simulink model "Controller_trorque_cbf_22Franka"  (R2022b)
settings: Solver=FixedStepDiscrete  StartTime=0.0  StopTime=inf  FixedStep=0.001  RelTol=1e-3
PreLoadFcn:
  | set_param(gcs, 'RTWSystemTargetFile', 'franka_emika_panda.tlc');
  | 
  | demos_common_configs();
  | collision_behavior = ones(1,52)*100;
values from neighbouring files (symbols this model uses):
  b_sg = fliplr(B(end, :))    [init_torque_cbf.m]
  cbf_dt = 0.001    [init_torque_cbf.m]
  cbf_Kd_rot = [120; 120; 120]*0    [init_torque_cbf.m]
  cbf_Kd_trans = [2000; 2000; 0]*0    [init_torque_cbf.m]
  cbf_stiff_decouple = 0    [init_torque_cbf.m]
  cbf_zeta_rot = [0.7; 0.7; 0.7]*0    [init_torque_cbf.m]
  cbf_zeta_trans = [0.7; 0.7; 0]*0    [init_torque_cbf.m]
  Dn = 20 * ones(7,1)    [init_torque_cbf.m]
  H_home = getTransform(Franka_robot, q_home, 'panda_link8', 'panda_link0')    [init_torque_cbf.m]
  Kn = 0 * ones(7,1)    [init_torque_cbf.m]
  plane_normal = [0.0; 0.0; 1.0]    [init_torque_cbf.m]
  q_home = q_init    [init_torque_cbf.m]
  q_init = [0 0  0  -(2/4)*pi  0  pi/2  -pi/4]'    [init_torque_cbf.m]
undefined symbols (not defined in the file or in its folder): cbf_torque_params, DiscIntNeverNeededParam, Fext_mag
libraries: franka_simulink_library x2, Robotics_lib x1, matrix_library x1
(part 6 of 7)

== matlab function Controller_trorque_cbf_22Franka/Dynamic Parameters/Coriolis Matrix ==
  data: q input; m output; q_dot input
function m = maple_R7plus_coriolismatrix_02(q, q_dot)
% Author: TU Wien, ACIN Robotics group
% Optimized and generated from Maple
  m = zeros(7,7);
  t2607 = q(4);
  t2593 = cos(t2607);
  t2531 = 0.345563e0 * t2593;
  t2606 = q(5);
  t2585 = sin(t2606);
  t2592 = cos(t2606);
  t3061 = 0.41065e-1 * t2585 + 0.11953e-1 * t2592;
  t2285 = t3061 + 0.825e-1;
  t2586 = sin(t2607);
  t3832 = t2285 * t2586;
  t3327 = -0.316e0 + t3832;
  t1967 = t2531 - t3327;
  t2609 = q(2);
  t2595 = cos(t2609);
  t3493 = 0.41065e-1 * t2592;
  t2464 = 0.11953e-1 * t2585 - t3493;
  t2608 = q(3);
  t2587 = sin(t2608);
  t3786 = t2587 * t2464;
  t2594 = cos(t2608);
  t2528 = 0.345563e0 * t2586;
  t3831 = t2285 * t2593;
  t4080 = t2528 + t3831;
  t3385 = 0.825e-1 - t4080;
  t4278 = t3385 * t2594;
  t1699 = t4278 + t3786;
  t2588 = sin(t2609);
  t3947 = t1699 * t2588;
  t1517 = -t1967 * t2595 + t3947;
  t2610 = q(1);
  t2596 = cos(t2610);
  t3108 = 0.61297300000000000000000000000000e0 * t2596;
  t3044 = t1517 * t3108;
  t4305 = 0.1e1 * t3044;
  t2605 = q(6);
  t2584 = sin(t2605);
  t2591 = cos(t2605);
  t2467 = 0.60149e-1 * t2591 + 0.14117e-1 * t2584;
  t3495 = 0.10517e-1 * t2592;
  t3243 = t2467 * t2585 + t3495;
  t2789 = t3243 * t2587;
  t2463 = 0.60149e-1 * t2584 - 0.14117e-1 * t2591;
  t2283 = t2463 + 0.384e0;
  t2155 = t2283 * t2586;
  t3503 = 0.10517e-1 * t2585;
  t2822 = -t2467 * t2592 + t3503;
  t4152 = 0.825e-1 + t2822;
  t4214 = t4152 * t2593;
  t3516 = -t4214 + 0.825e-1;
  t4288 = t3516 - t2155;
  t1526 = t2594 * t4288 - t2789;
  t4206 = t1526 * t2595;
  t4304 = 0.1e1 * t1526;
  t2604 = q(7);
  t2583 = sin(t2604);
  t2085 = 0.48418875570424600000000000000000e-2 * t2583 + 0.55042935974400000000000000000000e-3;
  t2590 = cos(t2604);
  t2576 = t2590 ^ 2;
  t2317 = 0.48418875570424600000000000000000e-2 * t2576;
  t3208 = 0.31608697465260160000000000000000e-2 * t2583;
  t2179 = t2590 * t3208;
  t2413 = 0.13614453378240000000000000000000e-2 * t2590;
  t3715 = t2179 - t2413;
  t1629 = -t2085 * t2583 + t2317 + t3715;
  t2417 = 0.51602752476000000000000000000000e-3 * t2590;
  t3214 = 0.12763550042100000000000000000000e-2 * t2583;
  t3681 = -t3214 + t2417;
  t1504 = t1629 * t2585 + t3681;
  t3793 = t2585 * t2584;
  t4076 = -0.33449653235675560000000000000000e-2 * t2590 + 0.10967182128164640000000000000000e-2 * t2583;
  t4303 = t2592 * (t1504 * t2591 + t3793 * t4076);
  t4301 = t1504 * t2584;
  t1692 = t1699 * t2595;
  t2156 = t2283 * t2593;
  t4215 = t2586 * t4152;
  t4230 = t2156 - t4215;
  t1706 = t4230 + 0.316e0;
  t4300 = t1706 * t2588;
  t2578 = t2592 ^ 2;
  t4235 = t1629 * t2591 + t2584 * t4076;
  t4299 = t4235 * t2578;
  t2129 = 0.4841887557042460000000000000000e-2 * t2583 + 0.55042935974400000000000000000000e-3;
  t2324 = 0.15804348732630080000000000000000e-2 * t2576;
  t2356 = 0.13614453378240000000000000000000e-2 * t2583;
  t3689 = t2324 + t2356;
  t1675 = -t2129 * t2590 + t3689 - 0.5826996021941340000000000000000e-3;
  t2347 = 0.59408523832320000000000000000000e-2 * t2583;
  t2412 = 0.24018735697920000000000000000000e-2 * t2590;
  t2026 = t2347 - t2412;
  t1891 = 0.47796540830203740000000000000000e-1 - t2026;
  t1498 = -t1675 * t2584 + t1891;
  t3158 = 0.10967182128164640000000000000000e-2 * t2590;
  t3207 = 0.33449653235675560000000000000000e-2 * t2583;
  t2029 = t3158 + t3207;
  t1896 = t2029 + 0.18713819462921000000000000000000e-3;
  t3916 = t1896 * t2591;
  t4289 = t1498 + t3916;
  t4298 = t4289 * t2592;
  t3802 = t2583 * t2590;
  t3035 = 0.85600000000000000000000000000000e-3 * t3802;
  t2812 = 0.28220000000000000000000000000000e-2 + t3035;
  t3238 = 0.2489000000000000000000000000000e-2 * t2576;
  t1821 = t2812 + t3238;
  t2577 = t2591 ^ 2;
  t1775 = t1821 * t2577;
  t4174 = -0.23920000000000000000000000000000e-2 * t2590 + 0.14820000000000000000000000000000e-2 * t2583;
  t1985 = -t4174 + 0.218e-3;
  t3796 = t2584 * t2591;
  t3618 = t1985 * t3796;
  t2321 = 0.24890000000000000000000000000000e-2 * t2576;
  t1809 = t2321 + t2812;
  t3710 = -t3035 - t2321;
  t1812 = -t3710 - 0.27050000000000000000000000000000e-2;
  t1414 = t1809 * t2577 + t1812 - t3618;
  t1397 = t1414 * t2578;
  t3154 = 0.14820000000000000000000000000000e-2 * t2590;
  t2200 = t2584 * t3154;
  t3211 = 0.23920000000000000000000000000000e-2 * t2583;
  t2267 = 0.682e-3 + t3211;
  t3033 = 0.49780000000000000000000000000000e-2 * t3802;
  t3222 = 0.17120000000000000000000000000000e-2 * t2576;
  t2726 = t3033 - t3222 - 0.14600000000000000000000000000000e-2;
  t2713 = t2726 * t2591;
  t3534 = t2267 * t2584 + t2200 - t2713;
  t1549 = 0.4234e-2 - t3534;
  t3761 = t2592 * t2585;
  t1518 = t1549 * t3761;
  t3736 = -t1518 - t1397;
  t4297 = -t3736 - t3618 + t1775;
  t1960 = t3681 * t2584;
  t2408 = 0.59408523832320000000000000000000e-2 * t2590;
  t3210 = 0.24018735697920000000000000000000e-2 * t2583;
  t3678 = -t3210 - t2408;
  t4286 = t1629 * t2584 + t3678;
  t4295 = -t2585 * t4286 - t1960;
  t2024 = 0.10517000000000000000000000000000e-1 * t2583 - 0.42520000000000000000000000000000e-2 * t2590;
  t1962 = t2024 * t2585;
  t2028 = 0.10517000000000000000000000000000e-1 * t2590 + 0.42520000000000000000000000000000e-2 * t2583;
  t1887 = 0.88000000000000000000000000000000e-1 + t2028;
  t3197 = 0.61597000000000000000000000000000e-1 * t2584;
  t3764 = t2591 * t2592;
  t3725 = t1887 * t3764 + t2592 * t3197;
  t4099 = t1962 + t3725;
  t1501 = 0.82500000000000000000000000000000e-1 - t4099;
  t4294 = t1501 * t2586;
  t4293 = t1501 * t2593;
  t3213 = 0.15804348732630080000000000000000e-2 * t2583;
  t2089 = -0.27228906756480000000000000000000e-2 + t3213;
  t3157 = 0.11008587194880000000000000000000e-2 * t2590;
  t3141 = 0.96837751140849200000000000000000e-2 * t2590;
  t2177 = t2583 * t3141;
  t3706 = -t2177 + t2324;
  t1627 = t2089 * t2583 + t3157 - t3706;
  t4275 = t1627 * t2584 - t2026;
  t3976 = t4275 * t2591;
  t2318 = 0.48152918111602840000000000000000e-2 * t2576;
  t2569 = t2583 ^ 2;
  t2299 = 0.26595745882176000000000000000000e-4 * t2569;
  t2357 = 0.11008587194880000000000000000000e-2 * t2583;
  t3692 = -t2299 - t2357;
  t3848 = t2089 * t2590;
  t3524 = -t3848 - t3692;
  t2932 = 0.17806630741175110000000000000000e-1 + t3524;
  t1592 = -t2318 + t2932;
  t2902 = (0.2e1 * t1592 - 0.12491350982639572000000000000000e-1) * t3796;
  t2589 = sin(t2610);
  t2575 = t2589 ^ 2;
  t2582 = t2596 ^ 2;
  t4260 = t2575 + t2582;
  t1322 = -t1526 * t2588 + t1706 * t2595;
  t2466 = 0.39252e-1 * t2594 + 0.27518e-1 * t2587;
  t3481 = 0.249498e0 * t2588;
  t3059 = 0.39252e-1 * t2587 - 0.27518e-1 * t2594;
  t4201 = t3059 * t2595;
  t2818 = t4201 - t3481;
  t4273 = t2466 * t2589 + t2596 * t2818;
  t4292 = 0.1e1 * t4273;
  t3970 = t1592 * t2577;
  t3201 = 0.11357396418885000000000000000000e-1 * t2584;
  t2099 = -0.24178658687700000000000000000000e-2 + t3201;
  t3155 = 0.12763550042100000000000000000000e-2 * t2590;
  t3220 = 0.51602752476000000000000000000000e-3 * t2583;
  t3684 = -t3220 - t3155;
  t1894 = -t3684 + 0.27219646194675000000000000000000e-1;
  t3918 = t1894 * t2591;
  t1681 = -t3918 - t2099;
  t3952 = t1681 * t2585;
  t1651 = t1681 * t2592;
  t2470 = 0.10517e-1 * t2590 + 0.4252e-2 * t2583;
  t2288 = t2470 + 0.88e-1;
  t3504 = 0.61597e-1 * t2584;
  t3244 = t2288 * t2591 + t3504;
  t3065 = 0.10517e-1 * t2583 - 0.4252e-2 * t2590;
  t4212 = t2585 * t3065;
  t2699 = t2592 * t3244 + t4212;
  t2693 = 0.825e-1 - t2699;
  t4290 = t2593 * t2693;
  t1595 = t1627 * t2577;
  t3676 = -0.66899306471351120000000000000000e-2 * t2583 - 0.21934364256329280000000000000000e-2 * t2590;
  t1922 = t3676 * t3796;
  t3262 = -t1922 - t1595;
  t2361 = 0.63817750210500000000000000000000e-3 * t2583;
  t2418 = 0.25801376238000000000000000000000e-3 * t2590;
  t3682 = t2418 - t2361;
  t2415 = 0.68072266891200000000000000000000e-3 * t2590;
  t3209 = 0.24209437785212300000000000000000e-2 * t2583;
  t2088 = 0.27521467987200000000000000000000e-3 + t3209;
  t3851 = t2088 * t2583;
  t3153 = 0.15804348732630080000000000000000e-2 * t2590;
  t2181 = t2583 * t3153;
  t2322 = 0.24209437785212300000000000000000e-2 * t2576;
  t4094 = t2181 + t2322;
  t1631 = t2415 + t3851 - t4094;
  t3966 = t1631 * t2585;
  t4287 = t3682 - t3966;
  t3496 = 0.61597e-1 * t2591;
  t3830 = t2288 * t2584;
  t2783 = -t3496 + t3830;
  t4044 = 0.384e0 + t2783;
  t3889 = t4044 * t2593;
  t4285 = t2586 * t2693 - t3889 - 0.316e0;
  t4283 = t1631 * t2584;
  t4282 = t1631 * t2591;
  t3506 = 0.5317e-1 * t2593;
  t3060 = 0.104419e0 * t2586 + t3506;
  t2286 = t3060 - 0.825e-1;
  t3497 = 0.27454e-1 * t2587;
  t2015 = t2286 * t2594 - t3497;
  t1943 = t2015 * t2595;
  t3511 = 0.5317e-1 * t2586;
  t2516 = -0.316e0 + t3511;
  t3475 = 0.104419e0 * t2593;
  t1694 = t2588 * (t2516 - t3475) + t1943;
  t4281 = t1694 * t2596;
  t4210 = t3385 * t2587;
  t4200 = t3065 * t2592;
  t2700 = t2585 * t3244 - t4200;
  t3888 = t4044 * t2586;
  t4045 = 0.825e-1 - t3888;
  t2661 = -t2700 * t2587 + (t4045 - t4290) * t2594;
  t1089 = t2588 * t2661 + t2595 * t4285;
  t4169 = 0.735522e0 * t4260 * t1089;
  t1924 = 0.3742763892584200000000000000000e-3 - t3676;
  t3900 = t1924 * t2591;
  t2084 = 0.96837751140849200000000000000000e-2 * t2583 + 0.11008587194880000000000000000000e-2;
  t2319 = 0.31608697465260160000000000000000e-2 * t2576;
  t2351 = 0.27228906756480000000000000000000e-2 * t2583;
  t4227 = t2319 + t2351 - 0.11653992043882680000000000000000e-2;
  t1667 = -t2084 * t2590 + t4227;
  t4268 = t1667 * t2584;
  t4277 = t3900 - t4268;
  t3223 = 0.85600000000000000000000000000000e-3 * t2576;
  t2804 = -0.85600000000000000000000000000000e-3 * t2569 + t3223;
  t1783 = t2804 - t3033;
  t2033 = t3154 + t3211;
  t3614 = t2033 * t3796;
  t1393 = t1783 * t2577 + t1783 + t3614;
  t3705 = t4174 * t2584;
  t2316 = 0.49780000000000000000000000000000e-2 * t2576;
  t4090 = -0.49780000000000000000000000000000e-2 * t2569 + t2316 + 0.34240000000000000000000000000000e-2 * t3802;
  t4165 = t2591 * t4090 + t3705;
  t3737 = -t1393 * t2578 - t3761 * t4165;
  t2341 = 0.4841887557042460000000000000000e-2 * t2576;
  t3869 = t4076 * t2591;
  t3444 = -t3678 + t3869;
  t4274 = t2584 * (-t2129 * t2583 + t2341 + t3715) - t3444;
  t1955 = t3682 * t2586;
  t4272 = 0.1e1 * t1955;
  t4271 = 0.1e1 * t2589;
  t2994 = 0.11198654185125000000000000000000e-1 + t3681;
  t3911 = t2994 * t2592;
  t4270 = 0.1e1 * t3911;
  t3492 = 0.61597e-1 * t2592;
  t2480 = t2584 * t3492;
  t4065 = -t2288 * t3764 - t4212;
  t1704 = t2480 - 0.825e-1 - t4065;
  t4267 = t1704 * t2593;
  t2007 = t2531 - t3832;
  t3743 = t2595 * t2594;
  t4264 = t2007 * t3743;
  t2451 = 0.11357396418885000000000000000000e-1 * t2591;
  t3921 = t1894 * t2584;
  t4161 = t3921 - t2451;
  t1698 = t2592 * t4161;
  t4263 = t2700 * t2594;
  t2973 = -0.11022068765350630000000000000000e-1 + t4076;
  t1769 = t2973 * t2586;
  t3753 = t2593 * t2584;
  t1795 = t2973 * t3753;
  t4261 = t4230 * t3743;
  t3212 = 0.16724826617837780000000000000000e-2 * t2583;
  t2130 = 0.9356909731460500000000000000000e-4 + t3212;
  t3164 = 0.54835910640823200000000000000000e-3 * t2590;
  t2965 = t2130 + t3164;
  t2105 = 0.12669508046976000000000000000000e0 + t3210;
  t2993 = -t2408 - t2105;
  t2300 = 0.13297872941088000000000000000000e-4 * t2569;
  t2362 = 0.55042935974400000000000000000000e-3 * t2583;
  t3694 = t2300 + t2362;
  t2989 = -0.32797153116247448000000000000000e-1 - t3694;
  t3239 = 0.2407645905580142000000000000000e-2 * t2576;
  t4259 = t2989 + t3239;
  t3131 = 0.61597000000000000000000000000000e-1 * t2591;
  t3932 = t1887 * t2584;
  t2893 = -t3131 + t3932;
  t1679 = t2893 + 0.38400000000000000000000000000000e0;
  t1650 = t1679 * t2586;
  t1636 = -0.825e-1 + t1650;
  t1525 = 0.825e-1 - t4099;
  t3972 = t1525 * t2593;
  t4191 = (t1636 + t3972) * t2594;
  t3791 = t2585 * t2591;
  t3276 = -t2288 * t3791 - t2585 * t3504 + t4200;
  t4241 = t3276 * t2587;
  t2987 = t4191 - t4241;
  t1239 = t2987 * t2589;
  t3742 = t2596 * t2587;
  t3772 = t2589 * t2588;
  t1369 = t1525 * t3742 - t3772 * t4044;
  t3973 = t1525 * t2586;
  t1484 = -0.316e0 + t3973;
  t2508 = 0.825e-1 * t3742;
  t3784 = t2587 * t2586;
  t3948 = t3276 * t2594;
  t1084 = t1484 * t3772 + t1239 * t2595 + t1369 * t2593 - t2508 + (t1679 * t3784 + t3948) * t2596;
  t3348 = -t1887 * t3791 - t2585 * t3197;
  t1576 = t4200 + t3348;
  t3747 = t2594 * t2593;
  t3349 = t1576 * t2587 + t1704 * t3747 + t2594 * t4045;
  t1281 = t3349 * t2596;
  t3741 = t2596 * t2588;
  t3773 = t2589 * t2587;
  t1483 = -t1704 * t3773 + t3741 * t4044;
  t3950 = t1704 * t2586;
  t1665 = 0.316e0 + t3950;
  t3971 = t1576 * t2594;
  t1112 = t1665 * t3741 + t1281 * t2595 + t1483 * t2593 + (-t2587 * t4045 + t3971) * t2589;
  t3109 = 0.36776100000000000000000000000000e0 * t2596;
  t3172 = 0.36776100000000000000000000000000e0 * t2589;
  t4175 = t1084 * t3109 + t1112 * t3172;
  t1862 = t1924 * t2584;
  t3103 = -t1667 * t2591 + 0.60609778933081200000000000000000e-2;
  t1441 = t3103 - t1862;
  t3221 = 0.25801376238000000000000000000000e-3 * t2583;
  t2107 = 0.13609823097337500000000000000000e-1 + t3221;
  t3163 = 0.63817750210500000000000000000000e-3 * t2590;
  t2996 = -t3163 - t2107;
  t4073 = -0.2392e-2 * t2590 + 0.1482e-2 * t2583;
  t3867 = t3682 * t2593;
  t4257 = -t3867 + t3682;
  t2416 = 0.55042935974400000000000000000000e-3 * t2590;
  t2038 = t2356 - t2416;
  t3876 = t2026 * t2584;
  t3531 = t3876 + t2038;
  t3917 = t1896 * t2584;
  t1739 = t3917 - 0.30304889466540600000000000000000e-2;
  t4256 = t1739 * t2585 - t2099;
  t3850 = t2088 * t2590;
  t2325 = 0.79021743663150400000000000000000e-3 * t2576;
  t2360 = 0.68072266891200000000000000000000e-3 * t2583;
  t2835 = -0.29134980109706700000000000000000e-3 + t2360;
  t4178 = -t2835 - t2325;
  t2861 = -0.1e1 * t3850 - t4178;
  t4255 = -0.1e1 * t2582 - 0.1e1 * t2575;
  t4179 = 0.24890000000000000000000000000000e-2 * t3802 - 0.73000000000000000000000000000000e-3 - t3223;
  t3942 = t4179 * t2584;
  t4254 = 0.229e-3 - t3942;
  t3143 = 0.48418875570424600000000000000000e-2 * t2590;
  t3034 = t2583 * t3143;
  t3226 = 0.79021743663150400000000000000000e-3 * t2569;
  t3691 = -t3226 + t2325;
  t3527 = -t3034 + t3691;
  t3218 = 0.79021743663150400000000000000000e-3 * t2583;
  t2091 = -0.13614453378240000000000000000000e-2 + t3218;
  t2911 = -t2325 + t3034;
  t1633 = -t2091 * t2583 - t2416 - t2911;
  t3615 = t2029 * t3796;
  t4069 = t1633 * t2577 + t3615;
  t1341 = (t3527 + t4069) * t2578;
  t3738 = t3761 * t4235 + t1341;
  t1961 = t3676 * t2577;
  t4252 = 0.1e1 * t1961;
  t3650 = t2973 * t3796;
  t4251 = 0.1e1 * t3650;
  t3925 = t2973 * t2577;
  t4250 = 0.1e1 * t3925;
  t4249 = t2593 - 0.1e1;
  t3148 = 0.24444132201840000000000000000000e-2 * t2590;
  t3217 = 0.98827089590400000000000000000000e-3 * t2583;
  t2046 = -t3217 - t3148;
  t1907 = -t2046 + 0.52129746651620000000000000000000e-1;
  t1858 = t1907 * t2584;
  t2093 = -t2361 + 0.55993270925625000000000000000000e-2;
  t4084 = t2418 + t2093;
  t3935 = t4084 * t2585;
  t1540 = 0.58416762559717300000000000000000e0 + t3935 + t1858;
  t4248 = t1540 * t2593;
  t1742 = -t1896 * t2585 + 0.11357396418885000000000000000000e-1;
  t4217 = t1742 * t2584;
  t4216 = t1742 * t2591;
  t4246 = t2578 * t3747;
  t3657 = t1809 * t3796;
  t2570 = t2584 ^ 2;
  t3815 = t2577 * t1985;
  t4164 = -t1985 * t2570 + t3815;
  t4061 = 0.2e1 * t3657 + t4164;
  t4245 = t2578 * t4061;
  t3781 = t2587 * t2593;
  t2792 = t2588 * t2822;
  t2132 = t2464 * t3747;
  t4042 = t2587 * t3061 + t2132;
  t4244 = t2588 * t4042;
  t2491 = 0.4978e-2 * t3802;
  t2527 = 0.1712e-2 * t2576;
  t2880 = -0.1460e-2 + t2491 - t2527;
  t4243 = t2591 * t2880;
  t2791 = t2822 * t2593;
  t2400 = 0.63817750210500000000000000000000e-3 * t2586;
  t4026 = 0.29704261916160000000000000000000e-2 - t2400;
  t4240 = t4026 * t2590;
  t4239 = (t2587 * t3065 + t3244 * t3747) * t2585;
  t2871 = t2288 * t2586;
  t3489 = 0.61597e-1 * t2593;
  t4238 = (t2592 * t3489 - t2871) * t2591;
  t4237 = t4179 * t2591;
  t1878 = -0.89033153705875550000000000000000e-2 - t3694;
  t2323 = 0.24076459055801420000000000000000e-2 * t2576;
  t3846 = t2091 * t2590;
  t1589 = t2323 + t3846 + t1878;
  t4143 = -0.2e1 * t1589 - 0.62456754913197860000000000000000e-2;
  t2901 = t4143 * t3796;
  t3926 = t2973 * t2570;
  t3450 = -t3925 + t3926;
  t1302 = (t2901 - t3450) * t2578;
  t3907 = t2993 * t2591;
  t4236 = t1302 - t3907;
  t1947 = t2029 + 0.187138194629210e-3;
  t1766 = t1947 * t2585 - 0.11357396418885000000000000000000e-1;
  t1735 = t1766 * t2591;
  t4234 = t1891 * t2585 + t1735 + 0.27752814537092170000000000000000e0;
  t3698 = 0.17120000000000000000000000000000e-2 * t2569 - t3222;
  t1788 = -0.9956000000000000000000000000000e-2 * t3802 - t3698;
  t2245 = 0.4978000000000000000000000000000e-2 * t3802;
  t1789 = t2804 - t2245;
  t4233 = -t1789 * t2577 + t1788 - t3614;
  t1951 = t2029 * t2577;
  t3679 = -t3212 - t3164;
  t4232 = t1951 + t3679;
  t4231 = t2155 + t4214;
  t2180 = 0.17120000000000000000000000000000e-2 * t3802;
  t2340 = 0.4978000000000000000000000000000e-2 * t2576;
  t3713 = t2180 + t2340;
  t1823 = 0.5644000000000000000000000000000e-2 + t3713;
  t3619 = t1823 * t3796;
  t4229 = -0.8292e-2 + t3619 + t4174;
  t2182 = t2590 * t3218;
  t2298 = 0.81354094419858000000000000000000e-4 * t2569;
  t3711 = t2182 + t2298;
  t3528 = 0.25022978729410880000000000000000e-2 * t2576 + t3711;
  t2882 = -0.31228377456598930000000000000000e-2 * t2570 + t3528;
  t2571 = t2585 ^ 2;
  t3912 = t2994 * t2585;
  t3712 = t2181 + t3912;
  t4228 = -0.22516878283212450000000000000000e-2 * t2571 - t3712;
  t4226 = 0.8292e-2 - t4073;
  t1600 = t1633 * t2584;
  t2350 = 0.29704261916160000000000000000000e-2 * t2583;
  t2414 = 0.12009367848960000000000000000000e-2 * t2590;
  t2030 = t2350 - t2414;
  t4105 = t1600 + t2030;
  t3977 = t4105 * t2591;
  t4225 = -t4232 + t3977;
  t4224 = t3681 - t3867;
  t4222 = -0.1e1 * t2576 + t2569;
  t3087 = -0.65941286852573577000000000000000e0 - t2362;
  t2104 = 0.17600000000000000000000000000000e0 + 0.76800000000000000000000000000000e0 * t2584;
  t3393 = 0.7735484874e-2 * t2590;
  t3295 = t2104 * t3393;
  t4221 = t3087 - 0.1e1 * t3295;
  t2714 = t2726 * t2584;
  t4220 = t2714 - 0.458e-3;
  t3507 = 0.4252e-2 * t2592;
  t3512 = 0.4252e-2 * t2585;
  t2730 = t2583 * (t2591 * t3495 - t3512) - t2590 * (t2591 * t3507 + t3503);
  t3799 = t2584 * t2586;
  t4116 = t3065 * t3799;
  t4219 = t2594 * (-t2593 * t2730 + t4116) + (t2583 * (t2591 * t3503 + t3507) - t2590 * (t2591 * t3512 - t3495)) * t2587;
  t1948 = -t3679 + 0.93569097314605e-4;
  t3132 = 0.52863517876992000000000000000000e-1 * t2591;
  t2353 = 0.24444132201840000000000000000000e-2 * t2583;
  t3160 = 0.98827089590400000000000000000000e-3 * t2590;
  t4172 = -t3160 + t2353;
  t2997 = -0.21447119530300000000000000000000e-1 + t4172;
  t3924 = t2973 * t2584;
  t1737 = 0.52863517876992000000000000000000e-1 - t3924;
  t4218 = t1737 * t2591;
  t4213 = t2015 * t2588;
  t3215 = 0.12009367848960000000000000000000e-2 * t2583;
  t2094 = -t3215 - 0.63347540234880000000000000000000e-1;
  t3844 = t2094 * t2584;
  t3783 = t2587 * t2591;
  t4211 = t2587 * t3244;
  t3067 = 0.2872e-1 * t2588 - 0.3141e-2 * t2595;
  t4208 = t2589 * t3067;
  t3749 = t2594 * t2585;
  t4207 = t2591 * t3749;
  t4205 = t2596 * t3067;
  t3785 = t2587 * t2585;
  t4204 = t2783 * t3785;
  t2363 = 0.54835910640823200000000000000000e-3 * t2583;
  t3152 = 0.16724826617837780000000000000000e-2 * t2590;
  t2801 = -t3152 + t2363;
  t4203 = t2801 * t2584;
  t4202 = t2801 * t2591;
  t2524 = 0.3507900e-3 * t2585;
  t3229 = 0.925496e-3 + t2524;
  t3474 = 0.735522e0 * t2593;
  t4199 = t3229 * t3474;
  t3746 = t2595 * t2586;
  t4198 = t3243 * t3746;
  t1931 = t3243 * t3747;
  t3779 = t2588 * t2586;
  t4115 = t3243 * t3779;
  t1537 = t1549 * t2578;
  t3216 = 0.11960000000000000000000000000000e-2 * t2583;
  t2268 = -0.341e-3 - t3216;
  t2072 = t2268 * t2584 + 0.3449e-2;
  t3162 = 0.74100000000000000000000000000000e-3 * t2590;
  t3028 = t2584 * t3162;
  t3609 = t1414 * t3761;
  t4048 = -t1537 - t3028 + t3609 + t4237 + t2072;
  t4196 = t4048 * t2586;
  t4195 = t4048 * t2593;
  t1918 = t4076 * t3791;
  t4192 = t4288 * t2587;
  t1999 = t2099 * t2585;
  t1584 = t1999 - t3917 - 0.47802211058981400000000000000000e-2;
  t4190 = -t1441 * t2578 + t1584;
  t3198 = 0.52863517876992000000000000000000e-1 * t2584;
  t1762 = -t4076 + t3198 + 0.8968493211292842000000000000000e-2;
  t2034 = -0.66899306471351120000000000000000e-2 * t2590 + 0.21934364256329280000000000000000e-2 * t2583;
  t1888 = 0.22044137530701260000000000000000e-1 - t2034;
  t3930 = t1888 * t2577;
  t3452 = t1762 - t3930;
  t4098 = t2965 * t2584;
  t1867 = -t2091 * t2584 + 0.29704261916160000000000000000000e-2;
  t1949 = t2416 + 0.26595745882176000000000000000000e-4 * t3802;
  t2216 = t2584 * t2325;
  t3233 = 0.4815291811160284000000000000000e-2 * t2590;
  t1390 = t1949 * t2584 - t2216 + t2414 + (t2584 * t3233 - 0.1e1 * t1867) * t2583;
  t4189 = t1390 * t2591 + t4232;
  t2080 = -0.23044843893347959000000000000000e-1 - t2298;
  t2512 = 0.13297872941088e-4 * t2576;
  t4188 = t2080 - t2512;
  t2092 = -t3220 - 0.27219646194675000000000000000000e-1;
  t4187 = t2092 - t3155;
  t2115 = -0.52129746651620000000000000000000e-1 - t3217;
  t4186 = t2115 - t3148;
  t3714 = t2180 + t2316;
  t2795 = -0.47840000000000000000000000000000e-2 * t2590 + 0.29640000000000000000000000000000e-2 * t2583;
  t1988 = t2795 - 0.436e-3;
  t1937 = t1988 * t2577;
  t4185 = -0.1e1 * t1937 + t4229;
  t3219 = 0.74100000000000000000000000000000e-3 * t2583;
  t2264 = 0.4146e-2 - t3219;
  t3156 = 0.11960000000000000000000000000000e-2 * t2590;
  t3620 = t1821 * t3796;
  t4184 = t2264 - 0.1e1 * t3815 - 0.1e1 * t3620 + t3156;
  t2982 = -t2300 + t3239;
  t3695 = t2300 - t2323;
  t4148 = -t2182 - 0.2489553776598930000000000000000e-3;
  t1714 = t2982 - t4148;
  t4183 = -t1714 * t2577 + t2341;
  t3683 = -t2362 - t2413;
  t2803 = t2415 - t2322;
  t4181 = t1896 * t3791 - t2451;
  t4059 = t3850 - t2325;
  t1670 = -t2835 + t4059;
  t1644 = t1670 * t2585;
  t2106 = -0.31600000000000000000000000000000e0 * t2586 + 0.82500000000000000000000000000000e-1;
  t2916 = 0.3127439544e-2 * t2583 + t3393;
  t2454 = 0.21751134959804000000000000000000e-1 * t2592;
  t2991 = t2454 - t2107;
  t2928 = t2991 - t3163;
  t4180 = t2916 * t2106 + t2593 * t2928 + t1644 + 0.13609823097337500000000000000000e-1;
  t3096 = t2363 - 0.44842466056464210000000000000000e-2;
  t3188 = 0.12089329343850000000000000000000e-2 * t2586;
  t2722 = 0.46305794820080000000000000000000e-2 * t2593 + t3096 - t3188;
  t4177 = t3198 + t4236;
  t1333 = t4300 + t4206;
  t2788 = t3243 * t2594;
  t1514 = -t2788 - t4192;
  t3975 = t1514 * t2589;
  t1211 = t1333 * t2596 + t3975;
  t2565 = 0.316e0 * t2588;
  t1334 = -t2588 * t4230 - t2565 - t4206;
  t3974 = t1514 * t2596;
  t1214 = t1334 * t2589 + t3974;
  t3106 = 0.83327750000000000000000000000000e0 * t2596;
  t3169 = 0.83327750000000000000000000000000e0 * t2589;
  t4176 = t1211 * t3169 + t1214 * t3106;
  t2044 = t3163 + t3221;
  t3473 = 0.104419e0 * t2595;
  t4060 = t2516 * t2595 - t2593 * t3473;
  t1574 = -t4213 + t4060;
  t4171 = 0.3587895e1 * t4260 * t1574;
  t1963 = t2024 * t2592;
  t4170 = t3348 + t1963;
  t2405 = 0.54835910640823200000000000000000e-3 * t2587;
  t3361 = 0.2444413220184e-2 * t2594;
  t3671 = -t3361 + t2405;
  t3373 = 0.6381775021050e-3 * t2586;
  t2890 = 0.2444413220184e-2 * t2593 - t3373;
  t4167 = 0.4784e-2 * t2590 - 0.2964e-2 * t2583;
  t4160 = 0.62456754913197860000000000000000e-2 * t2570 - 0.16270818883971600000000000000000e-3 * t2569 - 0.50045957458821760000000000000000e-2 * t2576 - t2181;
  t3471 = 0.345563e0 * t2595;
  t2479 = t2593 * t3471;
  t3520 = 0.825e-1 * t2593;
  t2520 = 0.825e-1 - t3520;
  t2946 = 0.41065e-1 * t3747 - 0.11953e-1 * t2587;
  t3522 = 0.825e-1 * t2586;
  t3271 = -0.316e0 + t3522;
  t3480 = 0.345563e0 * t2588;
  t3352 = t2594 * t3480;
  t3378 = 0.11953e-1 * t3747;
  t3775 = t2588 * t2594;
  t3777 = t2588 * t2592;
  t3778 = t2588 * t2587;
  t3792 = t2585 * t2588;
  t1330 = -t2520 * t3775 + t2586 * t3352 - t2595 * t3271 + t2946 * t3792 - t3061 * t3746 + t3378 * t3777 + t3493 * t3778 + t2479;
  t4158 = 0.1225946e1 * t4255 * t1330;
  t3441 = 0.1666555e1 * t1322;
  t3341 = t2582 * t3441;
  t3342 = t2575 * t3441;
  t4157 = 0.1e1 * t3341 + 0.1e1 * t3342;
  t4156 = t2180 + t2321 - 0.24890000000000000000000000000000e-2 * t2569;
  t4155 = t2181 - t2803;
  t3758 = t2592 * t2590;
  t4154 = t2091 * t3758 + t2592 * t4259;
  t4151 = -t2588 * t3059 - 0.249498e0 * t2595;
  t1654 = t2882 - 0.6284682367054690000000000000000e-3;
  t3852 = t2085 * t2590;
  t4147 = t3852 + 0.5826996021941340000000000000000e-3;
  t4146 = 0.16143020000000000000000000000000e1 * t4151;
  t3192 = 0.50000000000000000000000000000000e0 * t2585;
  t2087 = t2350 - 0.23898270415101870000000000000000e-1;
  t4144 = -t3912 - 0.80863245317250000000000000000000e-1;
  t3182 = 0.82500000000000000000000000000000e-1 * t2586;
  t2101 = -0.31600000000000000000000000000000e0 + t3182;
  t4142 = -t2101 * t2916 + 0.52129746651620000000000000000000e-1;
  t2102 = -0.38400000000000000000000000000000e0 + t3182;
  t4141 = t2102 * t2916 - 0.63347540234880000000000000000000e-1;
  t4022 = 0.2e1 * t2584;
  t4140 = 0.2e1 * t3761;
  t3523 = -t3852 + t3689;
  t1673 = -0.5826996021941340000000000000000e-3 + t3523;
  t4137 = t1673 * t2585;
  t4136 = t2029 * t3799;
  t4135 = t2087 * t2594;
  t4134 = t2093 * t2593;
  t3519 = 0.384e0 * t2593;
  t2292 = -t3271 + t3519;
  t4131 = t2292 * t2591;
  t4130 = t2463 * t2586;
  t4129 = t2466 * t2588;
  t3814 = t2577 * t2585;
  t3999 = t2595 / 0.2e1;
  t3578 = t2577 * t3999;
  t4128 = t2578 * t2586;
  t3748 = t2594 * t2586;
  t3547 = t3748 / 0.2e1;
  t3408 = t2578 * t3547;
  t2579 = t2593 ^ 2;
  t2581 = t2595 ^ 2;
  t4013 = t2581 / 0.2e1;
  t3577 = t2579 * t4013;
  t3789 = t2586 * t2585;
  t4126 = t2587 * t3060;
  t3765 = t2591 * t2586;
  t3751 = t2593 * t2591;
  t2472 = 0.2872e-1 * t2595 + 0.3141e-2 * t2588;
  t2602 = q_dot(2);
  t3435 = 0.3228604e1 * t2818;
  t2465 = -t3475 + t3511;
  t3518 = 0.825e-1 * t2595;
  t3387 = t2594 * t3518;
  t3672 = -t3387 - t2565;
  t3436 = 0.3587895e1 * t2465 * t2588 + 0.3587895e1 * (t2594 * t3060 - 0.1e1 * t3497) * t2595 + 0.3587895e1 * t3672;
  t3521 = 0.825e-1 * t2588;
  t2497 = t2586 * t3521;
  t3398 = t2593 * t3387 + t2497 + t3672;
  t4117 = t3061 * t2593;
  t4118 = t3061 * t2586;
  t3438 = 0.1225946e1 * (-0.1e1 * t2531 + t4118) * t2588 + 0.1225946e1 * (-0.1e1 * t3786 + (t2528 + t4117) * t2594) * t2595 + 0.1225946e1 * t3398;
  t3517 = 0.384e0 * t2595;
  t3389 = t2594 * t3517;
  t3440 = 0.1666555e1 * t2586 * t3389 + 0.1666555e1 * (t2789 + (t4130 + t2791) * t2594) * t2595 + 0.1666555e1 * t3398 + 0.1666555e1 * (-0.1e1 * t2463 * t2593 + t2586 * t2822 - 0.1e1 * t3519) * t2588;
  t3486 = -0.735522e0 * t4285 * t2588 + 0.735522e0 * t2661 * t2595;
  t4123 = t2602 * (t1089 * t3486 + t1322 * t3440 + t1330 * t3438 - t1574 * t3436 - 0.646926e0 * t2472 * t3067 - t3435 * t4151);
  t2706 = t4090 * t2584;
  t3760 = t2592 * t2586;
  t3254 = t2463 * t3760 - t2467 * t2593;
  t4114 = t3254 * t2588;
  t3757 = t2592 * t2593;
  t3255 = t2463 * t3757 + t2467 * t2586;
  t1774 = t3255 * t2594;
  t4113 = t3867 * t2591;
  t1495 = t4187 + t4137;
  t1471 = t1495 * t2591;
  t1306 = t1471 + t4256;
  t1712 = t3695 + t4148;
  t3097 = t2362 + 0.89033153705875550000000000000000e-2;
  t1591 = -t3846 + t3097 + t3695;
  t1568 = t1591 * t2577;
  t3264 = -t3650 + t1568;
  t3266 = t3264 - t2882;
  t1295 = 0.28801560650267140000000000000000e-2 + t3266;
  t1899 = -0.60294330025875550000000000000000e-2 + t3683;
  t3908 = t2993 * t2584;
  t4027 = -t3908 + 0.54361295502067749900000000000000e0;
  t2840 = t1295 * t2578 + t1899 * t2570 - t4027 + t4218 - t4228;
  t1081 = t1306 * t2592 + t1712 * t2577 + t2317 + t2840;
  t1653 = -0.1256936473410938000000000000000e-2 - t4160;
  t3651 = t1888 * t3796;
  t3265 = -t3651 - t3970;
  t1296 = t1653 + t3265;
  t4112 = -0.73920491408125335100000000000000e0 + t1296 * t2578 + t1441 * t3761 + 0.18916511922000000000000000000000e0 * t2586 - t2322 - t2182 + t1081 * t2579;
  t1877 = -0.11560955249855324000000000000000e-1 + t3692;
  t2935 = t3848 + t1877;
  t3236 = 0.4815291811160284000000000000000e-2 * t2576;
  t1603 = t2935 + t3236;
  t1450 = t1603 * t2584 + t2993;
  t3981 = t1450 * t2591;
  t1277 = -t3452 + t3981;
  t1272 = t1277 * t2592;
  t3101 = t3921 + 0.27752814537092170000000000000000e0;
  t4111 = t1272 + t3101;
  t2295 = 0.15804348732630080000000000000000e-2 * t2569;
  t3697 = t2295 - t2324;
  t3866 = t3684 * t2585;
  t4110 = t1341 + t3697 - t3866 + t4303;
  t1876 = 0.57804776249276620000000000000000e-2 + t3694;
  t2985 = t1876 - t3239;
  t1421 = t1867 * t2590 + t2584 * t2985 - t2094;
  t1401 = t1421 * t2593;
  t1897 = t2044 + 0.13609823097337500000000000000000e-1;
  t1852 = t1897 * t2586;
  t3735 = t1401 - t1852;
  t1674 = -t3689 + t4147;
  t3955 = t1674 * t2584;
  t1496 = t1891 + t3955;
  t3893 = t1947 * t2591;
  t4109 = t1496 + t3893;
  t3146 = 0.29704261916160000000000000000000e-2 * t2590;
  t2040 = t3146 + t3215;
  t1505 = t4283 + t2040;
  t4108 = t1505 + t4202;
  t2930 = -t3846 + t1876;
  t1605 = -t3239 + t2930;
  t1570 = t1605 * t2584;
  t1884 = t2040 + 0.63347540234880000000000000000000e-1;
  t4107 = t1570 + t1884;
  t3767 = t2590 * t2591;
  t1583 = t2088 * t3767 + t2591 * t4178;
  t1925 = -t3679 + 0.9356909731460500000000000000000e-4;
  t3899 = t1925 * t2584;
  t4106 = t1583 - t3899;
  t1647 = t1674 * t2591;
  t1440 = t1647 - t1739;
  t2392 = 0.26431758938496000000000000000000e-1 * t2584;
  t1758 = -t3152 + t3096 - t2392;
  t3453 = t1758 - t3925;
  t4087 = -t2413 - 0.81354094419858e-4 * t2576;
  t2929 = t3097 - t4087;
  t1700 = t2300 + t2929;
  t1797 = t2973 * t3757;
  t4101 = -t1700 * t2586 - t1797;
  t4100 = -t1907 + t1852;
  t4095 = -t2267 * t2591 - t2714;
  t2212 = t2585 * t2451;
  t4093 = t2212 - t3916;
  t4092 = t4226 * t2585 + 0.17282e-1;
  t4091 = -t2295 + t3866;
  t3685 = 0.25527100084200000000000000000000e-2 * t2583 - 0.10320550495200000000000000000000e-2 * t2590;
  t2833 = -0.11198654185125000000000000000000e-1 + t3214;
  t4085 = -t2417 + t2833;
  t2460 = 0.16724826617837780000000000000000e-2 * t2594;
  t2133 = -t2460 - 0.988270895904e-3 * t2587;
  t3513 = 0.2392e-2 * t2583;
  t2517 = 0.682e-3 + t3513;
  t3510 = 0.1482e-2 * t2590;
  t3325 = t2517 + t3510;
  t4081 = -0.436e-3 - t4167;
  t2551 = 0.4784e-2 * t2583;
  t3509 = 0.2964e-2 * t2590;
  t4079 = t2551 + t3509;
  t3119 = 0.49096519673609460000000000000000e-2 * t2593;
  t3002 = t2594 * t3119;
  t3194 = 0.49096519673609460000000000000000e-2 * t2585;
  t4078 = t2587 * t3194 - t2592 * t3002;
  t2526 = 0.4978e-2 * t2576;
  t2847 = -0.4978e-2 * t2569 + t2526 + 0.3424e-2 * t3802;
  t1782 = -t3033 + t3691;
  t2879 = -t2526 - 0.1712e-2 * t3802 - 0.5644e-2;
  t4077 = -t1651 + t4144;
  t2027 = 0.47840000000000000000000000000000e-2 * t2583 + 0.29640000000000000000000000000000e-2 * t2590;
  t2047 = -0.48888264403680000000000000000000e-2 * t2583 + 0.19765417918080000000000000000000e-2 * t2590;
  t4074 = t3651 + t4160;
  t1567 = t1589 * t2577;
  t4064 = -t3650 - t1567;
  t1294 = t2882 - 0.28801560650267140000000000000000e-2 - t4064;
  t4072 = t1294 * t2578 + t4228;
  t4067 = -t3620 - t3815;
  t2250 = t2470 * t2592;
  t4066 = -t3065 * t3791 - t2250;
  t3639 = t3681 * t3764;
  t3724 = t3639 - t3866;
  t1669 = -t3850 - t4178;
  t3318 = 0.1644487577369270e-2 * t2586;
  t4063 = t1669 * t3751 + t3318;
  t4062 = 0.2e1 * t3620 + t4164;
  t1826 = t4084 * t2593;
  t3902 = t2997 * t2586;
  t4058 = -t3902 + t1826;
  t4057 = -0.45033756566424900000000000000000e-2 * t3761 - t3911;
  t3913 = t1897 * t2593;
  t4056 = t1884 * t2586 + t3913;
  t3903 = t2997 * t2585;
  t3915 = t1897 * t2584;
  t1541 = t3915 - 0.12908973617152500000000000000000e-1 + t3903;
  t1870 = t2321 + t2182 + 0.3122837745659893e-2;
  t4055 = t1870 * t2570 - t4188;
  t2086 = 0.18713819462921000000000000000000e-3 + t3207;
  t1997 = t2086 * t2584;
  t2201 = t2584 * t3158;
  t3535 = t1647 - t2201 - t1997;
  t1432 = 0.3030488946654060e-2 + t3535;
  t4053 = t1432 * t2578 + t4098 + 0.2390110552949070e-2;
  t4052 = -0.1e1 * t2569 + t2576;
  t4051 = 0.1e1 * t4192 + t2788;
  t3086 = -0.1e1 * t3832 + t2531;
  t2048 = -0.41065000000000000000000000000000e-1 * t2592 + 0.11953000000000000000000000000000e-1 * t2585;
  t3858 = t2048 * t2587;
  t4050 = -0.1e1 * t3858 - t4278;
  t4049 = 0.1e1 * t3952 - t3911;
  t3080 = -t1654 + t4064;
  t3313 = 0.735522e0 * t2524 - t4199;
  t3425 = 0.8676525e-3 * t2585;
  t2509 = -0.374176e-3 + t3425;
  t2280 = t2509 * t2593;
  t3314 = 0.735522e0 * t2280 - 0.735522e0 * t3425;
  t3185 = 0.13609823097337500000000000000000e-1 * t2586;
  t4043 = t3185 + t4141;
  t2800 = -t3156 + t3219;
  t4041 = t2584 * t4156 - t2591 * t2800;
  t3138 = 0.16724826617837780000000000000000e-2 * t2591;
  t3660 = 0.88e-1 * t2584;
  t2523 = 0.384e0 + t3660;
  t3396 = 0.7735484874e-2 * t2523;
  t2853 = -t3138 + t3396;
  t3366 = 0.6381775021050e-3 * t2593;
  t4040 = -t2586 * t2853 - t3366;
  t4039 = 0.988270895904e-3 * t2586;
  t3365 = 0.1200936784896e-2 * t2593;
  t2962 = 0.988270895904e-3 + t3365;
  t1646 = t1673 * t2591;
  t3894 = t1947 * t2584;
  t3246 = -0.3030488946654060e-2 + t3894;
  t1462 = t1646 + t3246;
  t3979 = t1462 * t2578;
  t4036 = t3979 - 0.2390110552949070e-2;
  t3181 = 0.63817750210500000000000000000000e-3 * t2587;
  t3756 = t2592 * t2594;
  t1784 = -t2088 * t3756 - t3181;
  t3240 = 0.7902174366315040000000000000000e-3 * t2576;
  t4035 = t1784 * t2590 + (t3240 + t2835) * t3756;
  t3490 = 0.60149e-1 * t2593;
  t3491 = 0.14117e-1 * t2593;
  t3500 = 0.60149e-1 * t2586;
  t3501 = 0.14117e-1 * t2586;
  t4033 = t2584 * (t2592 * t3500 - t3491) - t2591 * (t2592 * t3501 + t3490);
  t4032 = t2585 * (0.41065e-1 * t2587 + t3378) - t2592 * t2946;
  t4030 = 0.50000000000000000000000000000000e0 * t2571;
  t4029 = 0.50000000000000000000000000000000e0 * t2578;
  t3123 = 0.50000000000000000000000000000000e0 * t2592;
  t2399 = 0.56786982094425000000000000000000e-2 * t2586;
  t3091 = t2399 - 0.21751134959804000000000000000000e-1;
  t4028 = t3908 - 0.10771188545559324000000000000000e-1;
  t2098 = 0.21751134959804000000000000000000e-1 * t2584 - 0.46305794820080000000000000000000e-2;
  t4025 = 0.26431758938496000000000000000000e-1 - t2399;
  t3686 = 0.11881704766464000000000000000000e-1 * t2590 + 0.48037471395840000000000000000000e-2 * t2583;
  t1913 = -0.25339016093952000000000000000000e0 - t3686;
  t4021 = -0.2e1 * t2584;
  t4020 = -0.2e1 * t2585;
  t2572 = t2586 ^ 2;
  t4019 = -t2572 / 0.2e1;
  t4018 = t2572 / 0.2e1;
  t2573 = t2587 ^ 2;
  t4017 = t2573 / 0.2e1;
  t2574 = t2588 ^ 2;
  t4016 = t2574 / 0.2e1;
  t4015 = t2579 / 0.2e1;
  t2580 = t2594 ^ 2;
  t4014 = t2580 / 0.2e1;
  t4012 = -t2584 / 0.2e1;
  t4011 = t2585 / 0.2e1;
  t4010 = -t2586 / 0.2e1;
  t4009 = t2586 / 0.2e1;
  t4008 = -t2587 / 0.2e1;
  t4007 = t2587 / 0.2e1;
  t4006 = -t2588 / 0.2e1;
  t4005 = t2588 / 0.2e1;
  t4004 = t2591 / 0.2e1;
  t4003 = t2592 / 0.2e1;
  t4002 = t2593 / 0.2e1;
  t4001 = -t2594 / 0.2e1;
  t4000 = t2594 / 0.2e1;
  t2603 = q_dot(1);
  t3235 = 0.9683775114084920000000000000000e-2 * t2583;
  t2131 = -0.11008587194880000000000000000000e-2 - t3235;
  t1672 = t2131 * t2590 + t4227;
  t3673 = -0.25527100084200000000000000000000e-2 * t2590 - 0.10320550495200000000000000000000e-2 * t2583;
  t1912 = -0.54439292389350000000000000000000e-1 + t3673;
  t1494 = t1672 * t2585 + t1912;
  t2053 = 0.48888264403680000000000000000000e-2 * t2590 + 0.19765417918080000000000000000000e-2 * t2583;
  t1889 = t2053 + 0.10425949330324000000000000000000e0;
  t1370 = t1494 * t2586 + t1889;
  t1765 = t1862 - 0.6060977893308120e-2;
  t1617 = t1765 * t2585 - 0.22714792837770000000000000000000e-1 * t2584 + 0.48357317375400000000000000000000e-2;
  t3199 = 0.43502269919608000000000000000000e-1 * t2584;
  t2097 = -0.92611589640160000000000000000000e-2 + t3199;
  t1242 = t1370 * t2591 + t1617 * t2586 + t2097;
  t1827 = t1888 * t2584;
  t1736 = t1827 + 0.10572703575398400000000000000000e0;
  t1658 = t1736 * t2586 - 0.11357396418885000000000000000000e-1;
  t1911 = -0.42894239060600000000000000000000e-1 - t2047;
  t1857 = t1911 * t2585;
  t1607 = -t3236 + t2932;
  t1299 = t1607 * t2577 + 0.5760312130053428000000000000000e-2 + t4074;
  t1713 = -t2318 - t2181 + t2299 - 0.4979107553197860000000000000000e-3;
  t1908 = 0.22397308370250000000000000000000e-1 - t3685;
  t2411 = 0.27228906756480000000000000000000e-2 * t2590;
  t1910 = -0.12058866005175110000000000000000e-1 - t2411 - t2357;
  t2314 = 0.96837751140849200000000000000000e-2 * t2576;
  t3250 = t1299 * t2578 + t1713 * t2577 + 0.45033756566424900000000000000000e-2 * t2571 + t1908 * t2585 + t1910 * t2570 + t1913 * t2584 + t2314 + t2179 - 0.10872259100413549980000000000000e1;
  t1069 = t1242 * t2592 + t1658 * t2591 + t1857 + t3921 - 0.25817947234305000000000000000000e-1 + t3250 * t2586;
  t1497 = t1674 * t2585 + t1894;
  t1473 = t1497 * t2591;
  t1307 = t1473 - t4256;
  t3723 = t3846 - t2362;
  t2934 = t2323 - 0.57804776249276620000000000000000e-2 + t3723;
  t1588 = -t2300 + t2934;
  t3732 = t1588 * t2577 + t3650;
  t1093 = t1307 * t2592 - t2317 + 0.53887119947770573000000000000000e0 + t3732 + t4072;
  t2933 = 0.11560955249855324000000000000000e-1 + t3524;
  t1593 = -t2318 + t2933;
  t1448 = t1593 * t2584 - t2993;
  t1353 = t1448 * t2586 + t4187;
  t1213 = t1353 * t2591 + (-0.1e1 * t3930 + t1762) * t2586 - t2099;
  t1668 = -0.58269960219413400000000000000000e-3 + t3523;
  t1490 = t1668 * t2584 - t1891;
  t3466 = t1490 * t2585 - t3101 + t4216;
  t1105 = t1213 * t2592 + t2586 * t3466 - t4144;
  t3078 = t3970 + 0.12569364734109380000000000000000e-2 + t4074;
  t1249 = t2585 * t3078 - t2994;
  t1900 = -0.37427638925842000000000000000000e-3 + t3676;
  t1434 = t1900 * t2584 + t3103;
  t3920 = t1894 * t2585;
  t1488 = t1668 - t3920;
  t1108 = t1249 * t2592 + t1434 * t2578 + t1488 * t2591 - t1584;
  t3252 = t1498 * t2585 + t4111 - t4216;
  t1127 = -0.88047764582400000000000000000000e0 + t3252 * t2586;
  t2096 = -t3208 + 0.54457813512960000000000000000000e-2;
  t1594 = -0.96305836223205680000000000000000e-2 * t2576 + t2096 * t2590 + 0.53191491764352000000000000000000e-4 * t2569 + 0.22017174389760000000000000000000e-2 * t2583 + 0.23121910499710648000000000000000e-1;
  t1449 = t1594 * t2584 - t1913;
  t1902 = -0.13379861294270224000000000000000e-1 * t2590 + 0.43868728512658560000000000000000e-2 * t2583 - 0.44088275061402520000000000000000e-1;
  t1276 = t1902 * t2577 + t1449 * t2591 + 0.10572703575398400000000000000000e0 * t2584 + 0.17936986422585684000000000000000e-1 - t2034;
  t3144 = 0.48037471395840000000000000000000e-2 * t2590;
  t3687 = 0.11881704766464000000000000000000e-1 * t2583 - t3144;
  t1489 = t4268 - 0.95593081660407480000000000000000e-1 + t3687;
  t2975 = t1924 * t2585 - 0.22714792837770000000000000000000e-1;
  t1132 = t1276 * t2592 - t2975 * t2591 + t1489 * t2585 + t1912 * t2584 - 0.55505629074184340000000000000000e0;
  t1731 = t1762 * t2585;
  t1792 = t1888 * t3814;
  t1170 = -t4298 + t1792 + t1450 * t3791 - t1731 + 0.3288975154738540e-2;
  t1586 = t2318 + t2935;
  t1447 = t1586 * t2584 + t2993;
  t1477 = t1653 * t2585 + t2994;
  t1493 = t1674 + t3920;
  t3928 = t1889 * t2584;
  t1542 = -t3912 - t3928 - 0.11683352511943460000000000000000e1;
  t1613 = t3683 + t4028;
  t3133 = 0.43502269919608000000000000000000e-1 * t2591;
  t1678 = -t3133 + t3928 + 0.20699436005309600000000000000000e0;
  t1685 = -t1731 + 0.3288975154738540000000000000000e-2;
  t1738 = t3921 + 0.28391278634449500000000000000000e0;
  t1744 = t1857 - 0.12056561435880000000000000000000e0;
  t1798 = t1896 * t3751;
  t3118 = 0.56786982094425000000000000000000e-2 * t2593;
  t3003 = t2591 * t3118;
  t3774 = t2588 * t2595;
  t3565 = t3774 / 0.2e1;
  t3594 = t2587 * t3757;
  t3787 = t2586 * t2593;
  t3662 = -0.2e1 * t3787;
  t3780 = t2587 * t2594;
  t3927 = t1889 * t2591;
  t949 = ((t1093 * t3662 + ((t1448 * t2591 + t3452) * t2592 + t3466) * t2579 - 0.1e1 * t1105 * t2586 + (0.10572703575398400000000000000000e0 * t2586 - 0.11357396418885000000000000000000e-1) * t3751 + 0.2e1 * t1613 * t3787 + t1738 * t2593) * t2580 + (-0.1e1 * t1108 * t2586 - 0.1e1 * t1798 * t2592 + (t1490 * t2592 + t1685 + (t1447 * t2591 + t3930) * t2585) * t2593) * t3780 - 0.1e1 * t1678 * t2586 + (t2097 + t3927) * t3757 + t1744 * t2593) * t4016 + ((t1132 * t3662 + ((t1494 * t2591 + t1617) * t2592 + t1736 * t2591 + t3250) * t2579 - 0.1e1 * t1069 * t2586 - t1681 * t3757 + (t3133 + t1542) * t2593) * t2594 - 0.1e1 * t1170 * t3784 + (t2585 * t3265 + t1477) * t3594 + t2587 * t1493 * t3751 + t4190 * t3781) * t3565 + t3252 * t3577 + (t1127 * t2581 - t1651 - t3912 + 0.79961440050675000000000000000000e0) * t4010 + t3003 + (-0.1e1 * t3921 - 0.47307790556449500000000000000000e0) * t4002 + (-0.1e1 * t1081 * t2586 + 0.94582559610000000000000000000000e-1) * t2593 * t2581;
  t3998 = t949 * t2603;
  t1208 = (t1477 + (-0.1e1 * t3651 - t3970) * t2585) * t2586 + t1911;
  t3919 = t1894 * t2586;
  t1351 = t1447 + t3919;
  t1216 = t1351 * t2591 + t2099 * t2586 - t3452;
  t1297 = 0.6284682367054690000000000000000e-3 + t3266;
  t3421 = -0.1e1 * t3916 + t1490;
  t1304 = t2586 * t3421 + t2994;
  t1312 = -0.4533121716787550000000000000000e-3 + t3528 + t3732;
  t1611 = t1889 * t2586 + t4187;
  t1394 = t1611 * t2591 + t2097 * t2586 - t2099;
  t1423 = t2578 * t1440;
  t1625 = t1673 * t3764;
  t3759 = t2592 * t2587;
  t3597 = t2586 * t3759;
  t3416 = t2585 * t3597;
  t3661 = -0.2e1 * t3761;
  t3468 = t2586 * t3661;
  t3539 = t1295 * t3661 - t4057;
  t3589 = t2591 * t3759;
  t3593 = t2587 * t3747;
  t3644 = t1896 * t3764;
  t3668 = t2571 - t2578;
  t3782 = t2578 * t2587;
  t3804 = t2581 * t2586;
  t3817 = t2571 * t1440;
  t1352 = t1447 * t2586 + t1894;
  t3987 = t1352 * t2591;
  t3989 = t1277 * t2585;
  t952 = ((t1423 - 0.1e1 * t3817 - (t2579 - 0.1e1 * t2593) * t3911) * t2580 + t4270 + ((-0.1e1 * t1307 * t2579 - 0.1e1 * t1213 * t2593) * t2580 + (-0.1e1 * t1249 * t2593 - 0.1e1 * t1304) * t3780 - 0.1e1 * t1394) * t2585 + (((-0.1e1 * t3918 - 0.1e1 * t2099) * t2593 + t3987 + t2099) * t3780 + (t1440 * t2579 * t2580 + t3078 * t3593) * t2592 + (((-0.2e1 * t1294 - 0.45033756566424900000000000000000e-2) * t2579 - 0.2e1 * t1312 + 0.65959876213732140000000000000000e-2) * t2580 - 0.2e1 * t1434 * t3593) * t2585 + (t3421 * t2593 * t2580 + (t3930 - 0.1e1 * t1762) * t3780 + t1911) * t2586) * t2592) * t4016 + (((-0.1e1 * t1276 * t2585 + (t1489 - 0.1e1 * t3900) * t2592) * t2579 + (t1299 * t3468 + (t1672 * t2591 + t1765) * t4128 - 0.1e1 * t1242 * t2585 + (0.90067513132849800000000000000000e-2 * t2585 + t1908) * t3760 + t1911 * t2592) * t2593 - 0.1e1 * t1216 * t2585 + t3644 - t2994 * t3760 + t1496 * t2592) * t2594 + (0.1e1 * t4289 * t2585 + (-0.1e1 * t3452 + t3981) * t2592) * t3781 + 0.2e1 * t1441 * t3416 + t1296 * t2586 * t3782 - 0.1e1 * t1208 * t3785 + (-0.1e1 * t1889 + t3919) * t3589 + t2099 * t3597 - 0.1e1 * t2097 * t3759) * t3565 + ((t1739 * t2592 + t1625) * t2592 - 0.1e1 * t1306 * t2585 + t3539) * t3577 + ((-0.1e1 * t3989 + t4298) * t3804 + t4049) * t4002 + (t1296 * t3661 - 0.1e1 * t1441 * t3668) * t4013 - 0.1e1 * t1297 * t3761 + (t4029 - t4030) * (t1646 + t1739);
  t3997 = t952 * t2603;
  t3726 = -0.2e1 * t3651 - t3132;
  t3969 = t1603 * t2577;
  t1226 = (-t1450 * t2584 + t3726 + t3969) * t2592;
  t2952 = t2591 * (-0.2e1 * t1591 + 0.62456754913197860000000000000000e-2);
  t2837 = 0.1e1 * t3926 + t2584 * t2952;
  t1310 = -t3925 + t2837;
  t1303 = t1310 * t2578;
  t1361 = t1493 * t2586 - t1889 * t2585;
  t1466 = -t3916 - t3955;
  t1442 = t1466 * t3761;
  t3186 = 0.11357396418885000000000000000000e-1 * t2586;
  t1655 = t1827 + 0.52863517876992000000000000000000e-1 * t2572 - t3186;
  t1677 = -t1742 + 0.43502269919608000000000000000000e-1 * t2586;
  t3663 = -0.2e1 * t3796;
  t3346 = t1588 * t3663 - t3450;
  t3401 = 0.2e1 * t1899 * t3796 + t1303 + t3907 - t3925;
  t3590 = t2585 * t3765;
  t3413 = t2584 * t3590;
  t3464 = -t1495 * t2592 - t1737;
  t3556 = t3761 / 0.2e1;
  t3563 = -t3765 / 0.2e1;
  t3623 = t2578 * t3784;
  t3625 = t2577 * t3789;
  t3813 = t2577 * t2586;
  t3652 = t1888 * t3813;
  t3664 = -0.1e1 * t2577 + t2570;
  t3727 = t1674 * t3791 + t3918;
  t3798 = t2584 * t2587;
  t3812 = t2577 * t2592;
  t3929 = t1888 * t2591;
  t3931 = t1888 * t2570;
  t3956 = t1673 * t2584;
  t3978 = t1497 * t2584;
  t953 = (((t1302 + (-t3978 - t4181) * t2592 + t3346) * t2579 + ((-0.1e1 * t1353 * t2584 - t2451) * t2592 + (t1593 * t3812 - 0.1e1 * t4217 - t3918 + ((0.52863517876992000000000000000000e-1 + 0.2e1 * t1827) * t2592 + t1668 * t2585) * t2591) * t2586) * t2593 + t3346 * t2578 + t1442 + t1593 * t3663 + t3930 - t1655 * t2584 + t2572 * t3907 + t1894 * t3765) * t2580 + (((t1900 * t2591 + t4268) * t2578 + (t1792 + (-0.1e1 * t3931 - t2902) * t2585) * t2592 - t1488 * t2584 - t4093) * t2593 + (t1668 * t2591 + t3917) * t3760 - 0.2e1 * t1888 * t3413 + t1586 * t3625 - t1352 * t3793 - t3132 * t3789 + t2212) * t3780 + (t3199 + t3927) * t2593 + (-t1611 * t2584 + t2586 * t3133 - t2451) * t2592 + t3346) * t4016 + ((((t1594 * t2577 - 0.1e1 * t1449 * t2584) * t2592 + t2975 * t2584 + ((t1902 * t4021 + 0.10572703575398400000000000000000e0) * t2592 + t1667 * t2585 + t1912) * t2591) * t2579 + ((t3930 - 0.1e1 * t3931 + (-0.2e1 * t1607 + 0.12491350982639572000000000000000e-1) * t3796) * t4128 + (-t1370 * t2584 + t2975 * t3765 + t3133) * t2592 + t1713 * t2586 * t3663 + t3652 - t1658 * t2584 + (t1910 * t4022 + t1913) * t3765 + t3918) * t2593 + (-t1351 * t2584 + t1586 * t2577 + t2451 * t2586 + t3726) * t2592 - t1677 * t2584 - t1889 * t3765 + t3727) * t2594 + ((t1675 * t2591 + t3917) * t2592 + (t3969 - t3132 + (-0.2e1 * t3929 - 0.1e1 * t1450) * t2584) * t2585) * t3781 + t4277 * t3623 + (t1888 * t3664 + t2902) * t3416 - t1361 * t3798 + t4093 * t3784 - t3133 * t3785) * t3565 + (t4181 * t2592 + (-0.2e1 * t1712 * t2591 + t3464) * t2584 + t3401) * t3577 + (-t1698 + (-t1675 * t3791 + t1226 + t3918 + t4217) * t3804) * t4002 + ((-t3930 + t2902 + t3931) * t2578 - t4277 * t3761) * t4013 + t1303 / 0.2e1 + (t3916 - t3956) * t3556 + (-0.52863517876992000000000000000000e-1 + t3186) * t4012 + t1894 * t3563 - t3907 / 0.2e1;
  t3996 = t953 * t2603;
  t1472 = t1496 * t2585;
  t1004 = t1132 * t2579 + t1069 * t2593 + t1216 * t2592 + t1677 * t2591 + t1542 * t2586 + t1472 + t3921 + 0.72089127222315021200000000000000e0;
  t1403 = t1440 * t3761;
  t1008 = -0.61633316391764946000000000000000e0 + t1093 * t2579 + t1105 * t2593 + t1312 * t2578 + t1403 + t1593 * t2577 + t1655 * t2591 + t1613 * t2572 + t1738 * t2586 + 0.32979938106866070000000000000000e-2 * t2571 + t2182 - t3695;
  t1040 = t1108 * t2593 + t1304 * t2592 + t1685 * t2586 + t1999 + 0.2438248419014880000000000000000e-3 + (t3652 + t3987) * t2585;
  t2765 = t1170 * t2593 + t1208 * t2592 + t1361 * t2591 - 0.26594038206575168000000000000000e-1 - 0.1e1 * t2097 * t2585;
  t3016 = 0.50000000000000000000000000000000e0 * t3774;
  t954 = -t1004 * t2587 * t3016 + 0.50000000000000000000000000000000e0 * (-0.1e1 * t2573 + t2580) * t2574 * t1040 + (-0.10000000000000000000000000000000e1 * t1008 * t2587 * t2574 + (-t1441 * t4128 + t1584 * t2586 + t2765) * t3016) * t2594;
  t3995 = t954 * t2603;
  t2774 = t1961 + t2029;
  t1325 = (t2774 - t3976) * t2592;
  t3688 = -t2325 + t2416;
  t1628 = (t2091 + t3143) * t2583 + t3688;
  t1597 = t1628 * t2577;
  t1459 = t1597 - t3615;
  t1779 = t2911 + t3226;
  t1349 = t1779 + t1459;
  t1340 = t1349 * t2578;
  t3142 = 0.63217394930520320000000000000000e-2 * t2590;
  t3873 = t2034 * t2584;
  t1467 = (t2314 - t2411 + (t3142 - 0.1e1 * t2084) * t2583) * t2591 + t3873;
  t3707 = -t2583 * t3142 + t2411;
  t1634 = t2084 * t2583 - t2314 + t3707;
  t1778 = t2177 + t3697;
  t1748 = t1779 * t2577;
  t1953 = t2038 * t2570;
  t3690 = t2324 - t3615;
  t2924 = t1340 + t1748 + t1953 + t3690 + t3876 + t4091 - t4303;
  t3140 = 0.19367550228169840000000000000000e-1 * t2590;
  t3165 = 0.27521467987200000000000000000000e-3 * t2590;
  t3303 = -t1961 + t3976;
  t3640 = t3681 * t3799;
  t3409 = -t3640 / 0.2e1;
  t3537 = -t1918 - t4295;
  t3612 = t2584 * t3784;
  t3870 = t3681 * t2591;
  t958 = (((t2177 + t4069 + t4110) * t2579 + ((-t3870 + (-0.1e1 * t2029 + t3303) * t2586) * t2592 + t4076 * t3590 + t4295 * t2586 + t3866) * t2593 + t3531 * t2572 + t3640 + t3527 - t3262 + t3738) * t2580 + ((t1467 * t2578 - t3684 * t2592 + ((t1595 + 0.1e1 * t1922 + t1778) * t2592 - t3870) * t2585 - t4235) * t2593 + ((-t4286 + t3869) * t2586 + t3684) * t2592 + t3676 * t3625 + (-t2586 * t4275 + t3681) * t3791 + t2029 * t3789) * t3780 + t2047 * t3753 + (t2047 * t2586 - t3681) * t3764 + t2053 * t3789 + t3866 + t4069) * t4016 + (((((0.13379861294270224000000000000000e-1 * t2583 + 0.43868728512658560000000000000000e-2 * t2590) * t2577 + ((-t2319 + 0.22017174389760000000000000000000e-2 * t2590) * t2584 + t3144 + ((t3140 - 0.1e1 * t2096) * t2584 - 0.11881704766464000000000000000000e-1) * t2583) * t2591 + t3676) * t2592 + t2034 * t3791 + (t1634 * t2584 + t3686) * t2585 + t3685 * t2584) * t2579 + (t2047 * t3764 + t2053 * t2585 + t1960 + ((t1778 - t3262) * t2578 + ((-0.9683775114084920000000000000000e-2 * t2576 - 0.1e1 * t2131 * t2583 + t3707) * t2585 + t3685) * t3764 + t1778 * t2577 + t3673 * t2585 + (t2351 - t3157) * t2570 - t2583 * t3140 + t2319 - 0.31608697465260160000000000000000e-2 * t2569 + (-0.1e1 * t2034 * t3761 + t3676 * t2591 + t3687) * t2584) * t2586) * t2593 + ((t2586 * t3681 - t4275) * t2591 + t2774) * t2592 + (-t2047 * t2584 - t3866) * t2586 + t3537) * t2594 + (-t4274 * t2592 + (t4252 - t3976 + t2029) * t2585) * t3781 + (t1634 * t2591 - t3873) * t3623 + (((-0.1e1 * t1778 + t3262) * t2585 + t3684) * t2586 + t2053) * t3759 + ((t2585 * t3681 + t1629) * t2586 - t2047 * t2585) * t3783 + t4076 * t3612) * t3565 + (-t2177 + t2924) * t3577 + ((t2585 * t4274 + t1325 + t1960) * t3804 + t3724) * t4002 + ((-t2295 + t3262 + t3706) * t2578 + t1467 * t3761 + t1779) * t4013 + t1340 / 0.2e1 - t4235 * t3556 + t3409 - t3876 / 0.2e1 - t2360 + t3165;
  t3994 = t958 * t2603;
  t3946 = t1766 * t2584;
  t1314 = -0.3030488946654060e-2 * t2585 + t1471 + t3946 + 0.24178658687700000000000000000000e-2;
  t1083 = t1314 * t2592 + t2840 + t4183;
  t3992 = t1083 * t2586;
  t1987 = t3162 - t2268;
  t3883 = t1987 * t2591;
  t1546 = -0.1e1 * t3883 + t4254;
  t2805 = -t3156 - 0.1e1 * t2264 - t4067;
  t1264 = t1546 * t2592 + t2585 * t2805 - 0.8641e-2;
  t3991 = t1264 * t2593;
  t1461 = -t1937 + t4229;
  t1986 = t2033 + 0.682e-3;
  t3885 = t1986 * t2591;
  t2729 = t3885 + t4220;
  t1265 = 0.15592e-1 + t1461 * t2592 + t2729 * t2585;
  t3990 = t1265 * t2579;
  t3986 = t1414 * t2571;
  t3985 = t1421 * t2591;
  t3116 = 0.26431758938496000000000000000000e-1 * t2593;
  t2735 = -t3116 + t3091;
  t2838 = t2861 * t2587;
  t1443 = -t2594 * t2735 + t2838;
  t3982 = t1443 * t2584;
  t2884 = t2982 + t3723;
  t1604 = t2884 - 0.57804776249276620000000000000000e-2;
  t1569 = t1604 * t2584;
  t3000 = t1569 + t2094;
  t1451 = -t3146 + t3000;
  t3980 = t1451 * t2591;
  t3968 = t1604 * t2577;
  t1596 = t1628 * t2584;
  t3857 = t2048 * t2594;
  t1638 = t3857 - t4210;
  t3963 = t1638 * t2589;
  t3962 = t1638 * t2596;
  t1643 = t1669 * t2584;
  t3960 = t1669 * t2591;
  t3959 = t1670 * t2584;
  t3958 = t1670 * t2592;
  t3954 = t1679 * t2593;
  t1749 = t1783 * t2578;
  t3938 = t1821 * t2570;
  t1844 = t1884 * t2593;
  t3934 = t4084 * t2586;
  t1886 = -t2091 + 0.29704261916160000000000000000000e-2 * t2584;
  t3933 = t1886 * t2590;
  t3923 = t2973 * t2587;
  t1893 = -t2801 + 0.44842466056464210000000000000000e-2;
  t3922 = t1893 * t2586;
  t1843 = t1893 * t2593;
  t1895 = t2414 - t2087;
  t1832 = t1895 * t2593;
  t3914 = t1897 * t2585;
  t1853 = t1897 * t2591;
  t2103 = -t3118 + 0.56786982094425000000000000000000e-2;
  t3183 = 0.26431758938496000000000000000000e-1 * t2586;
  t1904 = t2103 - t3183;
  t3910 = t1904 * t2584;
  t3909 = t1904 * t2591;
  t3906 = t1907 * t2586;
  t3905 = t1907 * t2587;
  t3904 = t1907 * t2592;
  t1859 = t1907 * t2593;
  t3901 = t2997 * t2593;
  t3898 = t1925 * t2585;
  t3897 = t1925 * t2586;
  t3896 = t1925 * t2591;
  t3895 = t1925 * t2594;
  t3892 = t1948 * t2584;
  t3891 = t1948 * t2594;
  t3887 = t2822 * t2587;
  t3886 = t1986 * t2584;
  t3884 = t1987 * t2584;
  t3488 = 0.27454e-1 * t2594;
  t2014 = t2286 * t2587 + t3488;
  t3879 = t2014 * t2589;
  t3058 = t2014 * t2596;
  t3875 = t4172 * t2584;
  t3874 = t4172 * t2593;
  t3872 = t3679 * t2592;
  t3871 = t4174 * t2591;
  t3868 = t3682 * t2591;
  t3865 = t2044 * t2585;
  t3863 = t2801 * t2585;
  t3861 = t2801 * t2592;
  t3860 = t2801 * t2594;
  t3859 = t2046 * t2593;
  t3114 = 0.24444132201840000000000000000000e-2 * t2594;
  t2051 = -t3114 - t2405;
  t3856 = t2051 * t2590;
  t2082 = t2463 * t2585;
  t3854 = t2082 * t2587;
  t3845 = t2093 * t2586;
  t3843 = t2098 * t2586;
  t3842 = t2098 * t2587;
  t3841 = t2098 * t2594;
  t3202 = 0.56786982094425000000000000000000e-2 * t2584;
  t2100 = -0.12089329343850000000000000000000e-2 + t3202;
  t3840 = t2100 * t2586;
  t3839 = t2100 * t2587;
  t3838 = t2100 * t2592;
  t2000 = t2100 * t2594;
  t2002 = t2107 * t2586;
  t3837 = t2835 * t2594;
  t3836 = t2115 * t2587;
  t2006 = t2115 * t2594;
  t2011 = t2130 * t2587;
  t3834 = t2130 * t2594;
  t3833 = t2133 * t2593;
  t2293 = -0.316e0 * t2593 + t3522 - 0.384e0;
  t3829 = t2293 * t2591;
  t3827 = t2466 * t2596;
  t3822 = t2470 * t2585;
  t3819 = t2570 * t2586;
  t3818 = t2570 * t2593;
  t3816 = t2571 * t2587;
  t3811 = t2577 * t2593;
  t3810 = t2578 * t2579;
  t3809 = t2578 * t2584;
  t3807 = t2578 * t2593;
  t3806 = t2579 * t2594;
  t3805 = t2579 * t2595;
  t3803 = t2583 * t2585;
  t3801 = t2583 * t2595;
  t3800 = t2584 * t2583;
  t3797 = t2584 * t2588;
  t3795 = t2584 * t2592;
  t3794 = t2584 * t2595;
  t3790 = t2585 * t2595;
  t3776 = t2588 * t2593;
  t3771 = t2589 * t2594;
  t3770 = t2589 * t2595;
  t3769 = t2590 * t2585;
  t3768 = t2590 * t2587;
  t3766 = t2590 * t2595;
  t3763 = t2591 * t2594;
  t3762 = t2591 * t2595;
  t3755 = t2592 * t2595;
  t3752 = t2593 * t2585;
  t2919 = t2594 * t2464;
  t3750 = t2594 * t2584;
  t3745 = t2595 * t2587;
  t3744 = t2595 * t2593;
  t3740 = t2596 * t2594;
  t3739 = t2596 * t2595;
  t2230 = t2591 * t3154;
  t1558 = t2230 - t4095;
  t3734 = t1558 * t3761 + t4245;
  t3733 = t1604 * t3753 - t1844;
  t1571 = t1605 * t2577;
  t3731 = t1571 - 0.2e1 * t3650;
  t3728 = t1670 * t3753 + t1832;
  t2003 = t2107 * t2593;
  t2235 = t2593 * t3163;
  t3722 = t2003 + t2235;
  t2170 = t2587 * t2350;
  t2227 = t2587 * t2414;
  t3721 = t2170 - t2227;
  t2226 = t2587 * t3160;
  t3178 = 0.24444132201840000000000000000000e-2 * t2587;
  t3720 = t2583 * t3178 - t2226;
  t2220 = t2587 * t3146;
  t3719 = t2587 * t3215 + t2220;
  t2228 = t2587 * t3152;
  t3718 = t2405 * t2583 - t2228;
  t3717 = t2044 * t2587;
  t2222 = t2587 * t2418;
  t3716 = -t2583 * t3181 + t2222;
  t3139 = 0.54835910640823200000000000000000e-3 * t2591;
  t3703 = t2130 * t2591 + t2590 * t3139;
  t2504 = t2587 * t3518;
  t3388 = t2593 * t3518;
  t3702 = -t2587 * t3388 + t2504;
  t2500 = t2588 * t3520;
  t3701 = -t2586 * t3387 + t2500;
  t3675 = t2399 - t3116;
  t3674 = -t3188 - t1843;
  t3667 = t2579 - t2572;
  t3666 = t2579 + t2578;
  t3665 = -0.1e1 * t2571 + t2578;
  t3659 = t4170 * t3747;
  t3656 = t1809 * t3787;
  t3655 = t1870 * t3819;
  t3649 = t2973 * t3799;
  t3648 = t2973 * t3760;
  t3647 = t2577 * t3923;
  t1796 = t2973 * t3811;
  t3646 = t2594 * t3925;
  t3643 = t1925 * t3789;
  t3642 = t1925 * t3760;
  t3641 = t1925 * t3751;
  t3637 = t2591 * t3851;
  t2289 = 0.218e-3 - t4073;
  t3633 = t2289 * t3796;
  t3632 = t2464 * t3746;
  t3631 = t2464 * t3779;
  t3630 = t2465 * t3743;
  t3629 = t3065 * t3797;
  t3627 = t2570 * t3789;
  t3626 = t2570 * t3748;
  t3624 = t2577 * t3747;
  t3622 = t2578 * t3746;
  t3617 = t1988 * t3796;
  t3616 = t2027 * t3796;
  t3613 = t2584 * t3761;
  t3611 = t2584 * t3791;
  t3610 = t2584 * t3746;
  t3608 = t2024 * t3791;
  t3607 = t2033 * t3814;
  t3606 = t2585 * t3748;
  t3605 = t2585 * t3746;
  t3098 = -t2180 + 0.33106000000000000000000000000000e-1;
  t1184 = -t2340 + t3098 + t4297;
  t3604 = t1184 * t3787;
  t3603 = t2586 * t3772;
  t3602 = t2586 * t3741;
  t3601 = t2589 * t3748;
  t3600 = t2584 * t3760;
  t3599 = t2586 * t3757;
  t3598 = t2586 * t3744;
  t3596 = t2586 * t3742;
  t3595 = t2586 * t3773;
  t3592 = t2585 * t3778;
  t3591 = t2589 * t3747;
  t3588 = t2584 * t3751;
  t3587 = t2591 * t3746;
  t3586 = t2593 * t3773;
  t3585 = t2584 * t3747;
  t3584 = t2593 * t3742;
  t3583 = -t4283 / 0.2e1;
  t3582 = t1782 * t2570 / 0.2e1;
  t3581 = t2577 * t4019;
  t3580 = t2572 * t3999;
  t3579 = -t3814 / 0.2e1;
  t3576 = t3805 / 0.2e1;
  t3575 = t3801 / 0.2e1;
  t3574 = t3794 / 0.2e1;
  t3573 = -t3792 / 0.2e1;
  t3572 = t3790 / 0.2e1;
  t3571 = t3787 / 0.2e1;
  t3570 = t3780 / 0.2e1;
  t3569 = t2580 * t4005;
  t3568 = -t3779 / 0.2e1;
  t3567 = -t3777 / 0.2e1;
  t3566 = -t3776 / 0.2e1;
  t3564 = t3766 / 0.2e1;
  t3562 = t3765 / 0.2e1;
  t3561 = t2591 * t4006;
  t3560 = -t3764 / 0.2e1;
  t3559 = t3764 / 0.2e1;
  t3558 = t3763 / 0.2e1;
  t3557 = t3762 / 0.2e1;
  t3555 = t3757 / 0.2e1;
  t3554 = t3756 / 0.2e1;
  t3553 = t3755 / 0.2e1;
  t3552 = -t3752 / 0.2e1;
  t3551 = t3752 / 0.2e1;
  t3550 = -t3750 / 0.2e1;
  t3549 = t3749 / 0.2e1;
  t3548 = -t3748 / 0.2e1;
  t3546 = t3747 / 0.2e1;
  t3545 = -t3746 / 0.2e1;
  t3544 = t3746 / 0.2e1;
  t3543 = -t3745 / 0.2e1;
  t3542 = t3745 / 0.2e1;
  t3541 = t3744 / 0.2e1;
  t3538 = -t2578 * t3080 + t2362 - t3132;
  t3536 = t1596 - t2030;
  t2459 = 0.21751134959804000000000000000000e-1 * t2594;
  t3038 = t2587 * t2325;
  t3532 = t2088 * t3768 + t2459 - t3038;
  t3529 = t4155 * t2587;
  t2176 = 0.99560000000000000000000000000000e-2 * t3802;
  t1777 = t2176 + t3698;
  t3525 = -t3517 * t3784 + t3702;
  t3515 = 0.1712e-2 * t2569;
  t3505 = 0.3495e-2 * t2596;
  t3499 = 0.61597e-1 * t2586;
  t3485 = 0.735522e0 * t2583;
  t3484 = 0.735522e0 * t2584;
  t3483 = 0.735522e0 * t2586;
  t3482 = 0.104419e0 * t2588;
  t3479 = 0.646926e0 * t2589;
  t3478 = 0.735522e0 * t2590;
  t3477 = 0.735522e0 * t2591;
  t3476 = 0.735522e0 * t2592;
  t3470 = 0.646926e0 * t2596;
  t3469 = -0.2e1 * t3611;
  t3467 = t1297 * t2585 - t4084;
  t1865 = t2088 * t2584 + 0.12009367848960000000000000000000e-2;
  t1464 = t1865 * t2590 - t2584 * t2835 - t2087 - t2216;
  t2841 = t1464 + t3896;
  t3465 = t1484 - t3889;
  t3463 = t1650 - 0.82500000000000000000000000000000e-1 + t4293;
  t1590 = -t2323 + t2930;
  t3462 = t1590 * t2577 - t3650;
  t3461 = -t1884 + t1569;
  t3459 = t1779 + t1597;
  t3456 = t1665 + t3889;
  t3316 = t2201 - 0.3030488946654060e-2;
  t1734 = t3316 + t1997;
  t3455 = t1734 + t1646;
  t3454 = t2591 * t3158 - t3956;
  t1770 = t2088 * t2594 + t2592 * t3181;
  t2244 = t2594 * t2325;
  t3451 = t1770 * t2590 - t2244;
  t2001 = t2100 * t2593;
  t3448 = -t2591 * t3913 - t2001;
  t1863 = t1925 * t2592;
  t3447 = t1884 * t2585 - t1863;
  t3443 = -t2835 + t3850;
  t3434 = 0.1632768e-2 * t2586;
  t3433 = 0.4038528e-2 * t2586;
  t3432 = 0.1225946e1 * t2589;
  t3431 = 0.1666555e1 * t2589;
  t3430 = 0.3587895e1 * t2589;
  t3429 = 0.1225946e1 * t2596;
  t3428 = 0.1666555e1 * t2596;
  t3427 = 0.3228604e1 * t2596;
  t3426 = 0.3587895e1 * t2596;
  t3424 = t1569 - 0.1e1 * t1884;
  t3423 = -t4283 - 0.1e1 * t2040;
  t3422 = -t3925 - 0.1e1 * t1893;
  t3420 = t1870 * t3588;
  t3419 = t2973 * t3585;
  t3418 = t2973 * t3611;
  t3415 = t2592 * t3606;
  t3414 = t2592 * t3605;
  t3412 = t2587 * t3598;
  t3411 = t2593 * t3582;
  t3410 = -t3655 / 0.2e1;
  t3407 = t2578 * t3544;
  t3406 = t2591 * t3549;
  t3405 = t2591 * t3551;
  t3404 = t2579 * t3542;
  t3403 = t2585 * t3543;
  t3402 = t2592 * t3542;
  t3399 = t2593 * t3389 + t3701 + 0.384e0 * t3779;
  t3397 = 0.3127439544e-2 * t2523;
  t3394 = 0.7735484874e-2 * t2583;
  t3392 = 0.3127439544e-2 * t2592;
  t3391 = 0.7735484874e-2 * t2592;
  t3390 = t2587 * t3521;
  t3384 = 0.9956e-2 * t3802;
  t3382 = -0.1e1 * t3959 - 0.1e1 * t1895;
  t3381 = 0.275214679872e-3 * t2591;
  t3380 = 0.680722668912e-3 * t2591;
  t3376 = 0.2580137623800e-3 * t2584;
  t3375 = 0.6381775021050e-3 * t2584;
  t3374 = 0.2580137623800e-3 * t2586;
  t3372 = 0.2580137623800e-3 * t2587;
  t3371 = 0.6381775021050e-3 * t2587;
  t3370 = 0.2444413220184e-2 * t2587;
  t3369 = 0.2580137623800e-3 * t2591;
  t3368 = 0.6381775021050e-3 * t2591;
  t3367 = 0.2580137623800e-3 * t2593;
  t3364 = 0.2970426191616e-2 * t2593;
  t3363 = 0.2580137623800e-3 * t2594;
  t3362 = 0.6381775021050e-3 * t2594;
  t1983 = t2292 * t3503 + 0.374176e-3 * t2586;
  t3358 = t1983 * t3477;
  t1989 = -t2292 * t3512 + 0.925496e-3 * t2586;
  t3357 = t1989 * t3477;
  t3355 = t2472 * t3470;
  t3354 = t2587 * t3483;
  t3353 = t2594 * t3483;
  t3351 = t2591 * t3476;
  t3350 = 0.2e1 * t3413;
  t3347 = -t1414 * t3661 + t1549 * t2571 - t1537;
  t3345 = t2093 * t2587 + t2000 + t2222;
  t3344 = t2006 - t2011 + t3856;
  t3343 = 0.13297872941088e-4 * t2569;
  t3339 = t1322 * t3428;
  t2284 = t2465 - 0.316e0;
  t1724 = t2284 * t2595 - t4213;
  t3333 = t1724 * t3426;
  t3331 = t4151 * t3427;
  t3330 = t2585 * t3434;
  t3329 = t2585 * t3433;
  t1822 = -0.5644000000000000000000000000000e-2 - t3714;
  t1416 = 0.5410000000000000000000000000000e-2 + t1822 * t2577 - t3617 - t3714;
  t1810 = -0.34240000000000000000000000000000e-2 * t2576 + t2176 - 0.29200000000000000000000000000000e-2;
  t2964 = -0.1364e-2 - t2027;
  t1548 = t1810 * t2591 + t2584 * t2964 + 0.8468e-2;
  t1194 = t1416 * t3761 + t1548 * t2578 + t3534 - 0.6898e-2;
  t1547 = -0.1e1 * t3885 - t4220;
  t2745 = t1547 * t2592 + t4185 * t2585 - 0.17282e-1;
  t1097 = 0.95220000000000000000000000000000e-2 + t1194 * t2593 + t2745 * t2586;
  t1460 = -t2800 + 0.4146e-2 + t4067;
  t1515 = t3879 - t4281;
  t1519 = t1694 * t2589 + t3058;
  t1661 = t2589 * t2818 - t3827;
  t2688 = 0.83327750000000000000000000000000e0 * t2588 * t4051;
  t1185 = -0.33106000000000000000000000000000e-1 + t3713 - t4297;
  t1776 = t1823 * t2577;
  t2737 = t1185 * t2579 + t1265 * t3787 + t1776 - t3035 - t3238 + t3617 + t3736 + 0.31784000000000000000000000000000e-1;
  t2786 = 0.36776100000000000000000000000000e0 * t2588 * (-t2587 * t3463 - t2594 * t4170);
  t2819 = 0.17939475000000000000000000000000e1 * t2588 * t2014;
  t2957 = -t2919 + t4210;
  t2979 = t4254 * t2585 - 0.19192000000000000000000000000000e-1;
  t3040 = 0.16143020000000000000000000000000e1 * t4129;
  t3105 = 0.17939475000000000000000000000000e1 * t2596;
  t3041 = t1724 * t3105;
  t3168 = 0.17939475000000000000000000000000e1 * t2589;
  t3042 = t1724 * t3168;
  t3171 = 0.61297300000000000000000000000000e0 * t2589;
  t3045 = t1517 * t3171;
  t3046 = t1322 * t3106;
  t3047 = t1322 * t3169;
  t1511 = -t2007 * t2588 - t1692 - t2565;
  t1311 = t1511 * t2589 + t3962;
  t3048 = t1311 * t3108;
  t1657 = t4278 + t3858;
  t1455 = t1657 * t2595 + (0.316e0 + t3086) * t2588;
  t1286 = t1455 * t2596 + t3963;
  t3049 = t1286 * t3171;
  t1308 = t3954 + 0.31600000000000000000000000000000e0 - t4294;
  t2988 = -t2587 * t4170 + t2594 * t3463;
  t1118 = t1308 * t2595 + t2588 * t2988;
  t3053 = t1118 * t3109;
  t3055 = t1118 * t3172;
  t2611 = t1097 * t2587 * t3775 - 0.1e1 * (-t1704 * t3591 - 0.1e1 * t1576 * t3773 + t4044 * t3601 - 0.825e-1 * t3771) * t3055 + (t2957 * t4305 - 0.1e1 * t4051 * t3046 - 0.1e1 * t2014 * t3041 - 0.1e1 * (-t3948 + (-0.1e1 * t3972 - 0.1e1 * t1636) * t2587) * t3053) * t3770 + (-0.1e1 * t1084 * t2786 - 0.1e1 * t1661 * t3040 + t4050 * t4305 - 0.1e1 * t1214 * t2688 + t3046 * t4304 + t1519 * t2819 + t2015 * t3041 - 0.1e1 * (-0.1e1 * t4241 + t4191) * t3053 - (-0.1e1 * t3059 * t2596 - 0.1e1 * t2466 * t3770) * t4146) * t2596 + ((-0.1e1 * t4210 + t3857) * t3045 - 0.1e1 * (t3971 + (-0.1e1 * t4267 - 0.1e1 * t4045) * t2587) * t3055 - 0.1e1 * (-0.1e1 * (-0.1e1 * t2155 + t3516) * t2587 - 0.1e1 * t2788) * t3047) * t3739 + (t1987 * t3406 + (t3991 - 0.12805000000000000000000000000000e-1 + t4196) * t4007 + t3058 * t3042) * t2595 + (-0.1e1 * t1112 * t2786 + t3040 * t4292 + t4050 * t3045 - 0.1e1 * t1211 * t2688 + t3047 * t4304 + t1515 * t2819 + t2015 * t3042 + (-0.1e1 * t2466 * t3739 + t3059 * t2589) * t4146) * t2589 - 0.50000000000000000000000000000000e0 * (t1460 * t2592 + t2979 + t3604 + t3990) * t3743 + ((t2587 * t4007 - 0.50000000000000000000000000000000e0 * t2580) * t2737 - 0.1e1 * t2957 * t3048 + (-0.1e1 * t4210 + t2919) * t3049) * t2588;
  t1606 = -t3236 + t2933;
  t1452 = t1606 * t2584 - t2993;
  t1278 = t1452 * t2591 + t3452;
  t1139 = t1278 * t2592 + t1495 * t2584 - t4234;
  t2897 = t1651 + t1571 + t2341 - t3650 - 0.53661951164938448500000000000000e0;
  t1219 = t2897 + t3712;
  t3249 = t3453 + t3980;
  t1222 = t2594 * t3249 - 0.21447119530300000000000000000000e-1 * t2587 + t3720;
  t1492 = t1644 + t1897;
  t1347 = t1492 * t2584 + t1895 * t2585 + 0.36044563611157510600000000000000e0;
  t1771 = t1948 * t2585 - 0.56786982094425000000000000000000e-2;
  t1521 = t1771 * t2594 - t1907 * t3785;
  t2839 = t1272 + t3978 + t4234;
  t2715 = t2586 * t2839 + t4077;
  t2860 = t1403 + t2413 + t3538 - t4028;
  t2870 = -t2392 + t3422;
  t3193 = 0.56786982094425000000000000000000e-2 * t2585;
  t1803 = t3193 - t1948;
  t2927 = t1803 * t2584 + t4036;
  t3089 = t2451 - 0.28391278634449500000000000000000e0;
  t2992 = -t3921 + t3089;
  t3174 = 0.21751134959804000000000000000000e-1 * t2587;
  t3029 = t2584 * t3174;
  t3175 = 0.13297019103287584000000000000000e-1 * t2587;
  t3177 = 0.46305794820080000000000000000000e-2 * t2587;
  t2223 = t2587 * t3164;
  t1560 = t1907 * t2594 - t2223 + (-0.93569097314605e-4 - t3212) * t2587;
  t1252 = t1560 * t2591 + t3841 + (-0.23898270415101870000000000000000e-1 + t1643) * t2587 + t3721;
  t3112 = 0.56786982094425000000000000000000e-2 * t2594;
  t3288 = t2585 * t3424;
  t1363 = t2587 * t3288 - t3112;
  t3305 = t1252 * t2592 + t1363 * t2591;
  t1544 = t1897 * t2594 + t3785 * t3924;
  t2875 = t1567 + t1654;
  t1188 = t1544 * t2591 + t2000 + (t2585 * t2875 + 0.55993270925625000000000000000000e-2) * t2587 + t3716;
  t2775 = -t2835 + t3914;
  t1382 = t2587 * t2775 + t3532;
  t3306 = t1188 * t2592 + t1382 * t2591;
  t2647 = (t1139 * t3806 + ((t1541 + t3992) * t2594 + (t2585 * t2870 + 0.1644487577369270e-2) * t2587 + t3305) * t2593 + (-t1540 * t2594 + (-0.12089329343850000000000000000000e-2 * t2585 + t2927) * t2587 + t3306) * t2586 + t1222 * t2592 + t1521 * t2591 + t1347 * t2594 - 0.1e1 * t2585 * t3029 + t2585 * t3177 - 0.1e1 * t3175) * t3999 + t2992 * t3568 + t2715 * t3566 + (t1219 * t2579 + t2572 * t2860 - t2182 + 0.68731045565809253900000000000000e0 - t2982) * t4006;
  t938 = t2611 + t2647;
  t1813 = -0.56440000000000000000000000000000e-2 - t3714;
  t2111 = -0.68200000000000000000000000000000e-3 - t3211;
  t2966 = t2111 - t3154;
  t1520 = t1813 * t3795 + t2585 * t2966;
  t1883 = -0.21800000000000000000000000000000e-3 + t4174;
  t1528 = t1883 * t3809 + t2726 * t3761;
  t1280 = t1520 * t3787 + t1528 * t2579;
  t2134 = 0.2920e-2 + 0.3424e-2 * t2576 - t3384;
  t1610 = t2134 * t2578 + t3613 * t4081 + t2880;
  t3068 = -t3510 - t3513;
  t2290 = -t3068 + 0.682e-3;
  t2766 = t2290 * t2592 + t2879 * t3793;
  t1339 = t1610 * t2593 + t2586 * t2766;
  t1707 = 0.42340000000000000000000000000000e-2 - t2200 + t2111 * t2584;
  t1358 = t1707 * t3761 + t1812 * t2578 - t2316 + t3098;
  t1892 = 0.82920000000000000000000000000000e-2 - t4174;
  t2692 = 0.45800000000000000000000000000000e-3 - t2714;
  t1404 = t1892 * t2592 - 0.15592000000000000000000000000000e-1 + t2692 * t2585;
  t1930 = -0.5410e-2 + t3714;
  t2493 = t2584 * t3509;
  t2515 = 0.1364e-2 + t2551;
  t1979 = t2515 * t2584 + t2493 - 0.8468e-2;
  t1480 = 0.6898e-2 + t1979 * t2578 + t1930 * t3761 + (-t3510 - 0.1e1 * t2517) * t2584;
  t2949 = t2289 * t3666 + t4081;
  t1485 = t2584 * t2949 - t2880 * t3761;
  t1901 = -0.43600000000000000000000000000000e-3 + t2795;
  t1516 = t1809 * t3810 + t1901 * t3599;
  t1929 = -0.2822e-2 + t3710;
  t2136 = -0.2822e-2 - 0.2489e-2 * t2576 - 0.856e-3 * t3802;
  t1554 = t1929 * t2578 + t2136 * t2579 - t2879;
  t1928 = 0.5644e-2 + t3714;
  t1641 = t1928 * t3757 + t2586 * t4081;
  t1923 = t2584 * t2880 - 0.458e-3;
  t1927 = 0.2705e-2 + t3710;
  t1982 = t2584 * t3325 - 0.4234e-2;
  t950 = t2466 * t2595 * t3435 + (t2504 + (-0.1e1 * t4126 - 0.1e1 * t3488) * t2595) * t3436 + ((-0.1e1 * t2919 + (-0.1e1 * t4117 - 0.1e1 * t2528) * t2587) * t2595 + t3702) * t3438 + ((t2788 + (-0.1e1 * t4130 - t2791) * t2587) * t2595 + t3525) * t3440 - 0.1e1 * ((t4263 + (-t2586 * t2783 + t2593 * t2699) * t2587) * t2595 + t3525) * t3486 + (t1358 * t2579 + t1404 * t3787 - t3710 - 0.31784e-1 - 0.1e1 * t1927 * t2578 - 0.1e1 * t1982 * t3761 + (t1280 - 0.1e1 * t1485) * t2591 + (t1516 - 0.1e1 * t1554) * t2577) * t3780 + 0.3228604e1 * t4255 * t4151 * t4129 + t4171 * (-t3390 + (t3488 + t4126) * t2588) + t4158 * (-t3390 + (t2587 * t4080 + t2919) * t2588) + t4157 * (-t2587 * t2500 + t3390 + (t2788 + (-t2791 - t2155) * t2587) * t2588) + t4169 * (-t3390 + (-t4263 + (t3888 + t4290) * t2587) * t2588) + (-0.50000000000000000000000000000000e0 * t2573 + t4014) * (-0.9522e-2 + t1641 * t3814 + t1339 * t2591 + t1480 * t2593 + (t1923 * t2592 + t4092) * t2586);
  t3323 = t2602 * t950 - t2603 * t938;
  t2474 = t2586 * t3480;
  t1545 = t3883 - t4254;
  t2742 = t1545 * t2592 + t4184 * t2585 + 0.8641e-2;
  t2981 = t2587 * t3086;
  t3242 = t4230 * t2587;
  t3275 = t2586 * t3482 + t2588 * t3506 - t3630;
  t2614 = (t4044 * t3586 - 0.1e1 * t1483 * t2586 + (t1704 * t3776 + (-0.1e1 * t3889 - 0.1e1 * t3950) * t3743) * t2596) * t3055 + (t1679 * t3584 - 0.1e1 * t1369 * t2586 + (t1525 * t3776 + (t3954 - 0.1e1 * t3973) * t3743) * t2589) * t3053 + ((t2588 * t4231 + t4261) * t2589 + t2596 * t3242) * t3046 + ((-0.1e1 * t4261 + (-0.1e1 * t2155 - 0.1e1 * t4214) * t2588) * t2596 + t2589 * t3242) * t3047 - ((t2285 * t3776 + t2474 + t4264) * t2589 + t2596 * t2981) * t3044 - 0.1e1 * t1265 * t3412 + (-0.1e1 * t4196 + t2742 * t2593) * t4005 + ((-0.2e1 * t1185 * t3787 + (t2579 - 0.1e1 * t2572) * t1265) * t3778 + (-0.1e1 * t1264 * t2586 + t4195) * t2595) * t4000 + (-0.1e1 * t1194 * t2586 + t2745 * t2593) * t3569 - 0.1e1 * ((-0.1e1 * t4264 + (-0.1e1 * t2528 - 0.1e1 * t3831) * t2588) * t2596 + t2589 * t2981) * t3045 - 0.1e1 * ((-0.1e1 * t2588 * t3060 + t3630) * t2596 - 0.1e1 * t2465 * t3773) * t3042 - 0.1e1 * (-0.1e1 * t2465 * t3742 + t2589 * t3275) * t3041 + (-0.1e1 * t1515 * t3168 - 0.1e1 * t1519 * t3105) * (t2465 * t3775 + t2595 * t3060) + t4176 * (-0.1e1 * t4231 * t2595 + t3775 * t4230) + (t2572 * t3543 + t3404) * t1184 + t4175 * ((-t4293 - 0.1e1 * t1650) * t2595 + (-0.1e1 * t4294 + t3954) * t3775) + (t3048 + 0.1e1 * t3049) * (t2007 * t3775 - t2595 * t4080);
  t2287 = -0.3344965323567556e-2 * t2583 - 0.187138194629210e-3;
  t2166 = 0.4841887557042460e-2 * t2583 + 0.55042935974400000000000000000000e-3;
  t2926 = t2166 * t2590 - 0.1580434873263008e-2 * t2576 + 0.582699602194134e-3 - t2356;
  t2779 = 0.1e1 * t3419 + t2926 * t2587;
  t3317 = 0.1096718212816464e-2 * t2590;
  t3270 = t2587 * t3317;
  t2678 = t1589 * t3624 + t1654 * t3747 + t2287 * t3798 - t2584 * t3270 + t2591 * t2779 + 0.3030488946654060e-2 * t2587;
  t2750 = t2594 * t4084 - t3839;
  t2752 = t1464 * t2594 - t3842;
  t3014 = t2587 * t3148;
  t1556 = -t3014 + t3836 + t3895;
  t2221 = t2587 * t3155;
  t2925 = t1556 * t2586 + t2221 + (-t2092 - t3913) * t2587;
  t2657 = t2099 * t2587 + t2585 * t2678 + t2586 * t2752 + t2591 * t2925 + t2593 * t2750;
  t1324 = t1421 * t2586 + t3913;
  t2832 = -0.21447119530300000000000000000000e-1 + t2353;
  t2969 = -t2832 + t3160;
  t2836 = -0.1e1 * t1758 * t2594 + t2969 * t2587;
  t2672 = t1324 * t3763 + t2593 * t3345 + t4085 * t2587 + (t2836 + t3646) * t2586;
  t2768 = -t2584 * t2996 + 0.29682175996164750000000000000000e0;
  t2703 = t2587 * t2768 - 0.16444875773692700000000000000000e-2 * t2594;
  t2762 = 0.2502297872941088e-2 * t2576 + t2298 + 0.790217436631504e-3 * t3802 - 0.6002993810686607e-2;
  t2704 = t2587 * t2762 + t3455 * t3747;
  t1709 = -0.23901105529490700000000000000000e-2 - t4098;
  t2767 = t4186 * t2584 - 0.50330438027992300000000000000000e0;
  t2732 = t1709 * t2594 + t2587 * t2767;
  t1564 = t1670 * t2594 + t3174;
  t2751 = t1564 * t2593 + (0.52863517876992000000000000000000e-1 - t2399) * t2587;
  t2856 = t2591 * t3735 - t2593 * t3453 - t3840;
  t2874 = t2586 * t3467 + t2593 * t2841;
  t2907 = t3462 - 0.22516878283212450000000000000000e-2;
  t2878 = t2587 * t2907;
  t2617 = 0.82224378868463500000000000000000e-3 * t3776 + (-0.1e1 * t2105 * t3798 + t2571 * t2878 + t2578 * t2704 + t2585 * t2672 + t2586 * t2703 + t2591 * t2751 + t2592 * t2657 + t2593 * t2732 + t4221 * t2587) * t3999 + t2874 * t3567 + t2856 * t3573 + t1669 * t2586 * t3561 + t4053 * t3568;
  t940 = t2614 - t2617;
  t2790 = t2822 * t2595;
  t951 = t3275 * t3436 + (t2474 - 0.1e1 * t3743 * t4118 + (t2588 * t3061 + t2594 * t3471) * t2593 + t3701) * t3438 + ((t2463 * t3743 + t2792) * t2593 + (t2463 * t2588 - t2594 * t2790) * t2586 + t3399) * t3440 - 0.1e1 * ((-t2588 * t2699 + t2783 * t3743) * t2593 + (t2588 * t2783 + t2699 * t3743) * t2586 + t3399) * t3486 + ((t1901 * t2592 * t3667 - 0.2e1 * t2578 * t3656) * t2577 + (t1520 * t3667 + t1528 * t3662) * t2591 + t1358 * t3662 + t3667 * t1404) * t4017 + (-0.1e1 * t1928 * t3760 * t3814 + t1923 * t3757 + (-0.1e1 * t1610 * t2591 - 0.1e1 * t1480) * t2586 + (t2591 * t2766 + t3814 * t4081 + t4092) * t2593) * t3570 + 0.2e1 * (-0.1e1 * t2136 * t2577 - 0.1e1 * t3633) * t2580 * t3571 - 0.1e1 * t2577 * t3656 - 0.1e1 * t2586 * t1883 * t3588 + t4171 * ((-t2594 * t3482 + 0.5317e-1 * t2595) * t2593 + (t3473 + 0.5317e-1 * t3775) * t2586) + t4158 * ((t2285 * t2595 - t3352) * t2593 + (t2285 * t3775 + t3471) * t2586) + t4157 * (-t2594 * t2497 - t3388 + (t2283 * t3775 - t2790) * t2593 + (-t2283 * t2595 - t2594 * t2792) * t2586) + t4169 * ((t2595 * t2693 - t3775 * t4044) * t2593 + (t2595 * t4044 + t2693 * t3775) * t2586);
  t3322 = t2602 * t951 + t2603 * t940;
  t1267 = -0.1e1 * t1461 * t2585 + t2729 * t2592;
  t1577 = -t3725 - t4212;
  t2055 = 0.41065000000000000000000000000000e-1 * t2585 + 0.11953000000000000000000000000000e-1 * t2592;
  t3256 = t2055 * t2594 - t2464 * t3781;
  t3257 = t2594 * t2822 + t3243 * t3781;
  t3309 = t3412 / 0.2e1;
  t2615 = ((t1577 * t2594 - t3276 * t3781) * t2589 + ((t1577 * t2587 + t3276 * t3747) * t2595 + t3276 * t3779) * t2596) * t3055 + ((-t3659 + (t2480 - 0.1e1 * t4065) * t2587) * t3770 + (-0.1e1 * t2480 + t4065) * t3740 - (t3584 + t3603) * t4170) * t3053 + (t3632 - t4244) * t3048 + (((t1931 - t3887) * t2595 + t4115) * t2589 + t3257 * t2596) * t3046 + (((-0.1e1 * t1931 + t3887) * t2595 - 0.1e1 * t4115) * t2596 + t3257 * t2589) * t3047 - ((-t4042 * t2595 - 0.1e1 * t3631) * t2589 + t3256 * t2596) * t3044 + ((-0.1e1 * t3986 + t1397 + 0.2e1 * t1518) * t2593 + (-0.1e1 * t1545 * t2585 + t4184 * t2592) * t2586) * t4005 + ((t1267 * t3787 + t2579 * t3347 + t3347) * t3778 + (-0.1e1 * t1546 * t2585 + t2805 * t2592) * t3744 + 0.2e1 * t1549 * t3414 + t1414 * t3622 - 0.1e1 * t3746 * t3986) * t4000 + ((-0.2e1 * t1548 * t3761 + t3665 * t1416) * t2593 + (-0.1e1 * t1547 * t2585 + t4185 * t2592) * t2586) * t3569 - 0.1e1 * (t4244 - 0.1e1 * t3632) * t3049 + t4254 * t3402 + t1267 * t3404 + t1460 * t3403 - 0.1e1 * (((t2055 * t2587 + t2132) * t2595 + t3631) * t2596 + t3256 * t2589) * t3045 + (-0.1e1 * t1549 * t3668 - 0.2e1 * t3609) * t3309 + t1987 * t3543 * t3764 + t4176 * (t1931 * t2588 - t2587 * t2792 - t4198) + t4175 * (t4170 * t3746 + (t2587 * t4099 - t3659) * t2588);
  t3117 = 0.21751134959804000000000000000000e-1 * t2593;
  t2794 = -t3117 + t2399;
  t2734 = t2794 - 0.26431758938496000000000000000000e-1;
  t2720 = t2734 * t2587;
  t1427 = t1669 * t3747 + t2720;
  t2883 = t2997 + t3934;
  t2747 = -t2228 + t1427 * t2584 + (-0.1e1 * t1832 + t2883) * t2594;
  t2831 = 0.46305794820080000000000000000000e-2 - t3188;
  t2776 = -t2831 + t1843;
  t2990 = -0.55993270925625000000000000000000e-2 - t3682;
  t2808 = t1826 + (t1895 + t3959) * t2586 + t2990;
  t2455 = 0.12089329343850000000000000000000e-2 * t2593;
  t3088 = t2455 - 0.12089329343850000000000000000000e-2;
  t2857 = t3088 + t3910 - t3922;
  t2971 = t2094 - t3146;
  t2764 = t1569 - 0.1e1 * t1859 + t1852 + t2971;
  t1228 = -0.1e1 * t1925 * t3747 + t2764 * t2587;
  t1235 = -t2223 - t2011 + (t2593 * t4107 - t4100) * t2594;
  t2905 = t1228 * t2585 + t1235 * t2592 - t2594 * t3649;
  t3260 = t1700 * t2593 - t3648;
  t3070 = t2577 * t3260;
  t1612 = -t3913 + t1897;
  t1287 = t2586 * t3424 + t1612;
  t3081 = t1287 * t2592 - t1795 + t3643;
  t3248 = 0.1e1 * t3901 + t3934 + t2087;
  t3253 = t2592 * t3747 - t3785;
  t2643 = ((t1700 * t3748 + t2973 * t3253) * t2577 + t2905 * t2591 + (t2587 * t3248 + t2594 * t2776 - t2227 + t3982) * t2592 + (t2587 * t2722 + t2747) * t2585 + t1870 * t3626 - t4188 * t3748) * t3999 + t2808 * t3573 + t3070 * t4006 + t3081 * t3561 + t2857 * t3567 + t4055 * t3566;
  t942 = t2615 - t2643;
  t2686 = (t2467 * t2587 + 0.10517e-1 * t3747) * t2592 + (t2467 * t3747 - 0.10517e-1 * t2587) * t2585;
  t2695 = t2586 * t2700;
  t2851 = t2879 * t2586;
  t2920 = t2464 * t2586;
  t2922 = t2593 * t3065;
  t957 = (-0.1e1 * t2588 * t2920 - 0.1e1 * t2595 * t4032) * t3438 + (t2595 * t2686 + t4115) * t3440 - 0.1e1 * (t2588 * t2695 + ((t4211 - 0.1e1 * t3065 * t3747) * t2592 + t4239) * t2595) * t3486 + ((-0.2e1 * t1809 * t2579 * t2592 - 0.1e1 * t1901 * t3787) * t3814 + ((-0.1e1 * t2726 * t3668 - 0.2e1 * t1883 * t3613) * t2579 + (-0.1e1 * t1813 * t3793 + t2966 * t2592) * t3787) * t2591 + (-0.1e1 * t1707 * t3668 + t1812 * t3661) * t2579 + (-0.1e1 * t1892 * t2585 + t2692 * t2592) * t3787) * t4017 + (t1641 * t3812 - 0.1e1 * t2571 * t1928 * t3811 + ((-0.2e1 * t2134 * t3757 - 0.1e1 * t2586 * t2290) * t2585 + (t2593 * t3665 * t4081 + t2592 * t2851) * t2584) * t2591 + (-0.1e1 * t1930 * t3668 + t1979 * t3661) * t2593 - 0.1e1 * t1923 * t3789 + t4226 * t3760) * t3570 + ((-0.1e1 * t1929 * t2577 - 0.1e1 * t1927 - 0.1e1 * t3633) * t4140 + (t4243 - 0.1e1 * t1982) * t3668) * t4014 + t4158 * (t2588 * t4032 - t2595 * t2920) + t4157 * (t2588 * t2686 - t4198) + t4169 * (t2595 * t2695 + ((t2594 * t2922 - t4211) * t2592 - t4239) * t2588);
  t3321 = t2602 * t957 + t2603 * t942;
  t1254 = (0.2e1 * t3617 - 0.1e1 * t2570 * t1823 + t1776) * t2592 + (-0.1e1 * t3886 + t2713) * t2585;
  t1682 = t2893 * t2585;
  t1683 = t2893 * t2592;
  t1721 = t1887 * t2591 + t3197;
  t3230 = -0.1e1 * t3830 + t3496;
  t1879 = t3230 * t2592;
  t2886 = -0.1e1 * t3932 + t3131;
  t2887 = t2463 * t3785;
  t3020 = 0.74100000000000000000000000000000e-3 * t3746;
  t3308 = t2591 * t3403;
  t3310 = t3542 * t3793;
  t2613 = ((t1682 * t2587 + (t1879 * t2593 - 0.1e1 * t3244 * t2586) * t2594) * t3739 + (t2589 * t2783 * t3759 + t3244 * t3741) * t2593 + t1879 * t3602 + t1682 * t3771 + t3244 * t3595) * t3055 + ((t2585 * t3230 * t3773 + t1683 * t3591 + t1721 * t3601) * t2595 + (t1683 * t3742 - 0.1e1 * t3244 * t3772) * t2593 + t2783 * t2585 * t3740 + t1683 * t3603 + t1721 * t3596) * t3053 + (((t1774 - 0.1e1 * t3854) * t2595 + t4114) * t2589 + (t2082 * t2594 + t2587 * t3255) * t2596) * t3046 + (((-0.1e1 * t1774 + t3854) * t2595 - 0.1e1 * t4114) * t2596 + t2082 * t3771 + t2463 * t2592 * t3586 + t2467 * t3595) * t3047 + ((t1558 * t2578 - t4061 * t3761 - 0.1e1 * t3942 + (t2268 - 0.1e1 * t3162) * t2591) * t2593 + (-0.1e1 * t3884 + t4237) * t3760 + t1985 * t3350 + (-0.1e1 * t3625 + t3627) * t1821) * t4005 + (((t3734 + t4062) * t2579 + t1254 * t3787 - 0.2e1 * t3619 + (t2577 - 0.1e1 * t2570) * t1988 + t3734) * t3778 + ((t3884 - 0.1e1 * t4237) * t2592 + t1985 * t3469 + t1821 * t3814 - 0.1e1 * t2585 * t3938) * t3744 + t1558 * t3622 - t4061 * t3414 - 0.1e1 * t4179 * t3610 - 0.1e1 * t3020 * t3767 + t2268 * t3587) * t4000 + (((-0.1e1 * t1810 * t2584 + t2964 * t2591) * t2578 + (t1822 * t3663 + t2570 * t1988 - 0.1e1 * t1937) * t3761 + t1558) * t2593 + (-0.1e1 * t2713 + t3886) * t3760 + t1988 * t3350 + (t3625 - 0.1e1 * t3627) * t1823) * t3569 + t1254 * t3404 + (-0.1e1 * t1775 + 0.2e1 * t3618 + t3938) * t3402 + t1987 * t3310 + (-t4245 + (-0.1e1 * t2230 + t4095) * t3761 - 0.1e1 * t4062) * t3309 + t4179 * t3308 + t4176 * ((t1774 - t2887) * t2588 - t3254 * t2595) + t4175 * ((t1721 * t2593 + t2886 * t3760) * t2595 + t2886 * t3592 + (t1683 * t3747 + t1721 * t3748) * t2588);
  t3124 = 0.26431758938496000000000000000000e-1 * t2592;
  t2696 = t1897 + t3124;
  t3125 = 0.56786982094425000000000000000000e-2 * t2592;
  t2829 = -0.52129746651620000000000000000000e-1 - t3125;
  t2810 = -t3217 + t2829;
  t2780 = t2810 * t2586;
  t2676 = t2780 + t2696;
  t2769 = t2884 - 0.32797153116247448000000000000000e-1;
  t2755 = t2769 * t2593;
  t2243 = t2586 * t3112;
  t3111 = 0.26431758938496000000000000000000e-1 * t2594;
  t2843 = t2593 * t3111 - t2243 + t3532;
  t2682 = (-t2587 * t2835 + t2843) * t2591 + t2594 * t2755;
  t2866 = t2996 + t4056;
  t2743 = t1670 * t2593 + t2585 * t2866 - t3642;
  t2757 = t4035 * t2593;
  t2895 = -t3846 - t4259;
  t2869 = t2895 * t2586;
  t2809 = t2869 + t3909;
  t2967 = t2107 * t2592 - 0.21751134959804000000000000000000e-1;
  t2816 = t2587 * t2967 + t3451;
  t3302 = -t1852 + t1844;
  t2864 = -t2594 * t3302 + t3344;
  t2914 = t2991 * t2593;
  t2970 = t2094 * t2592 + 0.56786982094425000000000000000000e-2;
  t3013 = t2592 * t3146;
  t3231 = 0.5483591064082320000000000000000e-3 * t2594;
  t2056 = -t3178 + t3231;
  t3297 = t2056 * t2590 + t3834;
  t3066 = t3297 + t3836;
  t3176 = 0.56786982094425000000000000000000e-2 * t2587;
  t2461 = 0.54835910640823200000000000000000e-3 * t2594;
  t2052 = -t3178 + t2461;
  t3298 = t2052 * t2590 + t3834;
  t3241 = t3298 * t2586;
  t3261 = t1670 * t3760 + t1925 * t2593;
  t2626 = t2809 * t3573 - t2743 * t3797 / 0.2e1 + t3261 * t3561 + ((t2864 * t2585 + (t2592 * t3066 - t3176) * t2593 + (t2816 - t3837) * t2586) * t2584 + t2682 * t2585 + (t2757 + t3241) * t2591 + ((-t3013 + t2970) * t2584 + (t2914 + t2676) * t2591 + t4154) * t2587) * t3999;
  t945 = t2613 - t2626;
  t2872 = t2288 * t2593;
  t2681 = (-t2586 * t3492 - t2872) * t2591 + (t2592 * t2871 - t3489) * t2584;
  t2684 = -t2887 + ((-t2592 * t3491 + t3500) * t2591 + (t2592 * t3490 + t3501) * t2584) * t2594;
  t959 = (t2588 * t4033 + t2595 * t2684) * t3440 - (t2681 * t2588 + (-t4204 + (-t4238 + (t2288 * t3757 + t3499) * t2584) * t2594) * t2595) * t3486 + (t1516 * t3663 + (t1813 * t3599 + t1883 * t3810) * t2577 - t1280 * t2584 + (t2111 * t2591 - t2230) * t2579 * t3761 - t2586 * t2713 * t3752) * t4017 + (t1641 * t3469 + (t3757 * t4081 + t2851) * t3814 - t1339 * t2584 + ((t2515 + t3509) * t2578 - t3325) * t3751 + t3760 * t4243) * t3570 + (t2591 * t3325 * t3761 - t1485 * t2584 + t1554 * t3663 + t2577 * t2949) * t4014 + t2572 * t3657 + t1883 * t3581 + t2570 * t1883 * t4018 + (t3341 + t3342) * (t2588 * t2684 - t2595 * t4033) + t4169 * (t2681 * t2595 + (t4204 + (t4238 + (-t2592 * t2872 - t3499) * t2584) * t2594) * t2588);
  t3320 = t2602 * t959 + t2603 * t945;
  t1268 = (-0.1e1 * t2027 * t2577 + t1788 * t3796 + t2033) * t2592 + (-0.1e1 * t3871 + t2706) * t2585;
  t1656 = t2024 * t3764 - t2028 * t2585;
  t1718 = t2250 + t3608;
  t1824 = -t3065 * t3764 + t3822;
  t3015 = t2585 * t3162;
  t3037 = t2585 * t3216;
  t3069 = (t1656 * t2593 - t2024 * t3799) * t2594;
  t2612 = ((t1718 * t2587 + (t1824 * t2593 + t4116) * t2594) * t3739 + (-0.1e1 * t1824 * t3773 - 0.1e1 * t2596 * t3629) * t2593 + t1824 * t3602 + t1718 * t3771 - 0.1e1 * t3065 * t2584 * t3595) * t3055 + ((t2587 * t4066 + t3069) * t3770 + (t1656 * t3742 + t2589 * t3629) * t2593 - 0.1e1 * t4066 * t3740 + t1656 * t3603 - 0.1e1 * t2024 * t2584 * t3596) * t3053 + ((-0.1e1 * t4165 * t2578 + t1393 * t3761 + 0.1e1 * t4156 * t2591 + t2800 * t2584) * t2593 + t4041 * t3760 - 0.1e1 * t1789 * t3413 + (t3607 - 0.1e1 * t3037 - 0.1e1 * t3015) * t2586) * t4005 + (((t3737 + t4233) * t2579 + t1268 * t3787 + t1788 * t2577 + t3616 + t2245 - 0.1e1 * t2804 + t3737) * t3778 + (t1789 * t3611 - 0.1e1 * t2592 * t4041 + t3015 + t3037 - 0.1e1 * t3607) * t3744 - 0.1e1 * t4165 * t3622 + t1393 * t3414 + t4156 * t3587 + t3020 * t3800 - 0.1e1 * t3156 * t3610) * t4000 + (((t2795 * t2584 + (0.68480000000000000000000000000000e-2 * t3802 + 0.99560000000000000000000000000000e-2 * t4052) * t2591) * t2578 + (t1777 * t2577 + t1777 - 0.1e1 * t3616) * t3761 - 0.1e1 * t4165) * t2593 + (-0.1e1 * t2706 + t3871) * t3760 - 0.1e1 * t2027 * t3625 + t1788 * t3413 + t2033 * t3789) * t3569 + t1268 * t3404 + (-0.1e1 * t1789 * t3796 + t2033 * t2577 - 0.1e1 * t3162 - 0.1e1 * t3216) * t3402 - 0.1e1 * t2800 * t3308 + (-0.1e1 * t4233 - t3737) * t3309 - 0.1e1 * t4156 * t3310 + t4175 * ((-t1656 * t2586 - t2024 * t3753) * t2595 + ((-t2028 * t2592 - t3608) * t2587 + t3069) * t2588);
  t2717 = -t4040 - 0.6381775021050e-3;
  t3120 = 0.16724826617837780000000000000000e-2 * t2593;
  t3007 = t2584 * t3120;
  t3189 = 0.54835910640823200000000000000000e-3 * t2586;
  t2761 = t2585 * t3189 + t3007;
  t2888 = t3313 - 0.735522e0 * t3330;
  t2673 = t2591 * t2888 + t2592 * t2717 - t2761;
  t2854 = t3139 + t3397;
  t2718 = t2586 * t2854 + t3367 - 0.2580137623800e-3;
  t3121 = 0.54835910640823200000000000000000e-3 * t2593;
  t3008 = t2584 * t3121;
  t3187 = 0.16724826617837780000000000000000e-2 * t2586;
  t2760 = t2585 * t3187 - t3008;
  t2889 = t3314 + 0.735522e0 * t3329;
  t2674 = t2591 * t2889 + t2592 * t2718 - t2760;
  t2824 = -t2890 - 0.2970426191616e-2;
  t2709 = t2587 * t2824 - t2593 * t3231;
  t3179 = 0.16724826617837780000000000000000e-2 * t2587;
  t2848 = -0.988270895904e-3 * t2594 + t3179;
  t3290 = t2594 * t3397;
  t2675 = t2586 * t3363 + t2591 * t2709 - t2593 * t3290 + t2848;
  t2961 = 0.1200936784896e-2 - t3374;
  t2826 = -0.1e1 * t3833 + t2961 * t2587;
  t3289 = t2594 * t3396;
  t2691 = t2586 * t3362 + t2591 * t2826 - t2593 * t3289 + t3671;
  t2702 = -t3229 * t3353 + (t2594 * t2962 - t3179) * t2585;
  t2845 = t2461 + t3370;
  t2738 = t2584 * t2845 - t2585 * t3372;
  t2739 = t2133 * t2584 - t2585 * t3371;
  t2771 = t2509 * t3353 + (-t2594 * t3364 + t3671) * t2585;
  t3285 = t2584 * t3372;
  t2815 = t2585 * t2845 - t3285;
  t3284 = t2584 * t3371;
  t2959 = -t2133 * t2585 + t3284;
  t3137 = 0.49096519673609460000000000000000e-2 * t2591;
  t3011 = t2586 * t3137;
  t3293 = t2587 * t3396;
  t3294 = t2587 * t3397;
  t2616 = ((t2585 * t3293 + t2586 * t2739 + t2591 * t2702 + t2592 * t2691 + t2593 * t2815 + t3285) * t2590 + (t2585 * t3294 + t2586 * t2738 + t2591 * t2771 + t2592 * t2675 + t2593 * t2959 - t3284) * t2583 - t2594 * t3011 + t4078 * t2584) * t3999 + (t2583 * t2674 + t2590 * t2673) * t4006 + 0.24548259836804730000000000000000e-2 * (t3751 - t3600) * t2588;
  t947 = t2612 - t2616;
  t2685 = t2584 * t2922 + t2586 * t2730;
  t968 = -0.1e1 * (t2685 * t2588 - 0.1e1 * t4219 * t2595) * t3486 + ((t1783 * t3810 + t2027 * t3599) * t2577 + ((t2033 * t3809 + t3761 * t4090) * t2579 + (t1777 * t3795 + t2585 * t4174) * t3787) * t2591 + (t3705 * t3761 + t1749 + t1777) * t2579 + (-0.1e1 * t2033 * t2592 - 0.1e1 * t2585 * t2706) * t3787 + t1783) * t4017 + ((-0.1e1 * t1777 * t3757 + t4079 * t2586) * t3814 + (((-0.6848e-2 * t3802 + 0.9956e-2 * t4222) * t2578 + t4079 * t3613 + t2847) * t2593 + (-0.1e1 * t4073 * t2592 + (-0.1e1 * t2527 + t3384 + t3515) * t3793) * t2586) * t2591 + (-0.1e1 * t1777 * t3761 + t4073 * t2584 + t3809 * t4167) * t2593 + t2847 * t3600 + (-0.1e1 * t3513 - 0.1e1 * t3510) * t3789) * t3570 + ((-0.1e1 * t1749 - 0.1e1 * t3384 + t2527 - 0.1e1 * t3515 + (t2491 + 0.856e-3 * t4222) * t2579) * t2577 + (-0.1e1 * t2847 * t3761 + t2493 + (t3068 * t3666 + t2551) * t2584) * t2591 - 0.1e1 * t1749 - 0.1e1 * t4073 * t3613) * t4014 + t1783 * t3581 + t3614 * t4019 + t4169 * (t2588 * t4219 + t2595 * t2685);
  t3319 = t2602 * t968 + t2603 * t947;
  t3315 = 0.3030488946654060e-2 - t3917;
  t1457 = -t1865 * t2583 + t2584 * t4155 - t3146;
  t3312 = (t1457 - t4202) * t2593;
  t3063 = t2590 * t3235;
  t3307 = t1597 - t3639 - t3063 + t3690;
  t1481 = t3893 - t3956;
  t2049 = t3118 + t3183;
  t3301 = -t2049 * t2584 - t3922;
  t3296 = t2104 * t3394;
  t3292 = t2593 * t3397;
  t3291 = t2593 * t3396;
  t3287 = -0.1e1 * t1951 + t3977;
  t3286 = t3874 + t4272;
  t3283 = t2586 * t3372;
  t3282 = t2586 * t3371;
  t3281 = t2587 * t3367;
  t3280 = t2587 * t3366;
  t3279 = t2584 * t3363;
  t3278 = t2584 * t3362;
  t3269 = t1647 + t3315;
  t3267 = -t2029 * t3753 + t2592 * t4257;
  t1946 = 0.6029433002587555e-2 - t3683;
  t3251 = t1946 * t2570 + t4027 + t4072 - t4183;
  t3247 = t1647 + 0.3030488946654060e-2;
  t3245 = t2100 * t2585 - 0.2390110552949070e-2;
  t3237 = 0.2502297872941088000000000000000e-2 * t2576;
  t3234 = 0.5483591064082320000000000000000e-3 * t2587;
  t3232 = 0.5483591064082320000000000000000e-3 * t2591;
  t3228 = 0.50000000000000000000000000000000e0 * t1631;
  t3227 = 0.50000000000000000000000000000000e0 * t2801;
  t3224 = 0.39510871831575200000000000000000e-3 * t2576;
  t3204 = 0.54835910640823200000000000000000e-3 * t2584;
  t3203 = 0.49096519673609460000000000000000e-2 * t2584;
  t3196 = 0.54835910640823200000000000000000e-3 * t2585;
  t3195 = 0.16724826617837780000000000000000e-2 * t2585;
  t3191 = 0.25801376238000000000000000000000e-3 * t2586;
  t3190 = 0.27417955320411600000000000000000e-3 * t2586;
  t3184 = 0.21751134959804000000000000000000e-1 * t2586;
  t3180 = 0.98827089590400000000000000000000e-3 * t2587;
  t3170 = 0.73552200000000000000000000000000e0 * t2589;
  t3167 = 0.32286040000000000000000000000000e1 * t2589;
  t3166 = 0.13611244295754000000000000000000e-3 * t2590;
  t3161 = 0.83624133089188900000000000000000e-3 * t2590;
  t3136 = 0.56786982094425000000000000000000e-2 * t2591;
  t3135 = 0.21751134959804000000000000000000e-1 * t2591;
  t3134 = 0.26431758938496000000000000000000e-1 * t2591;
  t3130 = 0.28244044800000000000000000000000e0 * t2591;
  t3128 = 0.25801376238000000000000000000000e-3 * t2592;
  t3127 = 0.54835910640823200000000000000000e-3 * t2592;
  t3126 = 0.16724826617837780000000000000000e-2 * t2592;
  t3122 = 0.25801376238000000000000000000000e-3 * t2593;
  t3115 = 0.12089329343850000000000000000000e-2 * t2594;
  t3113 = 0.46305794820080000000000000000000e-2 * t2594;
  t3110 = 0.24548259836804730000000000000000e-2 * t2595;
  t3107 = 0.73552200000000000000000000000000e0 * t2596;
  t3104 = 0.32286040000000000000000000000000e1 * t2596;
  t3100 = t3915 + 0.29682175996164750000000000000000e0;
  t3099 = -t1858 - 0.50330438027992300000000000000000e0;
  t3090 = -t3184 + 0.56786982094425000000000000000000e-2;
  t3085 = 0.3507900e-3 * t4249;
  t3084 = 0.8676525e-3 * t4249;
  t3079 = -t1654 + t3264;
  t1866 = t2089 * t2584 - 0.59408523832320000000000000000000e-2;
  t2984 = t1877 + t3236;
  t1420 = t1866 * t2590 + t2584 * t2984 - t2105;
  t1270 = t1420 * t2591 - t3452;
  t1825 = t2085 * t2585 + 0.12763550042100000000000000000000e-2;
  t1696 = t1825 * t2584 + 0.24018735697920000000000000000000e-2 * t2585;
  t2109 = 0.70158000000000000000000000000000e-3 - 0.18509920000000000000000000000000e-2 * t2585;
  t1732 = t2109 * t3485 + 0.5826996021941340000000000000000e-3 * t2585 + 0.27219646194675000000000000000000e-1;
  t3039 = t2584 * t2324;
  t1123 = 0.27752814537092170000000000000000e0 + t1270 * t2592 - t4216 + t1696 * t2590 + t1732 * t2584 + (-t3039 + 0.47796540830203740000000000000000e-1 - t2347) * t2585;
  t1422 = 0.30304889466540600000000000000000e-2 + t3535;
  t2036 = 0.51602752476000000000000000000000e-3 * t2585 + t3213;
  t1007 = (t1422 * t3761 + t3295 + t2105 * t2584 + 0.10771188545559324e-1 + t3538) * t3787 + t1123 * t4019 + (t1123 * t2593 + t2584 * t4187 + t3089) * t4002 - (t2036 * t2590 - t2585 * t2833 + t2897) * t3787 + t4077 * t4010;
  t2601 = q_dot(3);
  t2237 = t2594 * t2418;
  t2618 = ((-0.1e1 * t1646 - 0.1e1 * t1734) * t3781 * t2578 + ((-t1795 * t3783 + (-0.1e1 * t1567 - 0.1e1 * t1654) * t3781 + (-0.1e1 * t3317 + t2287) * t3750) * t2585 + (-0.1e1 * t4084 * t2587 - 0.1e1 * t2000) * t2593 + ((-0.1e1 * t1925 * t2587 + t2006) * t2591 - 0.1e1 * t1464 * t2587 - 0.1e1 * t3841) * t2586) * t2592 + (-0.1e1 * t1324 * t3783 + (t2237 - 0.1e1 * t3839) * t2593 + (t1758 * t2587 - t3647) * t2586) * t2585 + ((-0.1e1 * t1670 * t2587 + t2459) * t2593 - 0.1e1 * t2243) * t2591 - 0.1e1 * t1709 * t3781 + 0.16444875773692700000000000000000e-2 * t3784 - 0.1e1 * t2105 * t3750 + (t2762 * t2578 + ((t2591 * t2926 + 0.3030488946654060e-2) * t2585 + (-0.1e1 * t3913 - 0.1e1 * t2092 + (-0.24444132201840000000000000000000e-2 * t2586 + 0.12763550042100000000000000000000e-2) * t2590) * t2591 + t2099) * t2592 + t2907 * t2571 + (t2586 * t2969 + t4085 + t4134) * t2585 + t3132 + t2767 * t2593 + t2768 * t2586 + t4221) * t2594) * t4005;
  t2654 = (-0.1e1 * t3305 * t2586 + t3306 * t2593 + (t1083 * t2579 - 0.1e1 * t4248 + (-0.2e1 * t1139 * t2593 - 0.1e1 * t1541 - 0.1e1 * t3992) * t2586) * t2594 + (-0.1e1 * t3318 + t2927 * t2593 + (-0.1e1 * t2870 * t2586 - 0.1e1 * t2455) * t2585) * t2587) * t4006 + t2715 * t3544 + (t1219 - 0.1e1 * t2860) * t3598 - 0.50000000000000000000000000000000e0 * t2992 * t3744 - 0.50000000000000000000000000000000e0 * t2839 * t3805;
  t956 = t2618 + t2654;
  t2708 = -t2994 + t4058;
  t2719 = t2585 * t3269 - t2001 + t2099;
  t2723 = -t3913 + t1894;
  t2733 = -t2794 + 0.52863517876992000000000000000000e-1;
  t2999 = t1643 + t2087;
  t1491 = -t2414 + t2999;
  t2756 = (t1491 - t3896) * t2586 + (t2585 * t3079 - t4084) * t2593;
  t2787 = -0.60029938106866070000000000000000e-2 + t3237 + t3711;
  t2865 = t2586 * t3249 + t3448;
  t2944 = t2593 * (-t3917 + t3247);
  t3071 = t3462 - 0.2251687828321245e-2;
  t2632 = (t2578 * t2944 + t2756 * t2592 + t2865 * t2585 + (0.2390110552949070e-2 + t3899) * t2593 + t4063) * t4001 + (t2787 * t2578 + ((t2723 - t3906) * t2591 - t3843 + t2719) * t2592 + t3071 * t2571 + t2708 * t2585 + t2733 * t2591 + t3099 * t2593 + t3100 * t2586 + t3908 - t2413 + t3087) * t4007;
  t1639 = -t2585 * t3246 + t2099;
  t1659 = -t1737 * t2586 + 0.56786982094425000000000000000000e-2;
  t1371 = t1497 * t2586 + t4186;
  t2910 = t1371 * t2591 - t2098;
  t1071 = t2910 * t2592 + t1659 * t2591 + (t1639 * t2592 + t3251) * t2586 - t1541;
  t1138 = t1735 + t1472 + t4111;
  t1794 = t2973 * t3814;
  t1882 = t1948 * t2591;
  t2896 = -t1882 + t1491;
  t2913 = 0.1644487577369270e-2 + (t1758 + t3980) * t2585;
  t1173 = t2592 * t2896 - t1794 + t2913;
  t1478 = t1654 * t2585 + t4084;
  t1486 = t2775 + t4059;
  t1640 = t3245 - t3892;
  t1730 = t2593 * t3418;
  t2666 = (t1138 * t3662 + ((t1639 + t1473) * t2592 - t4218 + t3251) * t2579 - t1071 * t2586 + (-t1897 * t3751 - t2001) * t2592 - t2591 * t3117 + t4248) * t4007 + t1173 * t3548 + (t1730 + (t1589 * t3814 + t1478) * t2593) * t3554 + (t1486 * t2591 + t1640 + t3979) * t3546;
  t964 = t2632 + t2666;
  t3076 = t1007 * t2601 + t2602 * t964 - t2603 * t956;
  t1266 = t1605 * t3663 + t1698 + t3450;
  t1454 = -0.1e1 * t3955 + (-t3158 - 0.1e1 * t2086) * t2591;
  t1030 = (t1454 * t3761 + t4177) * t4018 + ((((t2984 + t3848) * t2577 - t1420 * t2584 + t3726) * t2592 + t4217 - t2324 * t3791 + t1825 * t3767) * t2593 - t3201 + (t1732 * t2593 + t4187) * t2591) * t4009 + t1266 * t4015 - t4161 * t3555;
  t2852 = t2593 * (-t3240 + t3443);
  t2625 = ((((-0.1e1 * t2115 + t3302) * t2587 - 0.1e1 * t3298) * t2585 + (-0.1e1 * t3112 + ((-0.1e1 * t3114 - 0.1e1 * t3234) * t2590 + t2006 - 0.1e1 * t2011) * t2592) * t2593 + t2838 * t2586) * t2584 + (-0.1e1 * t2244 * t2591 + (t2735 * t2591 - 0.1e1 * t2755) * t2587) * t2585 + (t2586 * t3856 + (-0.1e1 * t2130 * t2586 + t2592 * t2852) * t2587) * t2591 + (((-t2592 * t2996 - 0.21751134959804000000000000000000e-1) * t2586 - 0.1e1 * t3013 + t2970) * t2584 + (t3443 * t2585 + (t2991 - 0.1e1 * t3163) * t2593 + t2676) * t2591 + t4154) * t2594) * t2588;
  t2770 = t3968 - t3134 + (0.2e1 * t2973 * t2591 - 0.1e1 * t1451) * t2584;
  t3018 = t2587 * t3135;
  t2637 = (((t1606 * t2577 + t3132) * t2592 + t1471 + ((0.2e1 * t3929 - 0.1e1 * t1452) * t2592 + t1766) * t2584) * t3806 + ((t1735 * t2592 + (0.2e1 * t1714 * t2591 + t3464) * t2584 + t3401) * t3748 + (-0.1e1 * t1560 * t2584 + (t1669 * t2587 + t2459) * t2591) * t2592 + 0.2e1 * t2587 * t3418 - 0.1e1 * t1363 * t2584 + t1897 * t3763 + (t3968 - 0.1e1 * t3134) * t3785) * t2593 + ((-0.1e1 * t1544 * t2584 + t2591 * t3112) * t2592 - 0.1e1 * t1382 * t2584 - 0.1e1 * t1907 * t3763 + (t1481 * t2578 + t1803 * t2591 + (t4250 + t2901) * t3761) * t2587) * t2586 + t2770 * t3756 - t1521 * t2584 + t1492 * t3763 - t2585 * t3018) * t4005 + t1266 * t3576 + (-t3201 - t3918) * t3544 + ((t1226 + t1473 - t3946) * t2586 - t1698) * t3541 + (t1442 + t4177) * t3580;
  t962 = -t2625 / 0.2e1 + t2637;
  t2689 = -0.13609823097337500000000000000000e-1 * t2585 + t2861;
  t2705 = t2585 * t4142 + t2593 * t3447;
  t2894 = -0.26431758938496000000000000000000e-1 * t2585 + t3958;
  t2731 = t2585 * t3091 + t2593 * t2894;
  t2868 = t2895 * t2593;
  t2629 = (((-0.56786982094425000000000000000000e-2 - t3904) * t2593 + t4043 * t2592 - t3898 + t3090) * t2584 + (t2592 * t4025 - 0.52129746651620000000000000000000e-1 * t2586 + t4180) * t2591 + t2769 * t2592) * t4008 + (t2705 * t2584 + t2731 * t2591 + t2585 * t2868 + (t2584 * t2689 - t3896) * t2586) * t4000;
  t1354 = -t1852 + t4107;
  t1360 = t1486 * t2586 - t1907 * t2585;
  t1693 = -t1771 - t3184;
  t2908 = t3134 + t3731;
  t3010 = t2586 * t3136;
  t3023 = t2585 * t3136;
  t2649 = ((-0.1e1 * t3946 + t1226 + t3727) * t2579 + ((-0.1e1 * t1371 * t2584 - t3135) * t2592 - 0.1e1 * t1659 * t2584 - t1853) * t2593 + (-0.1e1 * t1354 * t2584 - t3010 + t2908) * t2592 - 0.1e1 * t1693 * t2584 + t1669 * t3791 - t1853 + ((t2451 * t2592 + t4236 + t4250) * t2593 + ((-0.1e1 * t1947 * t3761 + t1714 * t4021 + t1946 * t4022) * t2593 + t1907) * t2591) * t2586) * t4007 + t1360 * t3550 + ((t3892 + t3960) * t2592 + t2770 * t2585) * t3546 + (-t1882 + t3023) * t3547 - 0.10875567479902000000000000000000e-1 * t4207 + t1481 * t3408 + (-t2973 * t3664 + t2901) * t3415 / 0.2e1;
  t975 = -t2629 + t2649;
  t3075 = t1030 * t2601 + t2602 * t975 + t2603 * t962;
  t3027 = t2584 * t2412;
  t1036 = (t2416 + t3027 - t3296 + t3738) * t4018 + (((t4252 + (-t2584 * t3157 - t2412 + t3039) * t2591 + t3158 + ((-0.1e1 * t2584 * t3141 - 0.1e1 * t1866) * t2591 + 0.33449653235675560000000000000000e-2) * t2583) * t2592 - 0.1e1 * t1918 - 0.1e1 * t1696 * t2583 + t2109 * t2584 * t3478 - 0.1e1 * t2585 * t2408 + (t2179 + t2317) * t3793) * t2593 + t2584 * t3214 - t2584 * t2417) * t4009 + (-t2036 * t2583 - t2585 * t3155 + t3307) * t4015 + t3724 * t4002 + t2590 * t3209 - t3224 + 0.39510871831575200000000000000000e-3 * t2569;
  t2892 = -0.988270895904e-3 * t2593 + t3374;
  t3026 = t2592 * t3203;
  t2941 = t2593 * t3026;
  t3025 = t2584 * t3194;
  t2942 = t2594 * t3025;
  t2624 = ((((-t2587 * t3120 + (-t2892 + 0.1200936784896e-2) * t2594) * t2591 + t2587 * t3291 - t3282 + t2845) * t2592 + (t3229 * t3354 + (-t2587 * t3365 + t2133) * t2585) * t2591 + (-t2585 * t3671 - t3279) * t2593 + (t2584 * t2848 - t2585 * t3362) * t2586 + t2585 * t3289 + t3279) * t2590 + ((((-t3361 + t3234) * t2593 + (-0.2970426191616e-2 + t3373) * t2594) * t2591 + t2587 * t3292 - t3283 - t2133) * t2592 + (-t2509 * t3354 + (t2461 + (0.2444413220184e-2 + t3364) * t2587) * t2585) * t2591 + (-t2585 * t2848 + t3278) * t2593 + (-t2584 * t3671 - t2585 * t3363) * t2586 + t2585 * t3290 - t3278) * t2583 + t2587 * t2941 + t2587 * t3011 + t2942) * t2588;
  t2636 = t1779 * t3999 + (((t3303 - t2029) * t2592 - t4301 + t3444 * t2585) * t3806 + ((-t3063 + t2924) * t3748 + ((-t2594 * t4172 + t3718) * t2591 + t1631 * t3798 + t3719) * t2592 + t3682 * t3750 + (-t2046 * t2594 + t2587 * t4225) * t2585) * t2593 + ((t3682 * t3763 - t3717) * t2592 + t3529 * t2591 + (t3865 + t3875) * t2594 + (-t3637 - t4299 + t4203 + ((-t1779 + t4069) * t2592 + t3868) * t2585) * t2587) * t2586 + (-t2046 * t2587 + (-t3679 + t3287) * t2594) * t2592 + (t2587 * t4172 - t3860) * t3791 + (-t2040 * t2585 + t2584 * t4287) * t2594) * t4005 + ((t2585 * t3678 + t1325 - t1918 + t4301) * t2586 + t3724) * t3541 + (t3738 - t3531) * t3580 + (t3307 + t4091) * t3576 + t2595 * t3409;
  t969 = -t2624 / 0.2e1 + t2636;
  t2746 = t2593 * t2853 - t3373;
  t3032 = t2584 * t3189;
  t2758 = -t2585 * t3120 - t3032;
  t3031 = t2584 * t3187;
  t2759 = -t2585 * t3121 + t3031;
  t2162 = -t2293 + t3660;
  t2855 = 0.7735484874e-2 * t2162 - t3138;
  t2858 = t3232 + t3397;
  t2859 = 0.3127439544e-2 * t2162 + t3232;
  t2862 = 0.7735484874e-2 * t3829 + 0.16724826617837780000000000000000e-2;
  t2863 = -0.3127439544e-2 * t3829 + 0.54835910640823200000000000000000e-3;
  t2521 = 0.316e0 * t2586 - 0.825e-1;
  t2903 = 0.7735484874e-2 * t2521 + t3366;
  t2904 = -0.3127439544e-2 * t2521 - t3367;
  t2963 = 0.988270895904e-3 - t3374;
  t2634 = ((t2583 * t2862 + t2590 * t2863) * t2592 + (t2583 * t2859 + t2590 * t2855) * t2585 + (t2583 * t2903 + t2590 * t2904 + t3194) * t2584) * t4008 + (((0.2444413220184e-2 + t2746) * t2592 + t3357 + t2759) * t2590 + ((t2593 * t2858 + t2963) * t2592 + t3358 + t2758) * t2583 + t2941 + t3011) * t4000;
  t1952 = t3679 * t2585;
  t1954 = t3682 * t2584;
  t2943 = (-0.1e1 * t1779 + t4069) * t2585;
  t2645 = ((t1325 + t3537) * t2579 + (t3764 * t4172 - t1954) * t2593 + ((-t1955 + t3536) * t2591 + t4232) * t2592 - t1954 + (t3859 + t4108) * t2585 + ((-0.1e1 * t1748 + t3615 - 0.1e1 * t1953 - t3876 + t3063 + t4110) * t2593 - 0.1e1 * t3875 - 0.1e1 * t3865) * t2586) * t4007 + ((t2585 * t3682 - t1631) * t2586 + t4172 * t2585) * t3558 + ((t2943 - t2044) * t2586 - t2046) * t3554 + (t2585 * t3287 + t2592 * t4108 - t1952) * t3546 - t3548 * t4203 - t4235 * t3408;
  t985 = -t2634 + t2645;
  t3074 = t1036 * t2601 + t2602 * t985 + t2603 * t969;
  t1284 = t3080 * t3661;
  t1037 = (-0.1e1 * t1422 * t3668 - t1284) * t4018 + (-0.1e1 * t3952 + t4270) * t4015 + t4049 * t4002 + (-0.1e1 * t1270 * t2585 + t3644 + (-0.1e1 * t2356 + t4147) * t3795 + (-0.1e1 * t3039 + t2412 - 0.1e1 * t2347 + 0.47796540830203740000000000000000e-1) * t2592) * t3571;
  t2950 = -t3164 - 0.1e1 * t2130;
  t3012 = t2594 * t2414;
  t2630 = ((-t1700 * t3784 - (t3594 + t3749) * t2973) * t2577 + ((t4100 * t2592 + 0.1e1 * t3649 + ((-0.1e1 * t1570 - 0.1e1 * t1884) * t2592 + t3898) * t2593) * t2587 + (t2585 * t2764 + t2592 * t2950) * t2594) * t2591 + ((t2587 * t2735 + t2594 * t2861) * t2584 - t2776 * t2587 + t2997 * t3747 + t4084 * t3748 - t3012 + t4135) * t2592 + ((-0.1e1 * t1669 * t3781 + t2734 * t2594) * t2584 - (t2883 - t1832) * t2587 + t2593 * t3113 - t2586 * t3115 - t2590 * t2460 + t3096 * t2594) * t2585 - t2587 * t3655 + t4188 * t3784) * t2588;
  t1624 = t1670 * t3795;
  t2806 = t4251 + t2875;
  t2639 = ((-t1278 * t2585 + (-t1481 - t1891) * t2592) * t3806 + (((t2592 * t3246 + t1625) * t2592 - t1314 * t2585 + t3539) * t3748 - t1252 * t2585 - t2592 * t3647 + t3461 * t3589 + t2997 * t3756 - t3124 * t3798 - t1893 * t3759) * t2593 + (t1462 * t2587 * t3661 - t1188 * t2585 + t1897 * t3589 + t2806 * t3782 + t3125 * t3798 - t3756 * t4084 - 0.12089329343850000000000000000000e-2 * t3759) * t2586 - t1222 * t2585 + (t3891 - t3905) * t3764 + (t1895 * t2592 + t1624) * t2594 - t2592 * t3029 + t2592 * t3177) * t4005 + (-t3911 + (-t1277 * t2586 + t1681) * t2585 + t4109 * t3760) * t3541 + (t3911 - t3952) * t3576 + (-t1284 + t1423 - t3817) * t3580;
  t960 = -t2630 / 0.2e1 + t2639;
  t2716 = t3925 + t1893 + t2392;
  t2697 = t1354 * t2591 + t2716 - t3840;
  t2744 = (t1478 + (t1567 + t4251) * t2585) * t2586 + t2997;
  t2641 = t1462 * t3415 + ((t2592 * t4109 - t3989) * t2579 + (t1294 * t3468 + (-0.1e1 * t3894 + t3247) * t4128 - (t1639 * t2586 + t2910) * t2585 + t4057 * t2586 - t2997 * t2592) * t2593 - t2697 * t2585 - t1948 * t3764 + t4084 * t3760 + t1491 * t2592) * t4008 + t2098 * t3554 - (-0.1e1 * t2896 * t2585 + t3249 * t2592) * t3747 / 0.2e1 + t2744 * t3549 + t3548 * t3838 + t2594 * t4100 * t3560 + t3080 * t3408;
  t2113 = -0.24444132201840000000000000000000e-2 + t2400;
  t1283 = t2113 * t2590 + t2002 + t2115 + t3733;
  t1800 = t1925 * t3752;
  t1204 = t1283 * t2592 + t1769 * t2584 + t1800;
  t1289 = -t1859 + t2002 + t3000 - t4240;
  t1245 = t1289 * t2585 - t1863;
  t2108 = 0.98827089590400000000000000000000e-3 - t3191;
  t1301 = t2108 * t2590 - t2832 + t3728 - t3845;
  t2112 = -0.12009367848960000000000000000000e-2 + t3191;
  t1305 = t2112 * t2590 + t2999 + t3845 + t3901;
  t2825 = t1878 + t4087;
  t1446 = t2586 * t2825 - t1797;
  t1502 = t2584 * t2735 + t3674 + 0.46305794820080000000000000000000e-2;
  t1905 = -t3117 - t4025;
  t1513 = t1905 * t2584 + t2722 - t3152;
  t1754 = t1870 * t2586;
  t2680 = (t1204 * t2591 + t1301 * t2585 + t1446 * t2577 + t1502 * t2592 - t1754 * t2570 + t2586 * t4188) * t4000 + (t1305 * t2592 + t1513 * t2585) * t4008 - t1245 * t3783 / 0.2e1 - t3579 * t3923;
  t972 = t2641 + t2680;
  t3073 = t1037 * t2601 - t2602 * t972 + t2603 * t960;
  t3072 = -0.1e1 * t1654 + t3264;
  t3054 = t1118 * t3170;
  t3052 = t1118 * t3107;
  t3043 = t2584 * t3228;
  t3036 = t2583 * t3166;
  t3030 = t2586 * t3203;
  t3022 = t2585 * t3130;
  t3021 = t2586 * t3163;
  t3019 = t2586 * t3110;
  t3017 = t2587 * t3118;
  t3009 = t2592 * t2414;
  t3006 = t2591 * t3121;
  t3005 = t2591 * t3120;
  t3004 = t2591 * t3119;
  t3001 = t2594 * t2322;
  t2960 = 0.2444413220184e-2 - t3373;
  t2951 = -0.1e1 * t3904 - 0.56786982094425000000000000000000e-2;
  t2940 = t3110 * t3753;
  t2939 = t2586 * t3026;
  t2938 = t2586 * t3036;
  t2937 = t2591 * t3019;
  t2116 = 0.82500000000000000000000000000000e-1 * t4249;
  t2236 = t2590 * t3122;
  t2923 = t2584 * (-t2116 * t3394 + t2236 - t2418);
  t2917 = -0.3127439544e-2 * t2590 + t3394;
  t1539 = (-0.1e1 * t3846 + t2985) * t2591;
  t2909 = t1539 + 0.26431758938496000000000000000000e-1 - 0.2e1 * t3924;
  t2906 = (t2591 * t3536 + t4232) * t2585;
  t1335 = t1451 * t2592 + t2585 * t2965;
  t2664 = (t1335 * t2591 + t3453 * t2592 + (t3959 + t2414 - 0.1e1 * t2087) * t2585) * t4002 + (-t4188 + t3935) * t4010 + (t2399 * t2584 - t3188) * t4003 - t1700 * t3813 / 0.2e1 + t3410 + (t1897 * t2592 + t3924) * t3562;
  t2881 = t3072 * t2592 - 0.1e1 * t2100;
  t2667 = (-0.1e1 * (t2585 * t3072 + t2990) * t2585 + (t1432 * t4020 - 0.1e1 * t1853 + t2881) * t2592) * t4010 + t2841 * t3551 + t3560 * t1401 + t3453 * t3555;
  t1010 = t2664 + t2667;
  t1620 = t2934 - t3343;
  t2167 = 0.187138194629210e-3 + t3207;
  t1757 = t2167 * t2584 + t3316;
  t1101 = (t1757 * t2592 + t1625 + t2994) * t3123 + ((t1620 * t2577 + t4251 - 0.37513059823653620000000000000000e-2 + t3237 + t2182 + 0.81354094419858e-4 * t2569) * t2592 - 0.1e1 * t1757 * t3192) * t2585 + ((t1894 - 0.1e1 * t4137) * t2591 + t2099) * t3192;
  t2600 = q_dot(4);
  t2622 = t1432 * t3414 + (t2578 * t2678 - t2585 * t2657 + t2592 * t2672 + t2704 * t3661 + t2878 * t4140) * t4006 + t2874 * t3572 - t2856 * t3755 / 0.2e1 + t1297 * t2578 * t3545;
  t2648 = (t2594 * t3070 + ((-0.1e1 * t2586 * t4107 - 0.1e1 * t3913) * t3756 + (t1897 * t3781 + (t3895 + t3905) * t2586) * t2585 - t3419) * t2591 + ((t2455 + t3301) * t2594 + t4058 * t2587) * t2592 + ((t3017 + (-0.1e1 * t1669 * t2594 + t3174) * t2586) * t2584 + (t1895 * t2586 + t1826) * t2594 - 0.1e1 * t2586 * t3177 - 0.1e1 * t2587 * t2455) * t2585 + t4055 * t3747) * t4005 - t4188 * t3545 + (t2584 * t3675 + t3674) * t3553 + ((t1852 + t3733) * t2592 + t1800 + t3649) * t3557 + t4101 * t3578 + (t3728 - t3934) * t3572 + t2595 * t3410;
  t967 = t2622 + t2648;
  t2707 = -0.1e1 * t3906 + t2723;
  t2642 = (t3269 * t2578 - 0.1e1 * (t2707 * t2591 - 0.1e1 * t3843 + t2719) * t2585 + (0.2e1 * t2585 * t3071 + t2787 * t4020 + t2708) * t2592) * t4001 + (-t2585 * t2756 + t2592 * t2865 + t2944 * t3661 + t3079 * t3807) * t4008;
  t2050 = t3118 + t3184;
  t2653 = ((t2236 - t3902 + t4134) * t2592 + (t2050 * t2584 - t2455 - 0.46305794820080000000000000000000e-2 * t2586) * t2585) * t4000 + (0.1e1 * t3648 * t2577 + ((-0.1e1 * t2586 * t3461 + t3722) * t2592 - 0.1e1 * t3643 + t1795) * t2591 + (-t2455 - 0.1e1 * t3301) * t2592 + t3382 * t3789 - t1870 * t3818 + (t2825 * t2577 + (-0.1e1 * t2418 - 0.1e1 * t2093) * t2585 - 0.1e1 * t2512 + t2080) * t2593) * t4007 + (t3722 + t3906) * t3406;
  t989 = t2642 + t2653;
  t2899 = -t1010 * t2601 + t1101 * t2600 - t2602 * t989 - t2603 * t967;
  t2763 = -t4259 - t3134;
  t2740 = t1884 * t2584 + t2763 - t3846;
  t2662 = ((-t2002 - t3021) * t2584 + t3010) * t4011 + (t2740 * t2585 + (-0.1e1 * t3899 + (-t2325 + t3443) * t2591) * t2592) * t4002 - t1670 * t3799 / 0.2e1 + t2130 * t3563 - t3190 * t3767;
  t1487 = t1669 - t3914;
  t2669 = -t1730 + 0.13215879469248000000000000000000e-1 * t2585 * t3751 + (t1454 * t2578 + (t2585 * t2837 - t1794) * t2592 - t1487 * t2584 - t3023 + t3703) * t4009 + t4106 * t3555 + t1421 * t2584 * t3552 + t1539 * t3405;
  t1025 = -t2662 + t2669;
  t1142 = (t1620 * t3663 - t3450) * t4030 + t3454 * t3556 + (-0.1e1 * t1894 * t2592 - 0.52863517876992000000000000000000e-1) * t4012 + t2105 * t4004 + (t2167 * t3556 - 0.1e1 * t3125 + t3146) * t2591;
  t1336 = t1590 * t3663 + t3450;
  t1756 = t2973 * t3624;
  t2627 = ((t2086 * t2591 + t3454) * t4246 + ((t2287 * t3783 - 0.1e1 * t2584 * t2779 + 0.1e1 * t1756 + (-0.1e1 * t3270 + t4143 * t3585) * t2591) * t2585 - 0.1e1 * t2925 * t2584 + (t1583 * t2594 - 0.1e1 * t3018) * t2586 + (-0.1e1 * t3003 + t2451) * t2587) * t2592 + t1336 * t3816 + (-0.1e1 * t1324 * t2584 + (t2586 * t2909 + t3118) * t2591) * t3749 - t2751 * t2584 + (t2115 * t3783 - t2591 * t3014 + t2950 * t3763) * t2593 - t2996 * t2587 * t3765 - t2408 * t3783 - t2105 * t3783) * t4005 + (t1310 * t3789 + t2593 * t4106) * t3553 + (-0.1e1 * t3735 * t2584 - t3010 + t2909 * t3751) * t3572 + t3703 * t3544 + t3545 * t1643 + t1454 * t3407;
  t2640 = ((-0.1e1 * (t2056 * t3758 + (t2115 * t2592 - 0.56786982094425000000000000000000e-2) * t2587) * t2586 + t2816 * t2593 + (t4056 * t2585 - 0.1e1 * t2130 * t3760 - t2835 * t2593) * t2594) * t2584 + (-t2049 * t3763 - t2769 * t3748) * t2585 + (-(t2587 * t2991 + t4035) * t2586 + (t2587 * t2810 + t3298) * t2593) * t2591) * t4005 + (t2591 * t3675 + t2868) * t3572 + (-t1670 * t2586 - t1925 * t3757 + t2585 * t3302) * t3574 + (t1670 * t3757 - t3897) * t3557;
  t973 = t2627 - t2640;
  t2635 = ((-0.1e1 * t2951 * t2586 + t2235 * t2592) * t2584 - 0.1e1 * t2928 * t3765) * t4000 + ((-0.1e1 * t1897 * t3752 - 0.1e1 * t2586 * t3447) * t2584 - 0.1e1 * t2894 * t3765 - 0.1e1 * t2585 * t2869) * t4007 + ((t2967 * t2584 + (-0.1e1 * t1907 - 0.1e1 * t3125) * t2591) * t4000 + (t2861 * t2584 + (-0.1e1 * t1925 + t3193) * t2591) * t4007) * t2593;
  t2652 = ((t1466 * t2585 - 0.1e1 * t2707 * t2584 - t3003 + t2451) * t2592 + t1336 * t2571 - 0.1e1 * t2733 * t2584 + t3907 + (-0.1e1 * t1859 + (t1897 - t2454) * t2586) * t2591) * t4000 + ((-t1674 * t3753 - t1798) * t2578 + ((-t1796 + 0.1e1 * t2973 * t3818) * t2585 + t1669 * t3765 + (t2952 * t3752 + t3897) * t2584) * t2592 + (t2584 * t3913 + t2586 * t2770 - t3003) * t2585 - t1669 * t3753 + t3641) * t4007;
  t994 = -t2635 + t2652;
  t2898 = t1025 * t2601 + t1142 * t2600 + t2602 * t994 + t2603 * t973;
  t2633 = (((0.6381775021050e-3 * t2583 - 0.2580137623800e-3 * t2590) * t2593 + (0.2444413220184e-2 * t2583 - 0.988270895904e-3 * t2590) * t2586) * t3764 + ((-0.2444413220184e-2 * t2586 - t3366) * t2590 + (-t3367 - t4039) * t2583) * t2585 + (t2583 * t2890 + t2590 * t2892) * t2584) * t4000 + ((t4040 * t2592 + (t2593 * t3229 + t3330) * t3477 + t2761) * t2590 + ((-t2586 * t2858 - t3367) * t2592 + (-t3329 - t2280) * t3477 + t2760) * t2583 - t2939 + t3004) * t4007;
  t1965 = t2044 * t2593;
  t2659 = (t4235 * t3807 + (t4108 * t2586 + ((t3459 - t3615) * t2585 + t2044) * t2593) * t2592 + (t2586 * t4225 - t4113) * t2585 + t1631 * t3751 - t2801 * t3753) * t4007 + (-0.1e1 * t1779 * t2578 + (t4235 * t2585 + (t2586 * t4172 + t4224) * t2591) * t2592 + t1459 * t2571 + (t2046 * t2586 - t1965 - t3684) * t2585 + t3286 * t2584 + t3531) * t4000;
  t1005 = -t2633 + t2659;
  t2728 = t2523 * t2916 + t3203 + t4202;
  t2658 = t3161 * t3799 + 0.36776100000000000000000000000000e0 * (-0.8676525e-3 * t2590 - 0.3507900e-3 * t2583) * t3760 + (t2024 * t3022 - t2583 * t3195 - t2585 * t3164 + t2592 * t2728) * t4002 + (-t2509 * t3485 + t3229 * t3478 + 0.49096519673609460000000000000000e-2) * t3562 - t3190 * t3800;
  t2665 = (t4299 + t2044 * t2592 + t4282 - t2583 * t3204 + t2584 * t3152 + ((-0.1e1 * t3615 + t3459) * t2592 - t3868) * t2585) * t4009 - t3679 * t3552 + t3312 * t4003 + t1390 * t3405 + t3551 * t1951;
  t1034 = -t2658 + t2665;
  t1135 = (-t2592 * t4235 + t3684) * t3192 - 0.38677424370000000000000000000000e-2 * t2104 * t2583 + (t2578 * t3209 + 0.12009367848960000000000000000000e-2 * t2584 + 0.27521467987200000000000000000000e-3) * t2590 + t4069 * t4030 - 0.50000000000000000000000000000000e0 * t3639 - t3691 * t4029;
  t2619 = t2937 + t2592 * t2940 + ((((t2133 * t2586 - t3281) * t2591 + (t2586 * t3396 + t3366) * t2594) * t2592 + (-0.1200936784896e-2 * t3789 - t4199) * t3763 - t2815 * t2586 + t2739 * t2593) * t2590 + (((-(-t3231 - t3370) * t2586 + t3280) * t2591 + t2586 * t3290 + t2593 * t3363) * t2592 + (t2509 * t3474 + 0.2970426191616e-2 * t3789) * t3763 - t2959 * t2586 + t2738 * t2593) * t2583 + t2594 * t2939 - t2591 * t3002) * t4005 + ((t2593 * t2854 - t3374) * t2592 + (-t2509 * t2586 + 0.4038528e-2 * t3752) * t3477 + t2758) * t3575 + (t2746 * t2592 + (t2586 * t3229 - 0.1632768e-2 * t3752) * t3477 + t2759) * t3564;
  t2623 = t4203 * t3545 + (-t1955 * t2591 + t2593 * t4189) * t3572 + (t3312 + (t1349 * t2585 + t2044) * t2586) * t3553 + t3544 * t4282 + t4235 * t3407 + (-t4235 * t4246 + (((t3720 - 0.1e1 * t3860) * t2591 + t1457 * t2594) * t2586 + (t2943 - 0.1e1 * t2044) * t3747) * t2592 + t1459 * t3816 + (-0.1e1 * t3717 * t2593 + (-0.1e1 * t2583 * t3180 - 0.1e1 * t3014) * t2586 + t2221 + (t4189 * t2586 + 0.1e1 * t4113) * t2594) * t2585 - t3747 * t4282 + (t2594 * t4203 + t3798 * t4172) * t2593 + t3682 * t3612 + ((-0.1e1 * t3034 + 0.790217436631504e-3 * t4052) * t2578 + (((0.3160869746526016e-2 * t3802 + 0.4841887557042460e-2 * t2576 - 0.1e1 * t2166 * t2583 - 0.1e1 * t2413) * t2591 + 0.1096718212816464e-2 * t3800 - 0.3344965323567556e-2 * t2584 * t2590) * t2585 + t4224 * t2591) * t2592 + t3220 * t2585 + t3296 - 0.1e1 * t3027 - 0.1e1 * t2416) * t2587) * t4005;
  t978 = -t2619 + t2623;
  t2891 = t1005 * t2602 + t1034 * t2601 + t1135 * t2600 + t2603 * t978;
  t2877 = -0.1200936784896e-2 * t2591 - 0.54835910640823200000000000000000e-3;
  t2876 = 0.2970426191616e-2 * t2591 - 0.16724826617837780000000000000000e-2;
  t2850 = t3204 - t3381;
  t2849 = 0.16724826617837780000000000000000e-2 * t2584 + t3380;
  t2823 = t2116 * t3393 + t2003 - t2107;
  t2668 = (t2740 * t2592 + (t2591 * t2861 + t3899) * t2585) * t4009 + (t2584 * t2823 - t3003 + t3136) * t4003;
  t2679 = t3420 - t1700 * t3588 - t1796 / 0.2e1 + (t1604 * t3812 - 0.1e1 * t1335 * t2584 + (t1644 + (0.2e1 * t3924 - 0.26431758938496000000000000000000e-1) * t2592) * t2591) * t4009 + (t1612 * t2592 - t1795) * t4012 + t2103 * t3559;
  t1038 = -t2668 + t2679;
  t2712 = t4107 * t2584;
  t1095 = -0.1e1 * (t3933 - 0.1e1 * t3844 - t4259) * t3192 + t1925 * t3795 - 0.1e1 * (-0.1e1 * t2712 + t3731) * t3192 + 0.50000000000000000000000000000000e0 * (t1669 - 0.1e1 * t1670) * t3764;
  t1300 = t3925 / 0.2e1 - t3926 / 0.2e1 + (t2929 + t3343 - t1870) * t3796;
  t2599 = q_dot(5);
  t2638 = ((t2864 * t2592 - 0.1e1 * t3066 * t3752 + ((-0.1e1 * t3163 - 0.1e1 * t2107) * t3784 + t2220) * t2585) * t2584 + t2682 * t2592 + (t2594 * t2852 + t2720) * t3791 - 0.1e1 * t2091 * t2585 * t3768 + (-0.1e1 * t3844 - 0.1e1 * t3239 - 0.1e1 * t2989) * t3785) * t4005 + t2809 * t3553 + (t2592 * t2866 + t3643) * t3574;
  t2663 = t2595 * t3420 - t3260 * t2584 * t3762 + (-t2905 * t2584 + (t1443 * t2592 + (t1427 + (t1604 * t2591 + 0.2e1 * t3924) * t2587) * t2585 + (t4101 * t4022 + 0.2e1 * t1870 * t3799 + (t1605 * t3757 - t1769) * t2591) * t2594) * t2591) * t4005 + (t1604 * t3760 - t2593 * t2973) * t3578 - t3081 * t3794 / 0.2e1 + t3553 * t3909;
  t980 = t1644 * t3587 - t2638 + t2663;
  t2651 = ((-t1863 + (t1859 - t4043) * t2585) * t2584 + (t2585 * t2734 + t3958) * t2591 - t2769 * t2585) * t4001 + (((t1884 * t2592 + t3898) * t2593 + (-t3185 + t4142) * t2592) * t2584 + ((-t1644 - t3124) * t2593 + t3091 * t2592) * t2591 + t2592 * t2868) * t4008;
  t2677 = t2594 * t3418 + (-t1204 * t2584 + (t1670 * t3752 + t2735 * t2592 + (t1604 * t3757 + t1769) * t2591 + (-t1446 - t1754) * t4022) * t2591) * t4007 + t1245 * t3550 + (t1669 * t2592 + t1905 * t2585) * t3558 + t3549 * t3968;
  t999 = t2651 + t2677;
  t2846 = t1038 * t2601 - t1095 * t2600 - t1300 * t2599 + t2602 * t999 + t2603 * t980;
  t2644 = ((-0.1e1 * t2960 * t2585 - t3392 * t4131) * t2590 + (-0.1e1 * t2963 * t2585 + t3391 * t4131) * t2583 + ((-0.1e1 * t2853 * t2585 - t3127) * t2590 + (-0.1e1 * t2858 * t2585 - t3126) * t2583 - t3025) * t2593) * t4007 + ((-0.1e1 * t2863 * t2585 + t2855 * t2592) * t2590 + (-0.1e1 * t2862 * t2585 + t2859 * t2592) * t2583 + t3026) * t4000;
  t2213 = t2586 * t2418;
  t2646 = ((t4283 - 0.1e1 * t3859 - 0.1e1 * t2112 * t2583 + t4240) * t2592 - t1952) * t4000 + ((-0.1e1 * t2029 * t3757 + (-0.1e1 * t1949 + (0.162708188839716e-3 * t2590 + 0.13614453378240000000000000000000e-2) * t2583) * t2586) * t2577 + ((-t2113 * t2583 + t2593 * t4105 + t2213 - t3160) * t2592 - t2801 * t3752 + t4136) * t2591 - t3679 * t3757 + (-0.1e1 * t2108 * t2583 + t3021 - t3148 + t3423 * t2593) * t2585 - t1782 * t3819 - t2938) * t4007 + (t3861 + (t2583 * t4026 + t1600 + t2213 - t2414 + t3874) * t2585) * t3558 + t2029 * t2594 * t3579;
  t1014 = -t2644 + t2646;
  t1804 = -t3036 - t2038;
  t2656 = 0.12900688119000000000000000000000e-3 * t3803 + 0.31908875105250000000000000000000e-3 * t3769 + t3267 * t4004 + (-t2585 * t3163 + (-0.25801376238000000000000000000000e-3 * t2585 + t3166) * t2583) * t4002 + (t4105 * t3764 - t1631 * t3793 - t2029 * t3812 - t3872 + (-t2040 - t4202) * t2585) * t4009 + t3411 + t1804 * t3811 / 0.2e1;
  t2660 = (t1963 * t3130 - 0.1e1 * t2583 * t3126 - 0.1e1 * t2585 * t2728 - 0.1e1 * t2590 * t3127) * t4009 + 0.36776100000000000000000000000000e0 * t2520 * t3822 + (t2583 * t3084 - t2590 * t3085) * t4004 * t3476;
  t1060 = t2656 - t2660;
  t2736 = -0.34036133445600000000000000000000e-3 * t2590 - 0.13760733993600000000000000000000e-3 * t2583 - 0.24548259836804730000000000000000e-2;
  t2802 = -0.27417955320411600000000000000000e-3 * t2583 + t3161;
  t2827 = t2876 * t3803;
  t2828 = t2877 * t3769;
  t1125 = (0.14852130958080000000000000000000e-2 * t2590 + 0.60046839244800000000000000000000e-3 * t2583 + (-0.1e1 * t2802 - 0.1e1 * t3227) * t2591 + (-0.1e1 * t2736 - t3228) * t2584) * t2592 - 0.1e1 * t2040 * t3123 + 0.50000000000000000000000000000000e0 * t2906 + 0.50000000000000000000000000000000e0 * t2828 + 0.50000000000000000000000000000000e0 * t2827;
  t1364 = (-0.136112442957540e-3 * t3802 - t2038) * t2577 / 0.2e1 - t3615 / 0.2e1 + t3582 + 0.68056221478770e-4 * t3802;
  t2620 = ((-t2691 * t2585 + (-t3179 + (t2962 - t3374) * t2594) * t3764 + t2845 * t3757) * t2590 + (-t2675 * t2585 + ((-t3364 + t3373) * t2594 + t3671) * t3764 - t2133 * t3757) * t2583 + t2593 * t2942 + t2587 * t3026 + ((-t3282 + t3293) * t2590 + (-t3283 + t3294) * t2583) * t2592) * t4005 + (-t2718 * t2585 + (t3084 + t3433) * t3351 - t2586 * t3126) * t3575 + (-t2717 * t2585 + (-t3085 - t3434) * t3351 - t2586 * t3127) * t3564 - t3019 * t3793;
  t2628 = 0.68056221478770000000000000000000e-4 * t3744 * t3802 + ((t1804 * t3748 + t2029 * t3253) * t2577 + (t3718 * t2592 + t3721 * t2585 + ((-t1955 - t4172) * t2592 - 0.1e1 * t4136 + ((t1596 - 0.1e1 * t2030) * t2592 + t3863) * t2593) * t2594 + (t3286 + t1600) * t3785) * t2591 + (((t2088 - t3153) * t2583 + t2803) * t3798 + t3679 * t3747 - t2046 * t3781 - t2044 * t3784 + t3719) * t2592 + ((-0.1e1 * t2044 * t2586 + t1505 * t2593 - t2046) * t2594 - t3679 * t2587) * t2585 + t1782 * t3626 + t2594 * t2938) * t4005 + ((t2592 * t4105 - t3863) * t2586 + t3267) * t3557 + (t2586 * t3423 - t1965 + t2044) * t3572 + (t1804 * t2593 - t2029 * t3760) * t3578 + t2595 * t3411 - t3544 * t3872;
  t991 = -t2620 + t2628;
  t2842 = t1014 * t2602 + t1060 * t2601 + t1125 * t2600 + t1364 * t2599 + t2603 * t991;
  t2834 = -0.68072266891200000000000000000000e-3 + t3213;
  t2820 = t2592 * t2849;
  t2650 = (((t2293 * t3392 + t3195) * t2590 + (-t2293 * t3391 - 0.5483591064082320000000000000000e-3 * t2585) * t2583) * t2584 + ((0.680722668912e-3 * t2585 + t2904) * t2590 + (0.275214679872e-3 * t2585 + t2903) * t2583 + t3194) * t2591) * t4000 + ((-t1989 * t3484 + t2586 * t3138 + t2593 * t2820) * t2590 + ((-0.5483591064082320000000000000000e-3 * t2584 + t3381) * t3757 - t1983 * t3484 - t2586 * t3139) * t2583 + t2592 * t3004 - t3030) * t4007;
  t2655 = ((-t2102 * t2592 * t2917 + t3757 * t4172 + t3863) * t2584 + (-t2106 * t2917 - t3867 - t3966) * t2591 + t1633 * t2592) * t4001 + (((-t2030 * t2585 + t3861) * t2593 + t2917 * t2101 * t2585) * t2584 - t3757 * t4282 + t1628 * t3752 + (t4202 + t4283) * t2586) * t4008;
  t1029 = t2650 + t2655;
  t2781 = 0.680722668912e-3 * t2590 + 0.275214679872e-3 * t2583 + 0.49096519673609460000000000000000e-2;
  t2671 = ((-0.28244044800000000000000000000000e0 * t1962 - t3861) * t2584 + t2781 * t3764) * t4009 + (t2583 * t3314 + t2590 * t3313 - t3119) * t4012;
  t1086 = ((-0.1e1 * t2030 * t2584 + t1628) * t2585 + t2801 * t3795 - 0.1e1 * t2592 * t3637 + (-0.1e1 * t2415 + t4094) * t3764) * t4009 + t2923 * t4011 + t2593 * t3583 - t2583 * t3006 + t2590 * t3005 - t2671;
  t2670 = (t2583 * t2850 - t2590 * t2849 - t3137) * t4011 + (-t3369 + 0.1200936784896e-2 * t3795) * t2590 / 0.2e1 + (t3368 - 0.2970426191616e-2 * t3795) * t2583 / 0.2e1;
  t2683 = (t2584 * t2414 + (t3143 - 0.1e1 * t1886) * t2583 + t3688) * t4003 - t4287 * t4004 - t2801 * t3793 / 0.2e1;
  t1164 = -t2670 + t2683;
  t1315 = (t2802 - t3227) * t2591 + (t2736 - t3228) * t2584;
  t1648 = -t3224 + t3165 + (0.2420943778521230000000000000000e-2 * t2590 + 0.50000000000000000000000000000000e0 * t3218 - 0.68072266891200000000000000000000e-3) * t2583;
  t2598 = q_dot(6);
  t2621 = t2940 + t2592 * t2937 + (((-t2584 * t2826 - t3380 * t3747) * t2592 - t2702 * t2584 + t2133 * t3765 + t3380 * t3785 + t2587 * t3369) * t2590 + ((-t2584 * t2709 - t3381 * t3747) * t2592 - t2771 * t2584 + t2845 * t3765 + t3381 * t3785 - t2587 * t3368) * t2583 + t2594 * t3030 + (t2583 * t3280 - t2590 * t3281 + t4078) * t2591) * t4005 + (-t2584 * t2889 - t2850 * t3760 + t3006) * t3575 + (-t2584 * t2888 + t2586 * t2820 - t3005) * t3564;
  t2238 = t2594 * t3160;
  t2631 = (((-0.1e1 * t2051 * t2583 - 0.1e1 * t2228 - 0.1e1 * t2238 + (t2030 * t2593 + t4272) * t2594) * t2585 + (-0.1e1 * t2056 * t2583 + (t2460 - 0.1e1 * t3180) * t2590) * t3757 + (t3001 - 0.1e1 * t1770 * t2583 + (t2587 * t3128 + t2594 * t2834) * t2590) * t2586 + t2592 * t2170 - 0.1e1 * t2587 * t3009) * t2584 + ((-0.1e1 * t2587 * t3851 + t3529) * t2591 + t1633 * t3747) * t2585 + ((-0.1e1 * t2592 * t3001 - 0.1e1 * t1784 * t2583) * t2593 + (-0.1e1 * t2052 * t2583 - 0.1e1 * t2226) * t2586 + (-0.1e1 * t2587 * t3122 + (-0.1e1 * t2834 * t3757 + t3187) * t2594) * t2590 + t3716) * t2591 + t2592 * t3038 + (-0.1e1 * t1949 + (-0.1e1 * t3233 - 0.1e1 * t2091) * t2583) * t3759) * t4005 + ((-t2030 * t2586 - t4257) * t2585 - t1631 * t2593 + t2801 * t3760) * t3574 + (-t1631 * t3760 - t2593 * t2801) * t3557 + t1628 * t2585 * t3544;
  t996 = -t2621 + t2631;
  t2793 = t1029 * t2602 - t1086 * t2601 - t1164 * t2600 - t1315 * t2599 - t1648 * t2598 - t2603 * t996;
  t2773 = -0.275214679872e-3 * t2584 - t3139 - 0.1200936784896e-2;
  t2772 = -0.680722668912e-3 * t2584 + t3138 - 0.2970426191616e-2;
  t2597 = q_dot(7);
  t2567 = 0.316e0 * t2595;
  t2559 = 0.3495e-2 * t2589;
  t2071 = t3505 + t4208;
  t1981 = -t2559 + t4205;
  t1316 = t2781 * t2584 / 0.2e1 + t4202 / 0.2e1 - t3043 + t2802 * t2591;
  t1165 = t2670 + t2683;
  t1126 = (t2583 * t2773 + t2590 * t2772 - t3203) * t4003 - t2828 / 0.2e1 - t2827 / 0.2e1 + t2906 / 0.2e1 + (-t4202 / 0.2e1 + t3583 - t2040 / 0.2e1) * t2592;
  t1110 = -(t2763 - t3844 + t3933) * t2585 / 0.2e1 + (-t2712 + t2908) * t4011 + (t1669 + t1670) * t3559;
  t1091 = -t2593 * t3043 + ((-0.1e1 * t2030 * t2584 - t1633) * t2586 + t2923) * t3192 + (t4203 + ((t3153 - 0.1e1 * t2088) * t2583 - t2803) * t2591) * t2586 * t3123 + t2671;
  t1061 = t2656 + t2660;
  t1039 = t2668 + t2679;
  t1035 = t2658 + t2665;
  t1028 = t2650 - t2655;
  t1026 = t2662 + t2669;
  t1015 = t2644 + t2646;
  t1009 = t2664 - t2667;
  t1006 = t2633 + t2659;
  t1000 = -t2651 + t2677;
  t997 = t2621 + t2631;
  t995 = t2635 + t2652;
  t992 = t2620 + t2628;
  t988 = -t2642 + t2653;
  t986 = t2634 + t2645;
  t984 = t1004 * t2594 - 0.796671776787104e-2 + (t2586 * t4190 + t2765) * t2587;
  t982 = t2638 + t2663;
  t979 = t2619 + t2623;
  t977 = t1008 * t2580 + t1040 * t3780 + t1678 * t2593 + t1394 * t2592 + t1744 * t2586 + t3912 + 0.21398798995968741900000000000000e0 + t3732;
  t976 = t2629 + t2649;
  t974 = t2627 + t2640;
  t971 = -t2641 + t2680;
  t970 = t2624 / 0.2e1 + t2636;
  t966 = -t2622 + t2648;
  t965 = -t2632 + t2666;
  t963 = t2625 / 0.2e1 + t2637;
  t961 = t2630 / 0.2e1 + t2639;
  t955 = t2618 - t2654;
  t948 = t2612 + t2616;
  t946 = t2613 + t2626;
  t944 = (-t2574 / 0.2e1 + t4013) * t984 + (-t1127 * t2593 - t4112 + t977) * t3774;
  t943 = t2615 + t2643;
  t941 = t2614 + t2617;
  t939 = -t2611 + t2647;
  m(7,7) = 0;
  m(2,4) = (t1006 * t2597 + t995 * t2598 + t988 * t2599 + ((t1852 * t2591 - t1796) * t3785 + ((t1852 - t1859) * t3764 - 0.1e1 * t2050 * t2591) * t2594 + (((-0.1e1 * t3896 + t1491) * t2592 + t2913) * t2587 + (-0.1e1 * t2098 * t2592 - t3903 + t3100) * t2594) * t2593 + (((-0.1e1 * t1647 - t3315) * t2578 + ((t4251 - 0.1e1 * t1568 + t1654) * t2585 + t4084) * t2592 - 0.1e1 * t3960 - 0.1e1 * t3899 + t3245) * t2587 + (t3838 - 0.1e1 * t3935 - t3099) * t2594) * t2586) * t2600 + t965 * t2601 + t3322);
  m(6,4) = (t1095 * t2599 + t1164 * t2597 - t2898);
  m(4,3) = (-t1010 * t2599 + t1025 * t2598 + t1034 * t2597 - t3076);
  m(7,4) = (-t1125 * t2599 - t1164 * t2598 - t2891);
  m(7,6) = t2793;
  m(6,7) = (t2597 * t2801 - t2793);
  m(3,3) = (t1007 * t2600 + t1030 * t2598 + t1036 * t2597 + t1037 * t2599);
  m(2,1) = (t947 * t2597 + t945 * t2598 + t942 * t2599 + t940 * t2600 - 0.1e1 * t938 * t2601 + (t1127 * t2588 * t3744 - 0.1e1 * (t4205 - 0.1e1 * t2559) * t3355 + (-0.1e1 * t977 + t4112) * t3774 - 0.1e1 * t1515 * t3333 - 0.1e1 * (t4281 - 0.1e1 * t3879) * t3333 - 0.1e1 * t4273 * t3331 + t1981 * t3355 + (-0.50000000000000000000000000000000e0 * t2581 + t4016) * t984 + (-0.1e1 * t4208 - 0.1e1 * t3505 + t2071) * t2472 * t3479 + (-0.1e1 * t1214 - 0.1e1 * t1333 * t2589 + t3974) * t1322 * t3431 + (t1334 * t2596 - 0.1e1 * t3975 + t1211) * t3339 + (-0.1e1 * t1084 - 0.1e1 * t2508 + (t3971 + (t3888 - 0.1e1 * t4267) * t2587) * t2596 + (-0.1e1 * t2588 * t3456 - 0.1e1 * t2595 * t3349) * t2589) * t3054 + (t1112 + (-0.1e1 * t3948 + (-0.1e1 * t3972 - 0.1e1 * t1650 + 0.825e-1) * t2587) * t2589 + (t2588 * t3465 + t2595 * t2987) * t2596) * t3052 - (-0.1e1 * t1311 * t3432 + (t1511 * t2596 - 0.1e1 * t3963) * t3429) * t1517 + (-0.1e1 * t1286 * t3429 - 0.1e1 * (-0.1e1 * t1455 * t2589 + t3962) * t3432) * t1517 + (0.3228604e1 * t1661 * t2589 - 0.1e1 * (t2818 * t4271 - 0.1e1 * t3827) * t3167 + t3104 * t4292) * t4151 + (t1519 - 0.10000000000000000000000000000000e1 * t1694 * t4271 - 0.1e1 * t3058) * t1724 * t3430) * t2603);
  m(3,4) = (t1035 * t2597 + t1026 * t2598 + t1009 * t2599 + ((t1487 * t2591 + t2592 * t2990 + t4053) * t2593 + (-0.1e1 * t2841 * t2592 + 0.1644487577369270e-2) * t2586 + (t2881 * t2593 + (-0.1e1 * t3985 + t3453) * t2586) * t2585) * t2600 + t3076);
  m(2,3) = (t986 * t2597 + t976 * t2598 + t971 * t2599 + t965 * t2600 + ((t1071 * t2593 + t1138 * t2579 + t1491 * t2585 + t1540 * t2586 + t1693 * t2591 + t2592 * t2697 - t3915 - 0.36044563611157510600000000000000e0) * t2594 - t1173 * t3781 - t1462 * t3623 - t2744 * t3759 - t1360 * t3783 - t1640 * t3784 + t2098 * t3785 + t3175) * t2601 + t3323);
  m(6,2) = (-t1029 * t2597 - t2599 * t999 - t2600 * t994 - t2601 * t975 - t3320);
  m(5,5) = (-t1300 * t2598 + t1364 * t2597);
  m(6,3) = (-t1025 * t2600 - t1038 * t2599 + t1086 * t2597 - t3075);
  m(7,1) = (-t2598 * t996 - t2599 * t991 - t2600 * t978 - t2601 * t969 - t2602 * t947 - t3994);
  m(7,5) = (-t1315 * t2598 - t2842);
  m(4,4) = (t1101 * t2599 + t1135 * t2597 + t1142 * t2598);
  m(4,2) = (t1005 * t2597 + t2598 * t994 - t2599 * t989 - t2601 * t964 - t3322);
  m(4,1) = (t2597 * t978 + t2598 * t973 - t2599 * t967 + t2601 * t956 - t2602 * t940 - t3998);
  m(5,7) = (((0.680722668912e-3 * t2583 - 0.275214679872e-3 * t2590) * t2591 - t3679 * t2584) * t2597 + t1316 * t2598 + t2842);
  m(5,6) = (t1316 * t2597 + (t1670 * t2591 - t4098) * t2598 + t2846);
  m(1,6) = (t997 * t2597 + ((((-0.1e1 * t1884 * t3747 + t1897 * t3748 + t3344) * t2585 + (t3451 - t3837) * t2586 + t3297 * t3757 + (0.56786982094425000000000000000000e-2 + (t2115 * t2593 + t2002 + t2971) * t2592 - t2050) * t2587) * t2591 + (-0.1e1 * t2843 * t2585 - 0.1e1 * t2757 - 0.1e1 * t3241 + (t2835 * t2585 - 0.1e1 * t2914 - 0.1e1 * t2780 - t2696) * t2587) * t2584) * t2588 + t2743 * t3762 - t3790 * t3910 - t3261 * t3794) * t2598 + t982 * t2599 + t974 * t2600 + t963 * t2601 + t946 * t2602 + t3996);
  m(5,2) = (t1014 * t2597 + t2598 * t999 + t2600 * t989 + t2601 * t972 - t3321);
  m(5,3) = (t1010 * t2600 + t1038 * t2598 + t1060 * t2597 - t3073);
  m(7,2) = (-t1005 * t2600 - t1014 * t2599 + t1029 * t2598 - t2601 * t985 - t3319);
  m(4,7) = (((-t2583 * t2772 + t2590 * t2773) * t2585 - (t2592 * t2877 - t3376) * t2583 + (t2592 * t2876 + t3375) * t2590) * t2597 + t1165 * t2598 + t1126 * t2599 + t2891);
  m(3,5) = (t1061 * t2597 + t1039 * t2598 + ((t1794 + (-0.1e1 * t1451 * t2585 + t2965 * t2592) * t2591 - t1758 * t2585 + t1624 + t3009 - t2087 * t2592) * t2586 - t1612 * t3791 - (t2103 * t2584 + t3088) * t2585 + t4084 * t3757 - t2590 * t3128 - t2093 * t2592) * t2599 + t1009 * t2600 + t3073);
  m(2,5) = (t1015 * t2597 + t1000 * t2598 + (((t1301 + t3641) * t2592 + (-t1283 * t2591 - t1502 + t1796) * t2585) * t2587 + ((-t1305 + t3896) * t2585 + (t1289 * t2591 + t1513 - t3925) * t2592) * t2594) * t2599 + t988 * t2600 + t971 * t2601 + t3321);
  m(1,7) = (((-0.1e1 * (-0.1e1 * t2133 * t3751 + t3671) * t2592 * t2583 + (-0.1e1 * t2461 * t2593 * t2583 + (t3671 * t2591 - 0.1e1 * t3833) * t2590) * t2585 + (-0.1e1 * ((-t3291 + t3373) * t2592 + (t2585 * t2962 - t3229 * t3483) * t2591 - t3031) * t2583 + ((-t2593 * t3232 - t2963 - t3292) * t2592 + (t2509 * t3483 - t2585 * t3364) * t2591 + t3032) * t2590) * t2594 + (-0.1e1 * (t2961 * t3764 - 0.1e1 * t3376 * t2593 - t2584 * t4039 + t3376 + (-0.1e1 * t3138 + t3396 + t2890) * t2585) * t2583 + ((t2591 * t2824 + 0.16724826617837780000000000000000e-2) * t2592 + t2584 * t3366 + (0.2444413220184e-2 * t2584 - 0.2580137623800e-3 * t2585) * t2586 + t2585 * t3397 - t3375) * t2590) * t2587) * t2588 - t2673 * t3801 + t2674 * t3766) * t2597 + t997 * t2598 + t992 * t2599 + t979 * t2600 + t970 * t2601 + t948 * t2602 + t3994);
  m(1,4) = (t979 * t2597 + t974 * t2598 + t966 * t2599 + ((-t3455 * t2578 * t3748 + (t3080 * t3606 + (t1556 * t2593 + t1897 * t3784) * t2591 - t2750 * t2586 + t2752 * t2593) * t2592 + (-t2586 * t3345 + t2593 * t2836 + t3735 * t3763 + t1756) * t2585 + (-t1564 * t2586 - t3017) * t2591 - t2732 * t2586 + t2703 * t2593) * t2588 + (-t2586 * t2841 + t2593 * t3467) * t3755 + ((t3453 - t3985) * t2586 + t3448) * t3790 + t4053 * t3744 + t4063 * t2595) * t2600 + t955 * t2601 + t941 * t2602 + t3998);
  m(3,6) = (t1091 * t2597 + (((t1884 * t2591 + t2392) * t2585 - 0.1e1 * t1925 * t3764) * t2586 + (t2591 * t2823 - t3202) * t2585 + t1670 * t3751 + ((t2950 + t3193) * t2593 + t2861 * t3760) * t2584) * t2598 + t1039 * t2599 + t1026 * t2600 + t3075);
  m(3,1) = (t2597 * t969 + t2598 * t962 + t2599 * t960 - t2600 * t956 + t2602 * t938 - t3995);
  m(3,2) = (t2597 * t985 + t2598 * t975 - t2599 * t972 + t2600 * t964 - t3323);
  m(4,5) = (t1126 * t2597 + t1110 * t2598 + ((t2591 * t4107 + t2716) * t2592 + (-0.1e1 * t3896 + t3382) * t2585) * t2599 + t2899);
  m(2,2) = (t2597 * t968 + t2598 * t959 + t2599 * t957 + t2600 * t951 + t2601 * t950 + t4123 * t4260 - t4123);
  m(4,6) = (t1165 * t2597 + ((t2392 + (t3146 - 0.1e1 * t2094) * t2591) * t2592 - (t1669 * t2585 + t2996) * t2584 + t1925 * t3791 - t3136) * t2598 + t1110 * t2599 + t2898);
  m(1,1) = (t2597 * t958 + t2598 * t953 + t2599 * t952 + t2600 * t949 + t2601 * t954 + t2602 * t944);
  m(5,1) = (t2597 * t991 + t2598 * t980 + t2600 * t967 - t2601 * t960 - t2602 * t942 - t3997);
  m(6,6) = (t1648 * t2597);
  m(5,4) = (-t1095 * t2598 + t1125 * t2597 - t2899);
  m(2,6) = (t1028 * t2597 + (((t2951 * t2593 + t4141 * t2592 - 0.1e1 * t3898 + t3090) * t2591 - 0.1e1 * (t3124 + t4180) * t2584) * t2594 + (t2705 * t2591 - 0.1e1 * t2731 * t2584) * t2587 + ((0.13609823097337500000000000000000e-1 * t3764 - 0.1e1 * t2829 * t2584) * t2594 + (t2591 * t2689 + t3899) * t2587) * t2586) * t2598 + t1000 * t2599 + t995 * t2600 + t976 * t2601 + t3320);
  m(2,7) = (((-0.1e1 * (t2592 * t2960 + t3031 + t3357) * t2583 + (t2592 * t2963 - t3032 + t3358) * t2590 + (-0.1e1 * (t2592 * t2853 - t3196) * t2583 + (t2592 * t2858 - t3195) * t2590) * t2593) * t2587 + ((-0.1e1 * t2863 * t2583 + t2862 * t2590) * t2592 + (-0.1e1 * t2855 * t2583 + t2859 * t2590) * t2585 + (-0.1e1 * t2904 * t2583 + t2903 * t2590) * t2584) * t2594) * t2597 + t1028 * t2598 + t1015 * t2599 + t1006 * t2600 + t986 * t2601 + t3319);
  m(6,5) = (t1315 * t2597 - t2846);
  m(1,5) = (t992 * t2597 + t982 * t2598 + (((t1228 * t2591 + t2747) * t2592 + (-0.1e1 * t1235 * t2591 - 0.1e1 * t3982 + t2227 + (t2593 * t3422 + t2831) * t2594) * t2585 + (-0.1e1 * t3248 * t2585 + (t2722 - t3925) * t2592) * t2587) * t2588 + t3605 * t3925 + (-t1287 * t2585 + t3642) * t3762 - t2857 * t3790 + t2808 * t3755) * t2599 + t966 * t2600 + t961 * t2601 + t943 * t2602 + t3997);
  m(1,3) = (t970 * t2597 + t963 * t2598 + t961 * t2599 + t955 * t2600 + ((-0.1e1 * t1083 * t3784 + ((-0.1e1 * t3905 - 0.1e1 * t3891) * t2591 - 0.1e1 * t3842 + t1669 * t3750 - 0.1e1 * t3012 + t4135) * t2592 - t2585 * t3646 + (t2594 * t3288 + t3176) * t2591 - 0.1e1 * t3111 * t3793 - 0.1e1 * t1893 * t3749 + 0.1644487577369270e-2 * t2594) * t2593 + (t2237 * t2592 + (-0.1e1 * t3174 - 0.1e1 * t2244) * t2591 + t1803 * t3750 - 0.1e1 * t2585 * t3115 + ((t2585 * t2806 - 0.1e1 * t2361 + 0.55993270925625000000000000000000e-2) * t2592 + (t2775 + t3850) * t2591 + t4036) * t2594) * t2586 + (-0.1e1 * t2238 + t2832 * t2594) * t2592 - 0.1e1 * t1907 * t4207 - 0.1e1 * t2459 * t3793 + t2585 * t3113 - 0.13297019103287584000000000000000e-1 * t2594 + (-0.1e1 * t1139 * t2579 - 0.1e1 * t1541 * t2593 + ((-0.1e1 * t1853 - 0.1e1 * t2100) * t2592 + t1540) * t2586 + (t4250 - 0.1e1 * t3980 - 0.1e1 * t1758) * t2592 - 0.1e1 * t1771 * t2591 - 0.1e1 * t1347) * t2587) * t2588 * t2601 + t939 * t2602 + t3995);
  m(1,2) = (t948 * t2597 + t946 * t2598 + t943 * t2599 + t941 * t2600 + t939 * t2601 + t944 * t2603 + (t1097 * t2595 * t2580 - 0.1e1 * t2818 * t4273 * t3167 + 0.70400000000000000000000000000000e-3 * t2588 + t1661 * (-0.1e1 * t3481 + t4201) * t3427 + (-0.1e1 * t1281 * t2588 + t3456 * t3739) * t3054 + (-0.1e1 * t1239 * t2588 + t3465 * t3770) * t3052 + t3592 * t3883 - 0.1e1 * t2588 * t1460 * t3759 + (-0.1e1 * t3990 - 0.1e1 * t3604 - 0.1e1 * t2979) * t3778 + (-0.15015000000000000000000000000000e-1 + t4195 + t2742 * t2586) * t2595 + (t2737 * t3745 + (-0.1e1 * t3991 + 0.12805000000000000000000000000000e-1 + (0.1e1 * t1537 - 0.1e1 * t3609 - 0.1e1 * t4237 + t3028 - 0.1e1 * t2072) * t2586) * t2588) * t2594 + (-0.1e1 * t1981 * t3479 + t2071 * t3470) * t3067 + (-0.1e1 * t1519 * t3426 - 0.1e1 * t1515 * t3430) * (-0.1e1 * t2284 * t2588 - 0.1e1 * t1943) + (t1211 * t3431 + t1214 * t3428) * (-0.1e1 * t4300 - 0.1e1 * t4206) + (t1084 * t3107 + t1112 * t3170) * (-0.1e1 * t1308 * t2588 + t2595 * t2988) + ((t2567 + (-0.1e1 * t2156 + 0.1e1 * t4215 - 0.316e0 + t4230) * t2595 + (-0.1e1 * t1526 + t4304) * t2588) * t3339 + (-0.1e1 * t3947 + 0.1e1 * t2479 + 0.1e1 * t1657 * t2588 - 0.1e1 * t2567 + (-0.1e1 * t3327 - 0.1e1 * t3086) * t2595) * t1517 * t3429 + (-0.1e1 * t3331 + t3104 * t4151) * t4151 + (-0.1e1 * (t3475 - 0.1e1 * t2516) * t2595 - 0.1e1 * t4060) * t3333) * t2589 + (0.1e1 * t1286 * t3432 + t1311 * t3429) * (-0.1e1 * t1967 * t2588 - t1692)) * t2602);
  m(6,1) = (t2597 * t996 - t2599 * t980 - t2600 * t973 - t2601 * t962 - t2602 * t945 - t3996);
  m(7,3) = (-t1034 * t2600 - t1060 * t2599 - t1086 * t2598 - t3074);
  m(3,7) = ((((-t2523 * t2917 - t2591 * t3679) * t2592 + t2028 * t3022 + t2583 * t3196 - t2585 * t3152) * t2586 + 0.735522e0 * t2520 * t4200 + (-t2583 * t3313 + t2590 * t3314) * t2591 + t2583 * t3007 + t2590 * t3008) * t2597 + t1091 * t2598 + t1061 * t2599 + t1035 * t2600 + t3074);
end
